simulink model "solar_pv_protected_c07_circuit"  (R2026b)
(part 5 of 16)

      | 確認の範囲　　　　　; 現在の保存回路の端子・配線から求めた静的接続。抵抗やICの内部を導線として短絡せずに集計した。説明の更新は動作シミュレーション、タイミング、実部品の性能・実機動作を保証するものではない。
      | 記録の基準　　　　　; measurement_label_layout_20261022_r01/after_layout_graph.json。部品対応表は端子名の対応付けにのみ使用。
      | 
      | 【この説明欄の略語・記号】
      | 用語1　　　　　　　 ; DC：Direct Current（直流）。ここでは直流電源または直流成分。DCバイアスはコンデンサに重なる直流電圧を指す。
      | 用語2　　　　　　　 ; DC/DC：DC-to-DC Converter（直流電圧変換器）。直流入力を別の直流電圧へ変換する電源回路。絶縁の有無は個々の部品説明で確認する。
      | 用語3　　　　　　　 ; ADC：Analog-to-Digital Converter（アナログ・デジタル変換器）。測定電圧をデジタル値へ変換する回路。電流や温度も、センサーで電圧へ変換した後に読み取る。
      | 用語4　　　　　　　 ; IC：Integrated Circuit（集積回路）。複数の電子素子と機能を小さな半導体チップに集積した部品。
      | 用語5　　　　　　　 ; CH：Channel（測定チャネル）。CH0〜CH7はADCの入力番号であり、同時測定を意味しない。
      | 用語6　　　　　　　 ; MOSFET：Metal-Oxide-Semiconductor Field-Effect Transistor（金属・酸化膜・半導体構造の電界効果トランジスタ）。ゲートとソースの電圧でドレインとソースの導通を制御する素子。N-MOSはNチャネル型を表す。
      | 用語7　　　　　　　 ; LiFePO4：Lithium Iron Phosphate（リン酸鉄リチウム）。電池の正極材料を示す化学式。英語の頭文字を並べた略語ではない。
      | 用語8　　　　　　　 ; GND：Ground（回路の基準電位・電流帰路）。この図の共通基準。保護接地や大地への接続を意味するとは限らない。
      | 用語9　　　　　　　 ; AGND：Analog Ground（アナログ回路の基準端子）。アナログ部分の電流帰路。現図では共通GNDへ接続されるが、実装時の電流経路への配慮は別途必要。
      | 用語10　　　　　　　; DGND：Digital Ground（デジタル回路の基準端子）。デジタル部分の電流帰路。現図では共通GNDへ接続される。
      | 用語11　　　　　　　; VREF/REF：基準電圧を表す端子名。REFはReference（基準）の意味。ADCの変換尺度や電流アンプの出力基準に使う。REF1/REF2の接続電位は個別に確認する。
      | 用語12　　　　　　　; VCC/VDD/VEE/VS：ICの電源端子名。文字の歴史的な由来を現在の接続機能へ当てはめない。現回路のVEEはU8/U10では浮動基準SW、U9ではGND。各電圧・基準は端子と接続を参照する。
      | 用語13　　　　　　　; GNDP：U10の一次側電源の基準端子。絶縁電源の入力側GND。二次側基準VEE=SWと直接同一の導体ではない。
      | 用語14　　　　　　　; SW：Switching Node（スイッチング点）。主電力段の上下MOSFETとL1がつながる、電圧が高速に切り替わる点。GNDとは別電位。
  GND_Label_089 : ConnectionLabel  Description=|  Label=GND
      | この回路での名前　　; GND
      | 種別　　　　　　　　; ConnectionLabel
      | この回路での役割　　; 電池BT1の負極、太陽電池列の負極、制御・測定・保護回路のGNDを結ぶ共通の帰路。高側駆動の浮動帰路SWとは別のノード。
      | 共通帰路の代表接続　; BT1（充電先の蓄電池／51.2V 100Ah LiFePO4）: -
      |                     ; PV1（直列太陽電池列の負極側パネル／400W panel 1/2）: -
      |                     ; U7（RP2040搭載Pico W／SC0918）: 3(GND), 8(GND), 13(GND), 18(GND), 23(GND), 28(GND), 33(AGND), 38(GND)
      |                     ; U1（外付けADC／MCP3208-CI/SL）: 8(CH7), 9(DGND), 14(AGND)
      |                     ; P_U1（保護MOSFETを制御する保護IC／LTC4364IMS-1#PBF）: GND
      |                     ; Q2（同期整流降圧回路の下側スイッチ／TK9R6E15Q5,S1X）: 3(S)
      |                     ; U9（低側の光ゲートドライバ／ACPL-P346-560E）: 4(VEE)
      |                     ; U10（高側ゲート用の浮動電源を作る絶縁DC/DC／UCC14131QDWNRQ1）: 1(GNDP), 2(GNDP), 5(GNDP), 8(GNDP), 9(GNDP), 10(GNDP), 11(GNDP), 12(GNDP), 13(GNDP), 14(GNDP), 15(GNDP), 16(GNDP), 17(GNDP), 18(GNDP)
      | この場所の直接接続　; U5（放熱器温度センサー／TMP235A2DBZR）: 3(GND)
      | 直接接続の範囲　　　; このラベルから実際の線・分岐・明示的な境界端子だけを追った接続。同名ラベルによる離れた場所への接続はこの欄に含めない。
      | 同一ネット全端子　　; BT1: -
      |                     ; C1: 2(n)
      |                     ; C2: 2(n)
      |                     ; C3: 2(n)
      |                     ; C4: 2(n)
      |                     ; C7: 2(n)
      |                     ; C8: 2(n)
      |                     ; C9: 2(n)
      |                     ; C10: 2(n)
      |                     ; C13: 2(n)
      |                     ; C14: 2(n)
      |                     ; C15: 2(n)
      |                     ; C16: 2(n)
      |                     ; C17: 2
      |                     ; C18: 2
      |                     ; C19: 2
      |                     ; C20: 2
      |                     ; C21: 2
      |                     ; C22: 2
      |                     ; C23: 2
      |                     ; C24: 2
      |                     ; C25: 2
      |                     ; C26: 2
      |                     ; C27: 2
      |                     ; C28: 2
      |                     ; C29: 2
      |                     ; C30: 2
      |                     ; C31: 2
      |                     ; C33: 2
      |                     ; C34: 2
      |                     ; C35: 2
      |                     ; C36: 2
      |                     ; C40: 2
      |                     ; C41: 2
      |                     ; C42: 2
      |                     ; C43: 2
      |                     ; C44: 2
      |                     ; C45: 2
      |                     ; C46: 2
      |                     ; C47: 2
      |                     ; C48: 2
      |                     ; D2: 2(A)
      |                     ; PV1: -
      |                     ; P_CHG: N
      |                     ; P_COUT: N
      |                     ; P_CTMR: N
      |                     ; P_D1: A
      |                     ; P_R3: 2
      |                     ; P_R8: 2
      |                     ; P_RSHDN_PD: 2
      |                     ; P_U1: GND
      |                     ; Q2: 3(S)
      |                     ; Q3: 1(S1), 4(S2)
      |                     ; R1: 2(n)
      |                     ; R18: 2
      |                     ; R21: 2
      |                     ; R24: 2
      |                     ; R35: 2
      |                     ; R42: 2
      |                     ; R44: 2
      |                     ; R48: 2
      |                     ; U1: 8(CH7), 9(DGND), 14(AGND)
      |                     ; U2: 2(GND), 3(REF2), 4(RESERVED_GND)
      |                     ; U3: 2(GND), 3(REF2), 4(RESERVED_GND)
      |                     ; U4: 3(GND)
      |                     ; U5: 3(GND)
      |                     ; U6: 3(GND)
      |                     ; U7: 3(GND), 8(GND), 13(GND), 18(GND), 23(GND), 28(GND), 33(AGND), 38(GND)
      |                     ; U9: 4(VEE)
      |                     ; U10: 1(GNDP), 2(GNDP), 5(GNDP), 8(GNDP), 9(GNDP), 10(GNDP), 11(GNDP), 12(GNDP), 13(GNDP), 14(GNDP), 15(GNDP), 16(GNDP), 17(GNDP), 18(GNDP)
      |                     ; U11: 2(GND)
      |                     ; U12: 2(GND)
      | 接続部品数　　　　　; 72部品（部品番号で集計。同一ネット全体）
      | 接続端子数　　　　　; 99端子（423端子の部品対応表で集計。ラベル・境界ポートの重複は含めない）
      | この場所の端子数　　; 1端子／1部品（同名ラベルによる接続を除く）
      | 同階層同名ラベル数　; 75個（このラベル自身を含む）
      | 全階層の接続ラベル　; 87個（実際に同じノードへつながるラベル。名前が違う別名も含む）
      | 接続ルール　　　　　; 同じ階層の同じラベル名を仮想配線として結ぶ。別のSubsystem内とは名前だけでつながらず、明示的なConnection Portと配線をたどる。色は用途の表示であり接続を決めない。
      | 確認の範囲　　　　　; 現在の保存回路の端子・配線から求めた静的接続。抵抗やICの内部を導線として短絡せずに集計した。説明の更新は動作シミュレーション、タイミング、実部品の性能・実機動作を保証するものではない。
      | 記録の基準　　　　　; measurement_label_layout_20261022_r01/after_layout_graph.json。部品対応表は端子名の対応付けにのみ使用。
      | 
      | 【この説明欄の略語・記号】
      | 用語1　　　　　　　 ; DC：Direct Current（直流）。ここでは直流電源または直流成分。DCバイアスはコンデンサに重なる直流電圧を指す。
      | 用語2　　　　　　　 ; DC/DC：DC-to-DC Converter（直流電圧変換器）。直流入力を別の直流電圧へ変換する電源回路。絶縁の有無は個々の部品説明で確認する。
      | 用語3　　　　　　　 ; ADC：Analog-to-Digital Converter（アナログ・デジタル変換器）。測定電圧をデジタル値へ変換する回路。電流や温度も、センサーで電圧へ変換した後に読み取る。
      | 用語4　　　　　　　 ; IC：Integrated Circuit（集積回路）。複数の電子素子と機能を小さな半導体チップに集積した部品。
      | 用語5　　　　　　　 ; CH：Channel（測定チャネル）。CH0〜CH7はADCの入力番号であり、同時測定を意味しない。
      | 用語6　　　　　　　 ; MOSFET：Metal-Oxide-Semiconductor Field-Effect Transistor（金属・酸化膜・半導体構造の電界効果トランジスタ）。ゲートとソースの電圧でドレインとソースの導通を制御する素子。N-MOSはNチャネル型を表す。
      | 用語7　　　　　　　 ; LiFePO4：Lithium Iron Phosphate（リン酸鉄リチウム）。電池の正極材料を示す化学式。英語の頭文字を並べた略語ではない。
      | 用語8　　　　　　　 ; GND：Ground（回路の基準電位・電流帰路）。この図の共通基準。保護接地や大地への接続を意味するとは限らない。
      | 用語9　　　　　　　 ; AGND：Analog Ground（アナログ回路の基準端子）。アナログ部分の電流帰路。現図では共通GNDへ接続されるが、実装時の電流経路への配慮は別途必要。
      | 用語10　　　　　　　; DGND：Digital Ground（デジタル回路の基準端子）。デジタル部分の電流帰路。現図では共通GNDへ接続される。
      | 用語11　　　　　　　; VREF/REF：基準電圧を表す端子名。REFはReference（基準）の意味。ADCの変換尺度や電流アンプの出力基準に使う。REF1/REF2の接続電位は個別に確認する。
      | 用語12　　　　　　　; VCC/VDD/VEE/VS：ICの電源端子名。文字の歴史的な由来を現在の接続機能へ当てはめない。現回路のVEEはU8/U10では浮動基準SW、U9ではGND。各電圧・基準は端子と接続を参照する。
      | 用語13　　　　　　　; GNDP：U10の一次側電源の基準端子。絶縁電源の入力側GND。二次側基準VEE=SWと直接同一の導体ではない。
      | 用語14　　　　　　　; SW：Switching Node（スイッチング点）。主電力段の上下MOSFETとL1がつながる、電圧が高速に切り替わる点。GNDとは別電位。
  GND_Label_090 : ConnectionLabel  Description=|  Label=GND
      | この回路での名前　　; GND
      | 種別　　　　　　　　; ConnectionLabel
      | この回路での役割　　; 電池BT1の負極、太陽電池列の負極、制御・測定・保護回路のGNDを結ぶ共通の帰路。高側駆動の浮動帰路SWとは別のノード。
      | 共通帰路の代表接続　; BT1（充電先の蓄電池／51.2V 100Ah LiFePO4）: -
      |                     ; PV1（直列太陽電池列の負極側パネル／400W panel 1/2）: -
      |                     ; U7（RP2040搭載Pico W／SC0918）: 3(GND), 8(GND), 13(GND), 18(GND), 23(GND), 28(GND), 33(AGND), 38(GND)
      |                     ; U1（外付けADC／MCP3208-CI/SL）: 8(CH7), 9(DGND), 14(AGND)
      |                     ; P_U1（保護MOSFETを制御する保護IC／LTC4364IMS-1#PBF）: GND
      |                     ; Q2（同期整流降圧回路の下側スイッチ／TK9R6E15Q5,S1X）: 3(S)
      |                     ; U9（低側の光ゲートドライバ／ACPL-P346-560E）: 4(VEE)
      |                     ; U10（高側ゲート用の浮動電源を作る絶縁DC/DC／UCC14131QDWNRQ1）: 1(GNDP), 2(GNDP), 5(GNDP), 8(GNDP), 9(GNDP), 10(GNDP), 11(GNDP), 12(GNDP), 13(GNDP), 14(GNDP), 15(GNDP), 16(GNDP), 17(GNDP), 18(GNDP)
      | この場所の直接接続　; U6（2.5Vの測定基準電圧源／REF3025EAIDBZR）: 3(GND)
      | 直接接続の範囲　　　; このラベルから実際の線・分岐・明示的な境界端子だけを追った接続。同名ラベルによる離れた場所への接続はこの欄に含めない。
      | 同一ネット全端子　　; BT1: -
      |                     ; C1: 2(n)
      |                     ; C2: 2(n)
      |                     ; C3: 2(n)
      |                     ; C4: 2(n)
      |                     ; C7: 2(n)
      |                     ; C8: 2(n)
      |                     ; C9: 2(n)
      |                     ; C10: 2(n)
      |                     ; C13: 2(n)
      |                     ; C14: 2(n)
      |                     ; C15: 2(n)
      |                     ; C16: 2(n)
      |                     ; C17: 2
      |                     ; C18: 2
      |                     ; C19: 2
      |                     ; C20: 2
      |                     ; C21: 2
      |                     ; C22: 2
      |                     ; C23: 2
      |                     ; C24: 2
      |                     ; C25: 2
      |                     ; C26: 2
      |                     ; C27: 2
      |                     ; C28: 2
      |                     ; C29: 2
      |                     ; C30: 2
      |                     ; C31: 2
      |                     ; C33: 2
      |                     ; C34: 2
      |                     ; C35: 2
      |                     ; C36: 2
      |                     ; C40: 2
      |                     ; C41: 2
      |                     ; C42: 2
      |                     ; C43: 2
      |                     ; C44: 2
      |                     ; C45: 2
      |                     ; C46: 2
      |                     ; C47: 2
      |                     ; C48: 2
      |                     ; D2: 2(A)
      |                     ; PV1: -
      |                     ; P_CHG: N
      |                     ; P_COUT: N
      |                     ; P_CTMR: N
      |                     ; P_D1: A
      |                     ; P_R3: 2
      |                     ; P_R8: 2
      |                     ; P_RSHDN_PD: 2
      |                     ; P_U1: GND
      |                     ; Q2: 3(S)
      |                     ; Q3: 1(S1), 4(S2)
      |                     ; R1: 2(n)
      |                     ; R18: 2
      |                     ; R21: 2
      |                     ; R24: 2
      |                     ; R35: 2
      |                     ; R42: 2
      |                     ; R44: 2
      |                     ; R48: 2
      |                     ; U1: 8(CH7), 9(DGND), 14(AGND)
      |                     ; U2: 2(GND), 3(REF2), 4(RESERVED_GND)
      |                     ; U3: 2(GND), 3(REF2), 4(RESERVED_GND)
      |                     ; U4: 3(GND)
      |                     ; U5: 3(GND)
      |                     ; U6: 3(GND)
      |                     ; U7: 3(GND), 8(GND), 13(GND), 18(GND), 23(GND), 28(GND), 33(AGND), 38(GND)
      |                     ; U9: 4(VEE)
      |                     ; U10: 1(GNDP), 2(GNDP), 5(GNDP), 8(GNDP), 9(GNDP), 10(GNDP), 11(GNDP), 12(GNDP), 13(GNDP), 14(GNDP), 15(GNDP), 16(GNDP), 17(GNDP), 18(GNDP)
      |                     ; U11: 2(GND)
      |                     ; U12: 2(GND)
      | 接続部品数　　　　　; 72部品（部品番号で集計。同一ネット全体）
      | 接続端子数　　　　　; 99端子（423端子の部品対応表で集計。ラベル・境界ポートの重複は含めない）
      | この場所の端子数　　; 1端子／1部品（同名ラベルによる接続を除く）
      | 同階層同名ラベル数　; 75個（このラベル自身を含む）
      | 全階層の接続ラベル　; 87個（実際に同じノードへつながるラベル。名前が違う別名も含む）
      | 接続ルール　　　　　; 同じ階層の同じラベル名を仮想配線として結ぶ。別のSubsystem内とは名前だけでつながらず、明示的なConnection Portと配線をたどる。色は用途の表示であり接続を決めない。
      | 確認の範囲　　　　　; 現在の保存回路の端子・配線から求めた静的接続。抵抗やICの内部を導線として短絡せずに集計した。説明の更新は動作シミュレーション、タイミング、実部品の性能・実機動作を保証するものではない。
      | 記録の基準　　　　　; measurement_label_layout_20261022_r01/after_layout_graph.json。部品対応表は端子名の対応付けにのみ使用。
      | 
      | 【この説明欄の略語・記号】
      | 用語1　　　　　　　 ; DC：Direct Current（直流）。ここでは直流電源または直流成分。DCバイアスはコンデンサに重なる直流電圧を指す。
      | 用語2　　　　　　　 ; DC/DC：DC-to-DC Converter（直流電圧変換器）。直流入力を別の直流電圧へ変換する電源回路。絶縁の有無は個々の部品説明で確認する。
      | 用語3　　　　　　　 ; ADC：Analog-to-Digital Converter（アナログ・デジタル変換器）。測定電圧をデジタル値へ変換する回路。電流や温度も、センサーで電圧へ変換した後に読み取る。
      | 用語4　　　　　　　 ; IC：Integrated Circuit（集積回路）。複数の電子素子と機能を小さな半導体チップに集積した部品。
      | 用語5　　　　　　　 ; CH：Channel（測定チャネル）。CH0〜CH7はADCの入力番号であり、同時測定を意味しない。
      | 用語6　　　　　　　 ; MOSFET：Metal-Oxide-Semiconductor Field-Effect Transistor（金属・酸化膜・半導体構造の電界効果トランジスタ）。ゲートとソースの電圧でドレインとソースの導通を制御する素子。N-MOSはNチャネル型を表す。
      | 用語7　　　　　　　 ; LiFePO4：Lithium Iron Phosphate（リン酸鉄リチウム）。電池の正極材料を示す化学式。英語の頭文字を並べた略語ではない。
      | 用語8　　　　　　　 ; GND：Ground（回路の基準電位・電流帰路）。この図の共通基準。保護接地や大地への接続を意味するとは限らない。
      | 用語9　　　　　　　 ; AGND：Analog Ground（アナログ回路の基準端子）。アナログ部分の電流帰路。現図では共通GNDへ接続されるが、実装時の電流経路への配慮は別途必要。
      | 用語10　　　　　　　; DGND：Digital Ground（デジタル回路の基準端子）。デジタル部分の電流帰路。現図では共通GNDへ接続される。
      | 用語11　　　　　　　; VREF/REF：基準電圧を表す端子名。REFはReference（基準）の意味。ADCの変換尺度や電流アンプの出力基準に使う。REF1/REF2の接続電位は個別に確認する。
      | 用語12　　　　　　　; VCC/VDD/VEE/VS：ICの電源端子名。文字の歴史的な由来を現在の接続機能へ当てはめない。現回路のVEEはU8/U10では浮動基準SW、U9ではGND。各電圧・基準は端子と接続を参照する。
      | 用語13　　　　　　　; GNDP：U10の一次側電源の基準端子。絶縁電源の入力側GND。二次側基準VEE=SWと直接同一の導体ではない。
      | 用語14　　　　　　　; SW：Switching Node（スイッチング点）。主電力段の上下MOSFETとL1がつながる、電圧が高速に切り替わる点。GNDとは別電位。
  GND_Label_091 : ConnectionLabel  Description=|  Label=GND
      | この回路での名前　　; GND
      | 種別　　　　　　　　; ConnectionLabel
      | この回路での役割　　; 電池BT1の負極、太陽電池列の負極、制御・測定・保護回路のGNDを結ぶ共通の帰路。高側駆動の浮動帰路SWとは別のノード。
      | 共通帰路の代表接続　; BT1（充電先の蓄電池／51.2V 100Ah LiFePO4）: -
      |                     ; PV1（直列太陽電池列の負極側パネル／400W panel 1/2）: -
      |                     ; U7（RP2040搭載Pico W／SC0918）: 3(GND), 8(GND), 13(GND), 18(GND), 23(GND), 28(GND), 33(AGND), 38(GND)
      |                     ; U1（外付けADC／MCP3208-CI/SL）: 8(CH7), 9(DGND), 14(AGND)
      |                     ; P_U1（保護MOSFETを制御する保護IC／LTC4364IMS-1#PBF）: GND
      |                     ; Q2（同期整流降圧回路の下側スイッチ／TK9R6E15Q5,S1X）: 3(S)
      |                     ; U9（低側の光ゲートドライバ／ACPL-P346-560E）: 4(VEE)
      |                     ; U10（高側ゲート用の浮動電源を作る絶縁DC/DC／UCC14131QDWNRQ1）: 1(GNDP), 2(GNDP), 5(GNDP), 8(GNDP), 9(GNDP), 10(GNDP), 11(GNDP), 12(GNDP), 13(GNDP), 14(GNDP), 15(GNDP), 16(GNDP), 17(GNDP), 18(GNDP)
      | この場所の直接接続　; U7（RP2040搭載Pico W／SC0918）: 3(GND)
      | 直接接続の範囲　　　; このラベルから実際の線・分岐・明示的な境界端子だけを追った接続。同名ラベルによる離れた場所への接続はこの欄に含めない。
      | 同一ネット全端子　　; BT1: -
      |                     ; C1: 2(n)
      |                     ; C2: 2(n)
      |                     ; C3: 2(n)
      |                     ; C4: 2(n)
      |                     ; C7: 2(n)
      |                     ; C8: 2(n)
      |                     ; C9: 2(n)
      |                     ; C10: 2(n)
      |                     ; C13: 2(n)
      |                     ; C14: 2(n)
      |                     ; C15: 2(n)
      |                     ; C16: 2(n)
      |                     ; C17: 2
      |                     ; C18: 2
      |                     ; C19: 2
      |                     ; C20: 2
      |                     ; C21: 2
      |                     ; C22: 2
      |                     ; C23: 2
      |                     ; C24: 2
      |                     ; C25: 2
      |                     ; C26: 2
      |                     ; C27: 2
      |                     ; C28: 2
      |                     ; C29: 2
      |                     ; C30: 2
      |                     ; C31: 2
      |                     ; C33: 2
      |                     ; C34: 2
      |                     ; C35: 2
      |                     ; C36: 2
      |                     ; C40: 2
      |                     ; C41: 2
      |                     ; C42: 2
      |                     ; C43: 2
      |                     ; C44: 2
      |                     ; C45: 2
      |                     ; C46: 2
      |                     ; C47: 2
      |                     ; C48: 2
      |                     ; D2: 2(A)
      |                     ; PV1: -
      |                     ; P_CHG: N
      |                     ; P_COUT: N
      |                     ; P_CTMR: N
      |                     ; P_D1: A
      |                     ; P_R3: 2
      |                     ; P_R8: 2
      |                     ; P_RSHDN_PD: 2
      |                     ; P_U1: GND
      |                     ; Q2: 3(S)
      |                     ; Q3: 1(S1), 4(S2)
      |                     ; R1: 2(n)
      |                     ; R18: 2
      |                     ; R21: 2
      |                     ; R24: 2
      |                     ; R35: 2
      |                     ; R42: 2
      |                     ; R44: 2
      |                     ; R48: 2
      |                     ; U1: 8(CH7), 9(DGND), 14(AGND)
      |                     ; U2: 2(GND), 3(REF2), 4(RESERVED_GND)
      |                     ; U3: 2(GND), 3(REF2), 4(RESERVED_GND)
      |                     ; U4: 3(GND)
      |                     ; U5: 3(GND)
      |                     ; U6: 3(GND)
      |                     ; U7: 3(GND), 8(GND), 13(GND), 18(GND), 23(GND), 28(GND), 33(AGND), 38(GND)
      |                     ; U9: 4(VEE)
      |                     ; U10: 1(GNDP), 2(GNDP), 5(GNDP), 8(GNDP), 9(GNDP), 10(GNDP), 11(GNDP), 12(GNDP), 13(GNDP), 14(GNDP), 15(GNDP), 16(GNDP), 17(GNDP), 18(GNDP)
      |                     ; U11: 2(GND)
      |                     ; U12: 2(GND)
      | 接続部品数　　　　　; 72部品（部品番号で集計。同一ネット全体）
      | 接続端子数　　　　　; 99端子（423端子の部品対応表で集計。ラベル・境界ポートの重複は含めない）
      | この場所の端子数　　; 1端子／1部品（同名ラベルによる接続を除く）
      | 同階層同名ラベル数　; 75個（このラベル自身を含む）
      | 全階層の接続ラベル　; 87個（実際に同じノードへつながるラベル。名前が違う別名も含む）
      | 接続ルール　　　　　; 同じ階層の同じラベル名を仮想配線として結ぶ。別のSubsystem内とは名前だけでつながらず、明示的なConnection Portと配線をたどる。色は用途の表示であり接続を決めない。
      | 確認の範囲　　　　　; 現在の保存回路の端子・配線から求めた静的接続。抵抗やICの内部を導線として短絡せずに集計した。説明の更新は動作シミュレーション、タイミング、実部品の性能・実機動作を保証するものではない。
      | 記録の基準　　　　　; measurement_label_layout_20261022_r01/after_layout_graph.json。部品対応表は端子名の対応付けにのみ使用。
      | 
      | 【この説明欄の略語・記号】
      | 用語1　　　　　　　 ; DC：Direct Current（直流）。ここでは直流電源または直流成分。DCバイアスはコンデンサに重なる直流電圧を指す。
      | 用語2　　　　　　　 ; DC/DC：DC-to-DC Converter（直流電圧変換器）。直流入力を別の直流電圧へ変換する電源回路。絶縁の有無は個々の部品説明で確認する。
      | 用語3　　　　　　　 ; ADC：Analog-to-Digital Converter（アナログ・デジタル変換器）。測定電圧をデジタル値へ変換する回路。電流や温度も、センサーで電圧へ変換した後に読み取る。
      | 用語4　　　　　　　 ; IC：Integrated Circuit（集積回路）。複数の電子素子と機能を小さな半導体チップに集積した部品。
      | 用語5　　　　　　　 ; CH：Channel（測定チャネル）。CH0〜CH7はADCの入力番号であり、同時測定を意味しない。
      | 用語6　　　　　　　 ; MOSFET：Metal-Oxide-Semiconductor Field-Effect Transistor（金属・酸化膜・半導体構造の電界効果トランジスタ）。ゲートとソースの電圧でドレインとソースの導通を制御する素子。N-MOSはNチャネル型を表す。
      | 用語7　　　　　　　 ; LiFePO4：Lithium Iron Phosphate（リン酸鉄リチウム）。電池の正極材料を示す化学式。英語の頭文字を並べた略語ではない。
      | 用語8　　　　　　　 ; GND：Ground（回路の基準電位・電流帰路）。この図の共通基準。保護接地や大地への接続を意味するとは限らない。
      | 用語9　　　　　　　 ; AGND：Analog Ground（アナログ回路の基準端子）。アナログ部分の電流帰路。現図では共通GNDへ接続されるが、実装時の電流経路への配慮は別途必要。
      | 用語10　　　　　　　; DGND：Digital Ground（デジタル回路の基準端子）。デジタル部分の電流帰路。現図では共通GNDへ接続される。
      | 用語11　　　　　　　; VREF/REF：基準電圧を表す端子名。REFはReference（基準）の意味。ADCの変換尺度や電流アンプの出力基準に使う。REF1/REF2の接続電位は個別に確認する。
      | 用語12　　　　　　　; VCC/VDD/VEE/VS：ICの電源端子名。文字の歴史的な由来を現在の接続機能へ当てはめない。現回路のVEEはU8/U10では浮動基準SW、U9ではGND。各電圧・基準は端子と接続を参照する。
      | 用語13　　　　　　　; GNDP：U10の一次側電源の基準端子。絶縁電源の入力側GND。二次側基準VEE=SWと直接同一の導体ではない。
      | 用語14　　　　　　　; SW：Switching Node（スイッチング点）。主電力段の上下MOSFETとL1がつながる、電圧が高速に切り替わる点。GNDとは別電位。
  GND_Label_092 : ConnectionLabel  Description=|  Label=GND
      | この回路での名前　　; GND
      | 種別　　　　　　　　; ConnectionLabel
      | この回路での役割　　; 電池BT1の負極、太陽電池列の負極、制御・測定・保護回路のGNDを結ぶ共通の帰路。高側駆動の浮動帰路SWとは別のノード。
      | 共通帰路の代表接続　; BT1（充電先の蓄電池／51.2V 100Ah LiFePO4）: -
      |                     ; PV1（直列太陽電池列の負極側パネル／400W panel 1/2）: -
      |                     ; U7（RP2040搭載Pico W／SC0918）: 3(GND), 8(GND), 13(GND), 18(GND), 23(GND), 28(GND), 33(AGND), 38(GND)
      |                     ; U1（外付けADC／MCP3208-CI/SL）: 8(CH7), 9(DGND), 14(AGND)
      |                     ; P_U1（保護MOSFETを制御する保護IC／LTC4364IMS-1#PBF）: GND
      |                     ; Q2（同期整流降圧回路の下側スイッチ／TK9R6E15Q5,S1X）: 3(S)
      |                     ; U9（低側の光ゲートドライバ／ACPL-P346-560E）: 4(VEE)
      |                     ; U10（高側ゲート用の浮動電源を作る絶縁DC/DC／UCC14131QDWNRQ1）: 1(GNDP), 2(GNDP), 5(GNDP), 8(GNDP), 9(GNDP), 10(GNDP), 11(GNDP), 12(GNDP), 13(GNDP), 14(GNDP), 15(GNDP), 16(GNDP), 17(GNDP), 18(GNDP)
      | この場所の直接接続　; U7（RP2040搭載Pico W／SC0918）: 8(GND)
      | 直接接続の範囲　　　; このラベルから実際の線・分岐・明示的な境界端子だけを追った接続。同名ラベルによる離れた場所への接続はこの欄に含めない。
      | 同一ネット全端子　　; BT1: -
      |                     ; C1: 2(n)
      |                     ; C2: 2(n)
      |                     ; C3: 2(n)
      |                     ; C4: 2(n)
      |                     ; C7: 2(n)
      |                     ; C8: 2(n)
      |                     ; C9: 2(n)
      |                     ; C10: 2(n)
      |                     ; C13: 2(n)
      |                     ; C14: 2(n)
      |                     ; C15: 2(n)
      |                     ; C16: 2(n)
      |                     ; C17: 2
      |                     ; C18: 2
      |                     ; C19: 2
      |                     ; C20: 2
      |                     ; C21: 2
      |                     ; C22: 2
      |                     ; C23: 2
      |                     ; C24: 2
      |                     ; C25: 2
      |                     ; C26: 2
      |                     ; C27: 2
      |                     ; C28: 2
      |                     ; C29: 2
      |                     ; C30: 2
      |                     ; C31: 2
      |                     ; C33: 2
      |                     ; C34: 2
      |                     ; C35: 2
      |                     ; C36: 2
      |                     ; C40: 2
      |                     ; C41: 2
      |                     ; C42: 2
      |                     ; C43: 2
      |                     ; C44: 2
      |                     ; C45: 2
      |                     ; C46: 2
      |                     ; C47: 2
      |                     ; C48: 2
      |                     ; D2: 2(A)
      |                     ; PV1: -
      |                     ; P_CHG: N
      |                     ; P_COUT: N
      |                     ; P_CTMR: N
      |                     ; P_D1: A
      |                     ; P_R3: 2
      |                     ; P_R8: 2
      |                     ; P_RSHDN_PD: 2
      |                     ; P_U1: GND
      |                     ; Q2: 3(S)
      |                     ; Q3: 1(S1), 4(S2)
      |                     ; R1: 2(n)
      |                     ; R18: 2
      |                     ; R21: 2
      |                     ; R24: 2
      |                     ; R35: 2
      |                     ; R42: 2
      |                     ; R44: 2
      |                     ; R48: 2
      |                     ; U1: 8(CH7), 9(DGND), 14(AGND)
      |                     ; U2: 2(GND), 3(REF2), 4(RESERVED_GND)
      |                     ; U3: 2(GND), 3(REF2), 4(RESERVED_GND)
      |                     ; U4: 3(GND)
      |                     ; U5: 3(GND)
      |                     ; U6: 3(GND)
      |                     ; U7: 3(GND), 8(GND), 13(GND), 18(GND), 23(GND), 28(GND), 33(AGND), 38(GND)
      |                     ; U9: 4(VEE)
      |                     ; U10: 1(GNDP), 2(GNDP), 5(GNDP), 8(GNDP), 9(GNDP), 10(GNDP), 11(GNDP), 12(GNDP), 13(GNDP), 14(GNDP), 15(GNDP), 16(GNDP), 17(GNDP), 18(GNDP)
      |                     ; U11: 2(GND)
      |                     ; U12: 2(GND)
      | 接続部品数　　　　　; 72部品（部品番号で集計。同一ネット全体）
      | 接続端子数　　　　　; 99端子（423端子の部品対応表で集計。ラベル・境界ポートの重複は含めない）
      | この場所の端子数　　; 1端子／1部品（同名ラベルによる接続を除く）
      | 同階層同名ラベル数　; 75個（このラベル自身を含む）
      | 全階層の接続ラベル　; 87個（実際に同じノードへつながるラベル。名前が違う別名も含む）
      | 接続ルール　　　　　; 同じ階層の同じラベル名を仮想配線として結ぶ。別のSubsystem内とは名前だけでつながらず、明示的なConnection Portと配線をたどる。色は用途の表示であり接続を決めない。
      | 確認の範囲　　　　　; 現在の保存回路の端子・配線から求めた静的接続。抵抗やICの内部を導線として短絡せずに集計した。説明の更新は動作シミュレーション、タイミング、実部品の性能・実機動作を保証するものではない。
      | 記録の基準　　　　　; measurement_label_layout_20261022_r01/after_layout_graph.json。部品対応表は端子名の対応付けにのみ使用。
      | 
      | 【この説明欄の略語・記号】
      | 用語1　　　　　　　 ; DC：Direct Current（直流）。ここでは直流電源または直流成分。DCバイアスはコンデンサに重なる直流電圧を指す。
      | 用語2　　　　　　　 ; DC/DC：DC-to-DC Converter（直流電圧変換器）。直流入力を別の直流電圧へ変換する電源回路。絶縁の有無は個々の部品説明で確認する。
      | 用語3　　　　　　　 ; ADC：Analog-to-Digital Converter（アナログ・デジタル変換器）。測定電圧をデジタル値へ変換する回路。電流や温度も、センサーで電圧へ変換した後に読み取る。
      | 用語4　　　　　　　 ; IC：Integrated Circuit（集積回路）。複数の電子素子と機能を小さな半導体チップに集積した部品。
      | 用語5　　　　　　　 ; CH：Channel（測定チャネル）。CH0〜CH7はADCの入力番号であり、同時測定を意味しない。
      | 用語6　　　　　　　 ; MOSFET：Metal-Oxide-Semiconductor Field-Effect Transistor（金属・酸化膜・半導体構造の電界効果トランジスタ）。ゲートとソースの電圧でドレインとソースの導通を制御する素子。N-MOSはNチャネル型を表す。
      | 用語7　　　　　　　 ; LiFePO4：Lithium Iron Phosphate（リン酸鉄リチウム）。電池の正極材料を示す化学式。英語の頭文字を並べた略語ではない。
      | 用語8　　　　　　　 ; GND：Ground（回路の基準電位・電流帰路）。この図の共通基準。保護接地や大地への接続を意味するとは限らない。
      | 用語9　　　　　　　 ; AGND：Analog Ground（アナログ回路の基準端子）。アナログ部分の電流帰路。現図では共通GNDへ接続されるが、実装時の電流経路への配慮は別途必要。
      | 用語10　　　　　　　; DGND：Digital Ground（デジタル回路の基準端子）。デジタル部分の電流帰路。現図では共通GNDへ接続される。
      | 用語11　　　　　　　; VREF/REF：基準電圧を表す端子名。REFはReference（基準）の意味。ADCの変換尺度や電流アンプの出力基準に使う。REF1/REF2の接続電位は個別に確認する。
      | 用語12　　　　　　　; VCC/VDD/VEE/VS：ICの電源端子名。文字の歴史的な由来を現在の接続機能へ当てはめない。現回路のVEEはU8/U10では浮動基準SW、U9ではGND。各電圧・基準は端子と接続を参照する。
      | 用語13　　　　　　　; GNDP：U10の一次側電源の基準端子。絶縁電源の入力側GND。二次側基準VEE=SWと直接同一の導体ではない。
      | 用語14　　　　　　　; SW：Switching Node（スイッチング点）。主電力段の上下MOSFETとL1がつながる、電圧が高速に切り替わる点。GNDとは別電位。
  GND_Label_093 : ConnectionLabel  Description=|  Label=GND
      | この回路での名前　　; GND
      | 種別　　　　　　　　; ConnectionLabel
      | この回路での役割　　; 電池BT1の負極、太陽電池列の負極、制御・測定・保護回路のGNDを結ぶ共通の帰路。高側駆動の浮動帰路SWとは別のノード。
      | 共通帰路の代表接続　; BT1（充電先の蓄電池／51.2V 100Ah LiFePO4）: -
      |                     ; PV1（直列太陽電池列の負極側パネル／400W panel 1/2）: -
      |                     ; U7（RP2040搭載Pico W／SC0918）: 3(GND), 8(GND), 13(GND), 18(GND), 23(GND), 28(GND), 33(AGND), 38(GND)
      |                     ; U1（外付けADC／MCP3208-CI/SL）: 8(CH7), 9(DGND), 14(AGND)
      |                     ; P_U1（保護MOSFETを制御する保護IC／LTC4364IMS-1#PBF）: GND
      |                     ; Q2（同期整流降圧回路の下側スイッチ／TK9R6E15Q5,S1X）: 3(S)
      |                     ; U9（低側の光ゲートドライバ／ACPL-P346-560E）: 4(VEE)
      |                     ; U10（高側ゲート用の浮動電源を作る絶縁DC/DC／UCC14131QDWNRQ1）: 1(GNDP), 2(GNDP), 5(GNDP), 8(GNDP), 9(GNDP), 10(GNDP), 11(GNDP), 12(GNDP), 13(GNDP), 14(GNDP), 15(GNDP), 16(GNDP), 17(GNDP), 18(GNDP)
      | この場所の直接接続　; U7（RP2040搭載Pico W／SC0918）: 13(GND)
      | 直接接続の範囲　　　; このラベルから実際の線・分岐・明示的な境界端子だけを追った接続。同名ラベルによる離れた場所への接続はこの欄に含めない。
      | 同一ネット全端子　　; BT1: -
      |                     ; C1: 2(n)
      |                     ; C2: 2(n)
      |                     ; C3: 2(n)
      |                     ; C4: 2(n)
      |                     ; C7: 2(n)
      |                     ; C8: 2(n)
      |                     ; C9: 2(n)
      |                     ; C10: 2(n)
      |                     ; C13: 2(n)
      |                     ; C14: 2(n)
      |                     ; C15: 2(n)
      |                     ; C16: 2(n)
      |                     ; C17: 2
      |                     ; C18: 2
      |                     ; C19: 2
      |                     ; C20: 2
      |                     ; C21: 2
      |                     ; C22: 2
      |                     ; C23: 2
      |                     ; C24: 2
      |                     ; C25: 2
      |                     ; C26: 2
      |                     ; C27: 2
      |                     ; C28: 2
      |                     ; C29: 2
      |                     ; C30: 2
      |                     ; C31: 2
      |                     ; C33: 2
      |                     ; C34: 2
      |                     ; C35: 2
      |                     ; C36: 2
      |                     ; C40: 2
      |                     ; C41: 2
      |                     ; C42: 2
      |                     ; C43: 2
      |                     ; C44: 2
      |                     ; C45: 2
      |                     ; C46: 2
      |                     ; C47: 2
      |                     ; C48: 2
      |                     ; D2: 2(A)
      |                     ; PV1: -
      |                     ; P_CHG: N
      |                     ; P_COUT: N
      |                     ; P_CTMR: N
      |                     ; P_D1: A
      |                     ; P_R3: 2
      |                     ; P_R8: 2
      |                     ; P_RSHDN_PD: 2
      |                     ; P_U1: GND
      |                     ; Q2: 3(S)
      |                     ; Q3: 1(S1), 4(S2)
      |                     ; R1: 2(n)
      |                     ; R18: 2
      |                     ; R21: 2
      |                     ; R24: 2
      |                     ; R35: 2
      |                     ; R42: 2
      |                     ; R44: 2
      |                     ; R48: 2
      |                     ; U1: 8(CH7), 9(DGND), 14(AGND)
      |                     ; U2: 2(GND), 3(REF2), 4(RESERVED_GND)
      |                     ; U3: 2(GND), 3(REF2), 4(RESERVED_GND)
      |                     ; U4: 3(GND)
      |                     ; U5: 3(GND)
      |                     ; U6: 3(GND)
      |                     ; U7: 3(GND), 8(GND), 13(GND), 18(GND), 23(GND), 28(GND), 33(AGND), 38(GND)
      |                     ; U9: 4(VEE)
      |                     ; U10: 1(GNDP), 2(GNDP), 5(GNDP), 8(GNDP), 9(GNDP), 10(GNDP), 11(GNDP), 12(GNDP), 13(GNDP), 14(GNDP), 15(GNDP), 16(GNDP), 17(GNDP), 18(GNDP)
      |                     ; U11: 2(GND)
      |                     ; U12: 2(GND)
      | 接続部品数　　　　　; 72部品（部品番号で集計。同一ネット全体）
      | 接続端子数　　　　　; 99端子（423端子の部品対応表で集計。ラベル・境界ポートの重複は含めない）
      | この場所の端子数　　; 1端子／1部品（同名ラベルによる接続を除く）
      | 同階層同名ラベル数　; 75個（このラベル自身を含む）
      | 全階層の接続ラベル　; 87個（実際に同じノードへつながるラベル。名前が違う別名も含む）
      | 接続ルール　　　　　; 同じ階層の同じラベル名を仮想配線として結ぶ。別のSubsystem内とは名前だけでつながらず、明示的なConnection Portと配線をたどる。色は用途の表示であり接続を決めない。
      | 確認の範囲　　　　　; 現在の保存回路の端子・配線から求めた静的接続。抵抗やICの内部を導線として短絡せずに集計した。説明の更新は動作シミュレーション、タイミング、実部品の性能・実機動作を保証するものではない。
      | 記録の基準　　　　　; measurement_label_layout_20261022_r01/after_layout_graph.json。部品対応表は端子名の対応付けにのみ使用。
      | 
      | 【この説明欄の略語・記号】
      | 用語1　　　　　　　 ; DC：Direct Current（直流）。ここでは直流電源または直流成分。DCバイアスはコンデンサに重なる直流電圧を指す。
      | 用語2　　　　　　　 ; DC/DC：DC-to-DC Converter（直流電圧変換器）。直流入力を別の直流電圧へ変換する電源回路。絶縁の有無は個々の部品説明で確認する。
      | 用語3　　　　　　　 ; ADC：Analog-to-Digital Converter（アナログ・デジタル変換器）。測定電圧をデジタル値へ変換する回路。電流や温度も、センサーで電圧へ変換した後に読み取る。
      | 用語4　　　　　　　 ; IC：Integrated Circuit（集積回路）。複数の電子素子と機能を小さな半導体チップに集積した部品。
      | 用語5　　　　　　　 ; CH：Channel（測定チャネル）。CH0〜CH7はADCの入力番号であり、同時測定を意味しない。
      | 用語6　　　　　　　 ; MOSFET：Metal-Oxide-Semiconductor Field-Effect Transistor（金属・酸化膜・半導体構造の電界効果トランジスタ）。ゲートとソースの電圧でドレインとソースの導通を制御する素子。N-MOSはNチャネル型を表す。
      | 用語7　　　　　　　 ; LiFePO4：Lithium Iron Phosphate（リン酸鉄リチウム）。電池の正極材料を示す化学式。英語の頭文字を並べた略語ではない。
      | 用語8　　　　　　　 ; GND：Ground（回路の基準電位・電流帰路）。この図の共通基準。保護接地や大地への接続を意味するとは限らない。
      | 用語9　　　　　　　 ; AGND：Analog Ground（アナログ回路の基準端子）。アナログ部分の電流帰路。現図では共通GNDへ接続されるが、実装時の電流経路への配慮は別途必要。
      | 用語10　　　　　　　; DGND：Digital Ground（デジタル回路の基準端子）。デジタル部分の電流帰路。現図では共通GNDへ接続される。
      | 用語11　　　　　　　; VREF/REF：基準電圧を表す端子名。REFはReference（基準）の意味。ADCの変換尺度や電流アンプの出力基準に使う。REF1/REF2の接続電位は個別に確認する。
      | 用語12　　　　　　　; VCC/VDD/VEE/VS：ICの電源端子名。文字の歴史的な由来を現在の接続機能へ当てはめない。現回路のVEEはU8/U10では浮動基準SW、U9ではGND。各電圧・基準は端子と接続を参照する。
      | 用語13　　　　　　　; GNDP：U10の一次側電源の基準端子。絶縁電源の入力側GND。二次側基準VEE=SWと直接同一の導体ではない。
      | 用語14　　　　　　　; SW：Switching Node（スイッチング点）。主電力段の上下MOSFETとL1がつながる、電圧が高速に切り替わる点。GNDとは別電位。
  GND_Label_094 : ConnectionLabel  Description=|  Label=GND
      | この回路での名前　　; GND
      | 種別　　　　　　　　; ConnectionLabel
      | この回路での役割　　; 電池BT1の負極、太陽電池列の負極、制御・測定・保護回路のGNDを結ぶ共通の帰路。高側駆動の浮動帰路SWとは別のノード。
      | 共通帰路の代表接続　; BT1（充電先の蓄電池／51.2V 100Ah LiFePO4）: -
      |                     ; PV1（直列太陽電池列の負極側パネル／400W panel 1/2）: -
      |                     ; U7（RP2040搭載Pico W／SC0918）: 3(GND), 8(GND), 13(GND), 18(GND), 23(GND), 28(GND), 33(AGND), 38(GND)
      |                     ; U1（外付けADC／MCP3208-CI/SL）: 8(CH7), 9(DGND), 14(AGND)
      |                     ; P_U1（保護MOSFETを制御する保護IC／LTC4364IMS-1#PBF）: GND
      |                     ; Q2（同期整流降圧回路の下側スイッチ／TK9R6E15Q5,S1X）: 3(S)
      |                     ; U9（低側の光ゲートドライバ／ACPL-P346-560E）: 4(VEE)
      |                     ; U10（高側ゲート用の浮動電源を作る絶縁DC/DC／UCC14131QDWNRQ1）: 1(GNDP), 2(GNDP), 5(GNDP), 8(GNDP), 9(GNDP), 10(GNDP), 11(GNDP), 12(GNDP), 13(GNDP), 14(GNDP), 15(GNDP), 16(GNDP), 17(GNDP), 18(GNDP)
      | この場所の直接接続　; U7（RP2040搭載Pico W／SC0918）: 18(GND)
      | 直接接続の範囲　　　; このラベルから実際の線・分岐・明示的な境界端子だけを追った接続。同名ラベルによる離れた場所への接続はこの欄に含めない。
      | 同一ネット全端子　　; BT1: -
      |                     ; C1: 2(n)
      |                     ; C2: 2(n)
      |                     ; C3: 2(n)
      |                     ; C4: 2(n)
      |                     ; C7: 2(n)
      |                     ; C8: 2(n)
      |                     ; C9: 2(n)
      |                     ; C10: 2(n)
      |                     ; C13: 2(n)
      |                     ; C14: 2(n)
      |                     ; C15: 2(n)
      |                     ; C16: 2(n)
      |                     ; C17: 2
      |                     ; C18: 2
      |                     ; C19: 2
      |                     ; C20: 2
      |                     ; C21: 2
      |                     ; C22: 2
      |                     ; C23: 2
      |                     ; C24: 2
      |                     ; C25: 2
      |                     ; C26: 2
      |                     ; C27: 2
      |                     ; C28: 2
      |                     ; C29: 2
      |                     ; C30: 2
      |                     ; C31: 2
      |                     ; C33: 2
      |                     ; C34: 2
      |                     ; C35: 2
      |                     ; C36: 2
      |                     ; C40: 2
      |                     ; C41: 2
      |                     ; C42: 2
      |                     ; C43: 2
      |                     ; C44: 2
      |                     ; C45: 2
      |                     ; C46: 2
      |                     ; C47: 2
      |                     ; C48: 2
      |                     ; D2: 2(A)
      |                     ; PV1: -
      |                     ; P_CHG: N
      |                     ; P_COUT: N
      |                     ; P_CTMR: N
      |                     ; P_D1: A
      |                     ; P_R3: 2
      |                     ; P_R8: 2
      |                     ; P_RSHDN_PD: 2
      |                     ; P_U1: GND
      |                     ; Q2: 3(S)
      |                     ; Q3: 1(S1), 4(S2)
      |                     ; R1: 2(n)
      |                     ; R18: 2
      |                     ; R21: 2
      |                     ; R24: 2
      |                     ; R35: 2
      |                     ; R42: 2
      |                     ; R44: 2
      |                     ; R48: 2
      |                     ; U1: 8(CH7), 9(DGND), 14(AGND)
      |                     ; U2: 2(GND), 3(REF2), 4(RESERVED_GND)
      |                     ; U3: 2(GND), 3(REF2), 4(RESERVED_GND)
      |                     ; U4: 3(GND)
      |                     ; U5: 3(GND)
      |                     ; U6: 3(GND)
      |                     ; U7: 3(GND), 8(GND), 13(GND), 18(GND), 23(GND), 28(GND), 33(AGND), 38(GND)
      |                     ; U9: 4(VEE)
      |                     ; U10: 1(GNDP), 2(GNDP), 5(GNDP), 8(GNDP), 9(GNDP), 10(GNDP), 11(GNDP), 12(GNDP), 13(GNDP), 14(GNDP), 15(GNDP), 16(GNDP), 17(GNDP), 18(GNDP)
      |                     ; U11: 2(GND)
      |                     ; U12: 2(GND)
      | 接続部品数　　　　　; 72部品（部品番号で集計。同一ネット全体）
      | 接続端子数　　　　　; 99端子（423端子の部品対応表で集計。ラベル・境界ポートの重複は含めない）
      | この場所の端子数　　; 1端子／1部品（同名ラベルによる接続を除く）
      | 同階層同名ラベル数　; 75個（このラベル自身を含む）
      | 全階層の接続ラベル　; 87個（実際に同じノードへつながるラベル。名前が違う別名も含む）
      | 接続ルール　　　　　; 同じ階層の同じラベル名を仮想配線として結ぶ。別のSubsystem内とは名前だけでつながらず、明示的なConnection Portと配線をたどる。色は用途の表示であり接続を決めない。
      | 確認の範囲　　　　　; 現在の保存回路の端子・配線から求めた静的接続。抵抗やICの内部を導線として短絡せずに集計した。説明の更新は動作シミュレーション、タイミング、実部品の性能・実機動作を保証するものではない。
      | 記録の基準　　　　　; measurement_label_layout_20261022_r01/after_layout_graph.json。部品対応表は端子名の対応付けにのみ使用。
      | 
      | 【この説明欄の略語・記号】
      | 用語1　　　　　　　 ; DC：Direct Current（直流）。ここでは直流電源または直流成分。DCバイアスはコンデンサに重なる直流電圧を指す。
      | 用語2　　　　　　　 ; DC/DC：DC-to-DC Converter（直流電圧変換器）。直流入力を別の直流電圧へ変換する電源回路。絶縁の有無は個々の部品説明で確認する。
      | 用語3　　　　　　　 ; ADC：Analog-to-Digital Converter（アナログ・デジタル変換器）。測定電圧をデジタル値へ変換する回路。電流や温度も、センサーで電圧へ変換した後に読み取る。
      | 用語4　　　　　　　 ; IC：Integrated Circuit（集積回路）。複数の電子素子と機能を小さな半導体チップに集積した部品。
      | 用語5　　　　　　　 ; CH：Channel（測定チャネル）。CH0〜CH7はADCの入力番号であり、同時測定を意味しない。
      | 用語6　　　　　　　 ; MOSFET：Metal-Oxide-Semiconductor Field-Effect Transistor（金属・酸化膜・半導体構造の電界効果トランジスタ）。ゲートとソースの電圧でドレインとソースの導通を制御する素子。N-MOSはNチャネル型を表す。
      | 用語7　　　　　　　 ; LiFePO4：Lithium Iron Phosphate（リン酸鉄リチウム）。電池の正極材料を示す化学式。英語の頭文字を並べた略語ではない。
      | 用語8　　　　　　　 ; GND：Ground（回路の基準電位・電流帰路）。この図の共通基準。保護接地や大地への接続を意味するとは限らない。
      | 用語9　　　　　　　 ; AGND：Analog Ground（アナログ回路の基準端子）。アナログ部分の電流帰路。現図では共通GNDへ接続されるが、実装時の電流経路への配慮は別途必要。
      | 用語10　　　　　　　; DGND：Digital Ground（デジタル回路の基準端子）。デジタル部分の電流帰路。現図では共通GNDへ接続される。
      | 用語11　　　　　　　; VREF/REF：基準電圧を表す端子名。REFはReference（基準）の意味。ADCの変換尺度や電流アンプの出力基準に使う。REF1/REF2の接続電位は個別に確認する。
      | 用語12　　　　　　　; VCC/VDD/VEE/VS：ICの電源端子名。文字の歴史的な由来を現在の接続機能へ当てはめない。現回路のVEEはU8/U10では浮動基準SW、U9ではGND。各電圧・基準は端子と接続を参照する。
      | 用語13　　　　　　　; GNDP：U10の一次側電源の基準端子。絶縁電源の入力側GND。二次側基準VEE=SWと直接同一の導体ではない。
      | 用語14　　　　　　　; SW：Switching Node（スイッチング点）。主電力段の上下MOSFETとL1がつながる、電圧が高速に切り替わる点。GNDとは別電位。
  GND_Label_095 : ConnectionLabel  Description=|  Label=GND
      | この回路での名前　　; GND
      | 種別　　　　　　　　; ConnectionLabel
      | この回路での役割　　; 電池BT1の負極、太陽電池列の負極、制御・測定・保護回路のGNDを結ぶ共通の帰路。高側駆動の浮動帰路SWとは別のノード。
      | 共通帰路の代表接続　; BT1（充電先の蓄電池／51.2V 100Ah LiFePO4）: -
      |                     ; PV1（直列太陽電池列の負極側パネル／400W panel 1/2）: -
      |                     ; U7（RP2040搭載Pico W／SC0918）: 3(GND), 8(GND), 13(GND), 18(GND), 23(GND), 28(GND), 33(AGND), 38(GND)
      |                     ; U1（外付けADC／MCP3208-CI/SL）: 8(CH7), 9(DGND), 14(AGND)
      |                     ; P_U1（保護MOSFETを制御する保護IC／LTC4364IMS-1#PBF）: GND
      |                     ; Q2（同期整流降圧回路の下側スイッチ／TK9R6E15Q5,S1X）: 3(S)
      |                     ; U9（低側の光ゲートドライバ／ACPL-P346-560E）: 4(VEE)
      |                     ; U10（高側ゲート用の浮動電源を作る絶縁DC/DC／UCC14131QDWNRQ1）: 1(GNDP), 2(GNDP), 5(GNDP), 8(GNDP), 9(GNDP), 10(GNDP), 11(GNDP), 12(GNDP), 13(GNDP), 14(GNDP), 15(GNDP), 16(GNDP), 17(GNDP), 18(GNDP)
      | この場所の直接接続　; U7（RP2040搭載Pico W／SC0918）: 23(GND)
      | 直接接続の範囲　　　; このラベルから実際の線・分岐・明示的な境界端子だけを追った接続。同名ラベルによる離れた場所への接続はこの欄に含めない。
      | 同一ネット全端子　　; BT1: -
      |                     ; C1: 2(n)
      |                     ; C2: 2(n)
      |                     ; C3: 2(n)
      |                     ; C4: 2(n)
      |                     ; C7: 2(n)
      |                     ; C8: 2(n)
      |                     ; C9: 2(n)
      |                     ; C10: 2(n)
      |                     ; C13: 2(n)
      |                     ; C14: 2(n)
      |                     ; C15: 2(n)
      |                     ; C16: 2(n)
      |                     ; C17: 2
      |                     ; C18: 2
      |                     ; C19: 2
      |                     ; C20: 2
      |                     ; C21: 2
      |                     ; C22: 2
      |                     ; C23: 2
      |                     ; C24: 2
      |                     ; C25: 2
      |                     ; C26: 2
      |                     ; C27: 2
      |                     ; C28: 2
      |                     ; C29: 2
      |                     ; C30: 2
      |                     ; C31: 2
      |                     ; C33: 2
      |                     ; C34: 2
      |                     ; C35: 2
      |                     ; C36: 2
      |                     ; C40: 2
      |                     ; C41: 2
      |                     ; C42: 2
      |                     ; C43: 2
      |                     ; C44: 2
      |                     ; C45: 2
      |                     ; C46: 2
      |                     ; C47: 2
      |                     ; C48: 2
      |                     ; D2: 2(A)
      |                     ; PV1: -
      |                     ; P_CHG: N
      |                     ; P_COUT: N
      |                     ; P_CTMR: N
      |                     ; P_D1: A
      |                     ; P_R3: 2
      |                     ; P_R8: 2
      |                     ; P_RSHDN_PD: 2
      |                     ; P_U1: GND
      |                     ; Q2: 3(S)
      |                     ; Q3: 1(S1), 4(S2)
      |                     ; R1: 2(n)
      |                     ; R18: 2
      |                     ; R21: 2
      |                     ; R24: 2
      |                     ; R35: 2
      |                     ; R42: 2
      |                     ; R44: 2
      |                     ; R48: 2
      |                     ; U1: 8(CH7), 9(DGND), 14(AGND)
      |                     ; U2: 2(GND), 3(REF2), 4(RESERVED_GND)
      |                     ; U3: 2(GND), 3(REF2), 4(RESERVED_GND)
      |                     ; U4: 3(GND)
      |                     ; U5: 3(GND)
      |                     ; U6: 3(GND)
      |                     ; U7: 3(GND), 8(GND), 13(GND), 18(GND), 23(GND), 28(GND), 33(AGND), 38(GND)
      |                     ; U9: 4(VEE)
      |                     ; U10: 1(GNDP), 2(GNDP), 5(GNDP), 8(GNDP), 9(GNDP), 10(GNDP), 11(GNDP), 12(GNDP), 13(GNDP), 14(GNDP), 15(GNDP), 16(GNDP), 17(GNDP), 18(GNDP)
      |                     ; U11: 2(GND)
      |                     ; U12: 2(GND)
      | 接続部品数　　　　　; 72部品（部品番号で集計。同一ネット全体）
      | 接続端子数　　　　　; 99端子（423端子の部品対応表で集計。ラベル・境界ポートの重複は含めない）
      | この場所の端子数　　; 1端子／1部品（同名ラベルによる接続を除く）
      | 同階層同名ラベル数　; 75個（このラベル自身を含む）
      | 全階層の接続ラベル　; 87個（実際に同じノードへつながるラベル。名前が違う別名も含む）
      | 接続ルール　　　　　; 同じ階層の同じラベル名を仮想配線として結ぶ。別のSubsystem内とは名前だけでつながらず、明示的なConnection Portと配線をたどる。色は用途の表示であり接続を決めない。
      | 確認の範囲　　　　　; 現在の保存回路の端子・配線から求めた静的接続。抵抗やICの内部を導線として短絡せずに集計した。説明の更新は動作シミュレーション、タイミング、実部品の性能・実機動作を保証するものではない。
      | 記録の基準　　　　　; measurement_label_layout_20261022_r01/after_layout_graph.json。部品対応表は端子名の対応付けにのみ使用。
      | 
      | 【この説明欄の略語・記号】
      | 用語1　　　　　　　 ; DC：Direct Current（直流）。ここでは直流電源または直流成分。DCバイアスはコンデンサに重なる直流電圧を指す。
      | 用語2　　　　　　　 ; DC/DC：DC-to-DC Converter（直流電圧変換器）。直流入力を別の直流電圧へ変換する電源回路。絶縁の有無は個々の部品説明で確認する。
      | 用語3　　　　　　　 ; ADC：Analog-to-Digital Converter（アナログ・デジタル変換器）。測定電圧をデジタル値へ変換する回路。電流や温度も、センサーで電圧へ変換した後に読み取る。
      | 用語4　　　　　　　 ; IC：Integrated Circuit（集積回路）。複数の電子素子と機能を小さな半導体チップに集積した部品。
      | 用語5　　　　　　　 ; CH：Channel（測定チャネル）。CH0〜CH7はADCの入力番号であり、同時測定を意味しない。
      | 用語6　　　　　　　 ; MOSFET：Metal-Oxide-Semiconductor Field-Effect Transistor（金属・酸化膜・半導体構造の電界効果トランジスタ）。ゲートとソースの電圧でドレインとソースの導通を制御する素子。N-MOSはNチャネル型を表す。
      | 用語7　　　　　　　 ; LiFePO4：Lithium Iron Phosphate（リン酸鉄リチウム）。電池の正極材料を示す化学式。英語の頭文字を並べた略語ではない。
      | 用語8　　　　　　　 ; GND：Ground（回路の基準電位・電流帰路）。この図の共通基準。保護接地や大地への接続を意味するとは限らない。
      | 用語9　　　　　　　 ; AGND：Analog Ground（アナログ回路の基準端子）。アナログ部分の電流帰路。現図では共通GNDへ接続されるが、実装時の電流経路への配慮は別途必要。
      | 用語10　　　　　　　; DGND：Digital Ground（デジタル回路の基準端子）。デジタル部分の電流帰路。現図では共通GNDへ接続される。
      | 用語11　　　　　　　; VREF/REF：基準電圧を表す端子名。REFはReference（基準）の意味。ADCの変換尺度や電流アンプの出力基準に使う。REF1/REF2の接続電位は個別に確認する。
      | 用語12　　　　　　　; VCC/VDD/VEE/VS：ICの電源端子名。文字の歴史的な由来を現在の接続機能へ当てはめない。現回路のVEEはU8/U10では浮動基準SW、U9ではGND。各電圧・基準は端子と接続を参照する。
      | 用語13　　　　　　　; GNDP：U10の一次側電源の基準端子。絶縁電源の入力側GND。二次側基準VEE=SWと直接同一の導体ではない。
      | 用語14　　　　　　　; SW：Switching Node（スイッチング点）。主電力段の上下MOSFETとL1がつながる、電圧が高速に切り替わる点。GNDとは別電位。
  GND_Label_096 : ConnectionLabel  Description=|  Label=GND
      | この回路での名前　　; GND
      | 種別　　　　　　　　; ConnectionLabel
      | この回路での役割　　; 電池BT1の負極、太陽電池列の負極、制御・測定・保護回路のGNDを結ぶ共通の帰路。高側駆動の浮動帰路SWとは別のノード。
      | 共通帰路の代表接続　; BT1（充電先の蓄電池／51.2V 100Ah LiFePO4）: -
      |                     ; PV1（直列太陽電池列の負極側パネル／400W panel 1/2）: -
      |                     ; U7（RP2040搭載Pico W／SC0918）: 3(GND), 8(GND), 13(GND), 18(GND), 23(GND), 28(GND), 33(AGND), 38(GND)
      |                     ; U1（外付けADC／MCP3208-CI/SL）: 8(CH7), 9(DGND), 14(AGND)
      |                     ; P_U1（保護MOSFETを制御する保護IC／LTC4364IMS-1#PBF）: GND
      |                     ; Q2（同期整流降圧回路の下側スイッチ／TK9R6E15Q5,S1X）: 3(S)
      |                     ; U9（低側の光ゲートドライバ／ACPL-P346-560E）: 4(VEE)
      |                     ; U10（高側ゲート用の浮動電源を作る絶縁DC/DC／UCC14131QDWNRQ1）: 1(GNDP), 2(GNDP), 5(GNDP), 8(GNDP), 9(GNDP), 10(GNDP), 11(GNDP), 12(GNDP), 13(GNDP), 14(GNDP), 15(GNDP), 16(GNDP), 17(GNDP), 18(GNDP)
      | この場所の直接接続　; U7（RP2040搭載Pico W／SC0918）: 28(GND)
      | 直接接続の範囲　　　; このラベルから実際の線・分岐・明示的な境界端子だけを追った接続。同名ラベルによる離れた場所への接続はこの欄に含めない。
      | 同一ネット全端子　　; BT1: -
      |                     ; C1: 2(n)
      |                     ; C2: 2(n)
      |                     ; C3: 2(n)
      |                     ; C4: 2(n)
      |                     ; C7: 2(n)
      |                     ; C8: 2(n)
      |                     ; C9: 2(n)
      |                     ; C10: 2(n)
      |                     ; C13: 2(n)
      |                     ; C14: 2(n)
      |                     ; C15: 2(n)
      |                     ; C16: 2(n)
      |                     ; C17: 2
      |                     ; C18: 2
      |                     ; C19: 2
      |                     ; C20: 2
      |                     ; C21: 2
      |                     ; C22: 2
      |                     ; C23: 2
      |                     ; C24: 2
      |                     ; C25: 2
      |                     ; C26: 2
      |                     ; C27: 2
      |                     ; C28: 2
      |                     ; C29: 2
      |                     ; C30: 2
      |                     ; C31: 2
      |                     ; C33: 2
      |                     ; C34: 2
      |                     ; C35: 2
      |                     ; C36: 2
      |                     ; C40: 2
      |                     ; C41: 2
      |                     ; C42: 2
      |                     ; C43: 2
      |                     ; C44: 2
      |                     ; C45: 2
      |                     ; C46: 2
      |                     ; C47: 2
      |                     ; C48: 2
      |                     ; D2: 2(A)
      |                     ; PV1: -
      |                     ; P_CHG: N
      |                     ; P_COUT: N
      |                     ; P_CTMR: N
      |                     ; P_D1: A
      |                     ; P_R3: 2
      |                     ; P_R8: 2
      |                     ; P_RSHDN_PD: 2
      |                     ; P_U1: GND
      |                     ; Q2: 3(S)
      |                     ; Q3: 1(S1), 4(S2)
      |                     ; R1: 2(n)
      |                     ; R18: 2
      |                     ; R21: 2
      |                     ; R24: 2
      |                     ; R35: 2
      |                     ; R42: 2
      |                     ; R44: 2
      |                     ; R48: 2
      |                     ; U1: 8(CH7), 9(DGND), 14(AGND)
      |                     ; U2: 2(GND), 3(REF2), 4(RESERVED_GND)
      |                     ; U3: 2(GND), 3(REF2), 4(RESERVED_GND)
      |                     ; U4: 3(GND)
      |                     ; U5: 3(GND)
      |                     ; U6: 3(GND)
      |                     ; U7: 3(GND), 8(GND), 13(GND), 18(GND), 23(GND), 28(GND), 33(AGND), 38(GND)
      |                     ; U9: 4(VEE)
      |                     ; U10: 1(GNDP), 2(GNDP), 5(GNDP), 8(GNDP), 9(GNDP), 10(GNDP), 11(GNDP), 12(GNDP), 13(GNDP), 14(GNDP), 15(GNDP), 16(GNDP), 17(GNDP), 18(GNDP)
      |                     ; U11: 2(GND)
      |                     ; U12: 2(GND)
      | 接続部品数　　　　　; 72部品（部品番号で集計。同一ネット全体）
      | 接続端子数　　　　　; 99端子（423端子の部品対応表で集計。ラベル・境界ポートの重複は含めない）
      | この場所の端子数　　; 1端子／1部品（同名ラベルによる接続を除く）
      | 同階層同名ラベル数　; 75個（このラベル自身を含む）
      | 全階層の接続ラベル　; 87個（実際に同じノードへつながるラベル。名前が違う別名も含む）
      | 接続ルール　　　　　; 同じ階層の同じラベル名を仮想配線として結ぶ。別のSubsystem内とは名前だけでつながらず、明示的なConnection Portと配線をたどる。色は用途の表示であり接続を決めない。
      | 確認の範囲　　　　　; 現在の保存回路の端子・配線から求めた静的接続。抵抗やICの内部を導線として短絡せずに集計した。説明の更新は動作シミュレーション、タイミング、実部品の性能・実機動作を保証するものではない。
      | 記録の基準　　　　　; measurement_label_layout_20261022_r01/after_layout_graph.json。部品対応表は端子名の対応付けにのみ使用。
      | 
      | 【この説明欄の略語・記号】
      | 用語1　　　　　　　 ; DC：Direct Current（直流）。ここでは直流電源または直流成分。DCバイアスはコンデンサに重なる直流電圧を指す。
      | 用語2　　　　　　　 ; DC/DC：DC-to-DC Converter（直流電圧変換器）。直流入力を別の直流電圧へ変換する電源回路。絶縁の有無は個々の部品説明で確認する。
      | 用語3　　　　　　　 ; ADC：Analog-to-Digital Converter（アナログ・デジタル変換器）。測定電圧をデジタル値へ変換する回路。電流や温度も、センサーで電圧へ変換した後に読み取る。
      | 用語4　　　　　　　 ; IC：Integrated Circuit（集積回路）。複数の電子素子と機能を小さな半導体チップに集積した部品。
      | 用語5　　　　　　　 ; CH：Channel（測定チャネル）。CH0〜CH7はADCの入力番号であり、同時測定を意味しない。
      | 用語6　　　　　　　 ; MOSFET：Metal-Oxide-Semiconductor Field-Effect Transistor（金属・酸化膜・半導体構造の電界効果トランジスタ）。ゲートとソースの電圧でドレインとソースの導通を制御する素子。N-MOSはNチャネル型を表す。
      | 用語7　　　　　　　 ; LiFePO4：Lithium Iron Phosphate（リン酸鉄リチウム）。電池の正極材料を示す化学式。英語の頭文字を並べた略語ではない。
      | 用語8　　　　　　　 ; GND：Ground（回路の基準電位・電流帰路）。この図の共通基準。保護接地や大地への接続を意味するとは限らない。
      | 用語9　　　　　　　 ; AGND：Analog Ground（アナログ回路の基準端子）。アナログ部分の電流帰路。現図では共通GNDへ接続されるが、実装時の電流経路への配慮は別途必要。
      | 用語10　　　　　　　; DGND：Digital Ground（デジタル回路の基準端子）。デジタル部分の電流帰路。現図では共通GNDへ接続される。
      | 用語11　　　　　　　; VREF/REF：基準電圧を表す端子名。REFはReference（基準）の意味。ADCの変換尺度や電流アンプの出力基準に使う。REF1/REF2の接続電位は個別に確認する。
      | 用語12　　　　　　　; VCC/VDD/VEE/VS：ICの電源端子名。文字の歴史的な由来を現在の接続機能へ当てはめない。現回路のVEEはU8/U10では浮動基準SW、U9ではGND。各電圧・基準は端子と接続を参照する。
      | 用語13　　　　　　　; GNDP：U10の一次側電源の基準端子。絶縁電源の入力側GND。二次側基準VEE=SWと直接同一の導体ではない。
      | 用語14　　　　　　　; SW：Switching Node（スイッチング点）。主電力段の上下MOSFETとL1がつながる、電圧が高速に切り替わる点。GNDとは別電位。
  GND_Label_097 : ConnectionLabel  Description=|  Label=GND
      | この回路での名前　　; GND
      | 種別　　　　　　　　; ConnectionLabel
      | この回路での役割　　; 電池BT1の負極、太陽電池列の負極、制御・測定・保護回路のGNDを結ぶ共通の帰路。高側駆動の浮動帰路SWとは別のノード。
      | 共通帰路の代表接続　; BT1（充電先の蓄電池／51.2V 100Ah LiFePO4）: -
      |                     ; PV1（直列太陽電池列の負極側パネル／400W panel 1/2）: -
      |                     ; U7（RP2040搭載Pico W／SC0918）: 3(GND), 8(GND), 13(GND), 18(GND), 23(GND), 28(GND), 33(AGND), 38(GND)
      |                     ; U1（外付けADC／MCP3208-CI/SL）: 8(CH7), 9(DGND), 14(AGND)
      |                     ; P_U1（保護MOSFETを制御する保護IC／LTC4364IMS-1#PBF）: GND
      |                     ; Q2（同期整流降圧回路の下側スイッチ／TK9R6E15Q5,S1X）: 3(S)
      |                     ; U9（低側の光ゲートドライバ／ACPL-P346-560E）: 4(VEE)
      |                     ; U10（高側ゲート用の浮動電源を作る絶縁DC/DC／UCC14131QDWNRQ1）: 1(GNDP), 2(GNDP), 5(GNDP), 8(GNDP), 9(GNDP), 10(GNDP), 11(GNDP), 12(GNDP), 13(GNDP), 14(GNDP), 15(GNDP), 16(GNDP), 17(GNDP), 18(GNDP)
      | この場所の直接接続　; U7（RP2040搭載Pico W／SC0918）: 33(AGND)
      | 直接接続の範囲　　　; このラベルから実際の線・分岐・明示的な境界端子だけを追った接続。同名ラベルによる離れた場所への接続はこの欄に含めない。
      | 同一ネット全端子　　; BT1: -
      |                     ; C1: 2(n)
      |                     ; C2: 2(n)
      |                     ; C3: 2(n)
      |                     ; C4: 2(n)
      |                     ; C7: 2(n)
      |                     ; C8: 2(n)
      |                     ; C9: 2(n)
      |                     ; C10: 2(n)
      |                     ; C13: 2(n)
      |                     ; C14: 2(n)
      |                     ; C15: 2(n)
      |                     ; C16: 2(n)
      |                     ; C17: 2
      |                     ; C18: 2
      |                     ; C19: 2
      |                     ; C20: 2
      |                     ; C21: 2
      |                     ; C22: 2
      |                     ; C23: 2
      |                     ; C24: 2
      |                     ; C25: 2
      |                     ; C26: 2
      |                     ; C27: 2
      |                     ; C28: 2
      |                     ; C29: 2
      |                     ; C30: 2
      |                     ; C31: 2
      |                     ; C33: 2
      |                     ; C34: 2
      |                     ; C35: 2
      |                     ; C36: 2
      |                     ; C40: 2
      |                     ; C41: 2
      |                     ; C42: 2
      |                     ; C43: 2
      |                     ; C44: 2
      |                     ; C45: 2
      |                     ; C46: 2
      |                     ; C47: 2
      |                     ; C48: 2
      |                     ; D2: 2(A)
      |                     ; PV1: -
      |                     ; P_CHG: N
      |                     ; P_COUT: N
      |                     ; P_CTMR: N
      |                     ; P_D1: A
      |                     ; P_R3: 2
      |                     ; P_R8: 2
      |                     ; P_RSHDN_PD: 2
      |                     ; P_U1: GND
      |                     ; Q2: 3(S)
      |                     ; Q3: 1(S1), 4(S2)
      |                     ; R1: 2(n)
      |                     ; R18: 2
      |                     ; R21: 2
      |                     ; R24: 2
      |                     ; R35: 2
      |                     ; R42: 2
      |                     ; R44: 2
      |                     ; R48: 2
      |                     ; U1: 8(CH7), 9(DGND), 14(AGND)
      |                     ; U2: 2(GND), 3(REF2), 4(RESERVED_GND)
      |                     ; U3: 2(GND), 3(REF2), 4(RESERVED_GND)
      |                     ; U4: 3(GND)
      |                     ; U5: 3(GND)
      |                     ; U6: 3(GND)
      |                     ; U7: 3(GND), 8(GND), 13(GND), 18(GND), 23(GND), 28(GND), 33(AGND), 38(GND)
      |                     ; U9: 4(VEE)
      |                     ; U10: 1(GNDP), 2(GNDP), 5(GNDP), 8(GNDP), 9(GNDP), 10(GNDP), 11(GNDP), 12(GNDP), 13(GNDP), 14(GNDP), 15(GNDP), 16(GNDP), 17(GNDP), 18(GNDP)
      |                     ; U11: 2(GND)
      |                     ; U12: 2(GND)
      | 接続部品数　　　　　; 72部品（部品番号で集計。同一ネット全体）
      | 接続端子数　　　　　; 99端子（423端子の部品対応表で集計。ラベル・境界ポートの重複は含めない）
      | この場所の端子数　　; 1端子／1部品（同名ラベルによる接続を除く）
      | 同階層同名ラベル数　; 75個（このラベル自身を含む）
      | 全階層の接続ラベル　; 87個（実際に同じノードへつながるラベル。名前が違う別名も含む）
      | 接続ルール　　　　　; 同じ階層の同じラベル名を仮想配線として結ぶ。別のSubsystem内とは名前だけでつながらず、明示的なConnection Portと配線をたどる。色は用途の表示であり接続を決めない。
      | 確認の範囲　　　　　; 現在の保存回路の端子・配線から求めた静的接続。抵抗やICの内部を導線として短絡せずに集計した。説明の更新は動作シミュレーション、タイミング、実部品の性能・実機動作を保証するものではない。
      | 記録の基準　　　　　; measurement_label_layout_20261022_r01/after_layout_graph.json。部品対応表は端子名の対応付けにのみ使用。
      | 
      | 【この説明欄の略語・記号】
      | 用語1　　　　　　　 ; DC：Direct Current（直流）。ここでは直流電源または直流成分。DCバイアスはコンデンサに重なる直流電圧を指す。
      | 用語2　　　　　　　 ; DC/DC：DC-to-DC Converter（直流電圧変換器）。直流入力を別の直流電圧へ変換する電源回路。絶縁の有無は個々の部品説明で確認する。
      | 用語3　　　　　　　 ; ADC：Analog-to-Digital Converter（アナログ・デジタル変換器）。測定電圧をデジタル値へ変換する回路。電流や温度も、センサーで電圧へ変換した後に読み取る。
      | 用語4　　　　　　　 ; IC：Integrated Circuit（集積回路）。複数の電子素子と機能を小さな半導体チップに集積した部品。
      | 用語5　　　　　　　 ; CH：Channel（測定チャネル）。CH0〜CH7はADCの入力番号であり、同時測定を意味しない。
      | 用語6　　　　　　　 ; MOSFET：Metal-Oxide-Semiconductor Field-Effect Transistor（金属・酸化膜・半導体構造の電界効果トランジスタ）。ゲートとソースの電圧でドレインとソースの導通を制御する素子。N-MOSはNチャネル型を表す。
      | 用語7　　　　　　　 ; LiFePO4：Lithium Iron Phosphate（リン酸鉄リチウム）。電池の正極材料を示す化学式。英語の頭文字を並べた略語ではない。
      | 用語8　　　　　　　 ; GND：Ground（回路の基準電位・電流帰路）。この図の共通基準。保護接地や大地への接続を意味するとは限らない。
      | 用語9　　　　　　　 ; AGND：Analog Ground（アナログ回路の基準端子）。アナログ部分の電流帰路。現図では共通GNDへ接続されるが、実装時の電流経路への配慮は別途必要。
      | 用語10　　　　　　　; DGND：Digital Ground（デジタル回路の基準端子）。デジタル部分の電流帰路。現図では共通GNDへ接続される。
      | 用語11　　　　　　　; VREF/REF：基準電圧を表す端子名。REFはReference（基準）の意味。ADCの変換尺度や電流アンプの出力基準に使う。REF1/REF2の接続電位は個別に確認する。
      | 用語12　　　　　　　; VCC/VDD/VEE/VS：ICの電源端子名。文字の歴史的な由来を現在の接続機能へ当てはめない。現回路のVEEはU8/U10では浮動基準SW、U9ではGND。各電圧・基準は端子と接続を参照する。
      | 用語13　　　　　　　; GNDP：U10の一次側電源の基準端子。絶縁電源の入力側GND。二次側基準VEE=SWと直接同一の導体ではない。
      | 用語14　　　　　　　; SW：Switching Node（スイッチング点）。主電力段の上下MOSFETとL1がつながる、電圧が高速に切り替わる点。GNDとは別電位。
  GND_Label_098 : ConnectionLabel  Description=|  Label=GND
      | この回路での名前　　; GND
      | 種別　　　　　　　　; ConnectionLabel
      | この回路での役割　　; 電池BT1の負極、太陽電池列の負極、制御・測定・保護回路のGNDを結ぶ共通の帰路。高側駆動の浮動帰路SWとは別のノード。
      | 共通帰路の代表接続　; BT1（充電先の蓄電池／51.2V 100Ah LiFePO4）: -
      |                     ; PV1（直列太陽電池列の負極側パネル／400W panel 1/2）: -
      |                     ; U7（RP2040搭載Pico W／SC0918）: 3(GND), 8(GND), 13(GND), 18(GND), 23(GND), 28(GND), 33(AGND), 38(GND)
      |                     ; U1（外付けADC／MCP3208-CI/SL）: 8(CH7), 9(DGND), 14(AGND)
      |                     ; P_U1（保護MOSFETを制御する保護IC／LTC4364IMS-1#PBF）: GND
      |                     ; Q2（同期整流降圧回路の下側スイッチ／TK9R6E15Q5,S1X）: 3(S)
      |                     ; U9（低側の光ゲートドライバ／ACPL-P346-560E）: 4(VEE)
      |                     ; U10（高側ゲート用の浮動電源を作る絶縁DC/DC／UCC14131QDWNRQ1）: 1(GNDP), 2(GNDP), 5(GNDP), 8(GNDP), 9(GNDP), 10(GNDP), 11(GNDP), 12(GNDP), 13(GNDP), 14(GNDP), 15(GNDP), 16(GNDP), 17(GNDP), 18(GNDP)
      | この場所の直接接続　; U7（RP2040搭載Pico W／SC0918）: 38(GND)
      | 直接接続の範囲　　　; このラベルから実際の線・分岐・明示的な境界端子だけを追った接続。同名ラベルによる離れた場所への接続はこの欄に含めない。
      | 同一ネット全端子　　; BT1: -
      |                     ; C1: 2(n)
      |                     ; C2: 2(n)
      |                     ; C3: 2(n)
      |                     ; C4: 2(n)
      |                     ; C7: 2(n)
      |                     ; C8: 2(n)
      |                     ; C9: 2(n)
      |                     ; C10: 2(n)
      |                     ; C13: 2(n)
      |                     ; C14: 2(n)
      |                     ; C15: 2(n)
      |                     ; C16: 2(n)
      |                     ; C17: 2
      |                     ; C18: 2
      |                     ; C19: 2
      |                     ; C20: 2
      |                     ; C21: 2
      |                     ; C22: 2
      |                     ; C23: 2
      |                     ; C24: 2
      |                     ; C25: 2
      |                     ; C26: 2
      |                     ; C27: 2
      |                     ; C28: 2
      |                     ; C29: 2
      |                     ; C30: 2
      |                     ; C31: 2
      |                     ; C33: 2
      |                     ; C34: 2
      |                     ; C35: 2
      |                     ; C36: 2
      |                     ; C40: 2
      |                     ; C41: 2
      |                     ; C42: 2
      |                     ; C43: 2
      |                     ; C44: 2
      |                     ; C45: 2
      |                     ; C46: 2
      |                     ; C47: 2
      |                     ; C48: 2
      |                     ; D2: 2(A)
      |                     ; PV1: -
      |                     ; P_CHG: N
      |                     ; P_COUT: N
      |                     ; P_CTMR: N
      |                     ; P_D1: A
      |                     ; P_R3: 2
      |                     ; P_R8: 2
      |                     ; P_RSHDN_PD: 2
      |                     ; P_U1: GND
      |                     ; Q2: 3(S)
      |                     ; Q3: 1(S1), 4(S2)
      |                     ; R1: 2(n)
      |                     ; R18: 2
      |                     ; R21: 2
      |                     ; R24: 2
      |                     ; R35: 2
      |                     ; R42: 2
      |                     ; R44: 2
      |                     ; R48: 2
      |                     ; U1: 8(CH7), 9(DGND), 14(AGND)
      |                     ; U2: 2(GND), 3(REF2), 4(RESERVED_GND)
      |                     ; U3: 2(GND), 3(REF2), 4(RESERVED_GND)
      |                     ; U4: 3(GND)
      |                     ; U5: 3(GND)
      |                     ; U6: 3(GND)
      |                     ; U7: 3(GND), 8(GND), 13(GND), 18(GND), 23(GND), 28(GND), 33(AGND), 38(GND)
      |                     ; U9: 4(VEE)
      |                     ; U10: 1(GNDP), 2(GNDP), 5(GNDP), 8(GNDP), 9(GNDP), 10(GNDP), 11(GNDP), 12(GNDP), 13(GNDP), 14(GNDP), 15(GNDP), 16(GNDP), 17(GNDP), 18(GNDP)
      |                     ; U11: 2(GND)
      |                     ; U12: 2(GND)
      | 接続部品数　　　　　; 72部品（部品番号で集計。同一ネット全体）
      | 接続端子数　　　　　; 99端子（423端子の部品対応表で集計。ラベル・境界ポートの重複は含めない）
      | この場所の端子数　　; 1端子／1部品（同名ラベルによる接続を除く）
      | 同階層同名ラベル数　; 75個（このラベル自身を含む）
      | 全階層の接続ラベル　; 87個（実際に同じノードへつながるラベル。名前が違う別名も含む）
      | 接続ルール　　　　　; 同じ階層の同じラベル名を仮想配線として結ぶ。別のSubsystem内とは名前だけでつながらず、明示的なConnection Portと配線をたどる。色は用途の表示であり接続を決めない。
      | 確認の範囲　　　　　; 現在の保存回路の端子・配線から求めた静的接続。抵抗やICの内部を導線として短絡せずに集計した。説明の更新は動作シミュレーション、タイミング、実部品の性能・実機動作を保証するものではない。
      | 記録の基準　　　　　; measurement_label_layout_20261022_r01/after_layout_graph.json。部品対応表は端子名の対応付けにのみ使用。
      | 
      | 【この説明欄の略語・記号】
      | 用語1　　　　　　　 ; DC：Direct Current（直流）。ここでは直流電源または直流成分。DCバイアスはコンデンサに重なる直流電圧を指す。
      | 用語2　　　　　　　 ; DC/DC：DC-to-DC Converter（直流電圧変換器）。直流入力を別の直流電圧へ変換する電源回路。絶縁の有無は個々の部品説明で確認する。
      | 用語3　　　　　　　 ; ADC：Analog-to-Digital Converter（アナログ・デジタル変換器）。測定電圧をデジタル値へ変換する回路。電流や温度も、センサーで電圧へ変換した後に読み取る。
      | 用語4　　　　　　　 ; IC：Integrated Circuit（集積回路）。複数の電子素子と機能を小さな半導体チップに集積した部品。
      | 用語5　　　　　　　 ; CH：Channel（測定チャネル）。CH0〜CH7はADCの入力番号であり、同時測定を意味しない。
      | 用語6　　　　　　　 ; MOSFET：Metal-Oxide-Semiconductor Field-Effect Transistor（金属・酸化膜・半導体構造の電界効果トランジスタ）。ゲートとソースの電圧でドレインとソースの導通を制御する素子。N-MOSはNチャネル型を表す。
      | 用語7　　　　　　　 ; LiFePO4：Lithium Iron Phosphate（リン酸鉄リチウム）。電池の正極材料を示す化学式。英語の頭文字を並べた略語ではない。
      | 用語8　　　　　　　 ; GND：Ground（回路の基準電位・電流帰路）。この図の共通基準。保護接地や大地への接続を意味するとは限らない。
      | 用語9　　　　　　　 ; AGND：Analog Ground（アナログ回路の基準端子）。アナログ部分の電流帰路。現図では共通GNDへ接続されるが、実装時の電流経路への配慮は別途必要。
      | 用語10　　　　　　　; DGND：Digital Ground（デジタル回路の基準端子）。デジタル部分の電流帰路。現図では共通GNDへ接続される。
      | 用語11　　　　　　　; VREF/REF：基準電圧を表す端子名。REFはReference（基準）の意味。ADCの変換尺度や電流アンプの出力基準に使う。REF1/REF2の接続電位は個別に確認する。
      | 用語12　　　　　　　; VCC/VDD/VEE/VS：ICの電源端子名。文字の歴史的な由来を現在の接続機能へ当てはめない。現回路のVEEはU8/U10では浮動基準SW、U9ではGND。各電圧・基準は端子と接続を参照する。
      | 用語13　　　　　　　; GNDP：U10の一次側電源の基準端子。絶縁電源の入力側GND。二次側基準VEE=SWと直接同一の導体ではない。
      | 用語14　　　　　　　; SW：Switching Node（スイッチング点）。主電力段の上下MOSFETとL1がつながる、電圧が高速に切り替わる点。GNDとは別電位。
  GND_Label_099 : ConnectionLabel  Description=|  Label=GND
      | この回路での名前　　; GND
      | 種別　　　　　　　　; ConnectionLabel
      | この回路での役割　　; 電池BT1の負極、太陽電池列の負極、制御・測定・保護回路のGNDを結ぶ共通の帰路。高側駆動の浮動帰路SWとは別のノード。
      | 共通帰路の代表接続　; BT1（充電先の蓄電池／51.2V 100Ah LiFePO4）: -
      |                     ; PV1（直列太陽電池列の負極側パネル／400W panel 1/2）: -
      |                     ; U7（RP2040搭載Pico W／SC0918）: 3(GND), 8(GND), 13(GND), 18(GND), 23(GND), 28(GND), 33(AGND), 38(GND)
      |                     ; U1（外付けADC／MCP3208-CI/SL）: 8(CH7), 9(DGND), 14(AGND)
      |                     ; P_U1（保護MOSFETを制御する保護IC／LTC4364IMS-1#PBF）: GND
      |                     ; Q2（同期整流降圧回路の下側スイッチ／TK9R6E15Q5,S1X）: 3(S)
      |                     ; U9（低側の光ゲートドライバ／ACPL-P346-560E）: 4(VEE)
      |                     ; U10（高側ゲート用の浮動電源を作る絶縁DC/DC／UCC14131QDWNRQ1）: 1(GNDP), 2(GNDP), 5(GNDP), 8(GNDP), 9(GNDP), 10(GNDP), 11(GNDP), 12(GNDP), 13(GNDP), 14(GNDP), 15(GNDP), 16(GNDP), 17(GNDP), 18(GNDP)
      | この場所の直接接続　; U9（低側の光ゲートドライバ／ACPL-P346-560E）: 4(VEE)
      | 直接接続の範囲　　　; このラベルから実際の線・分岐・明示的な境界端子だけを追った接続。同名ラベルによる離れた場所への接続はこの欄に含めない。
      | 同一ネット全端子　　; BT1: -
      |                     ; C1: 2(n)
      |                     ; C2: 2(n)
      |                     ; C3: 2(n)
      |                     ; C4: 2(n)
      |                     ; C7: 2(n)
      |                     ; C8: 2(n)
      |                     ; C9: 2(n)
      |                     ; C10: 2(n)
      |                     ; C13: 2(n)
      |                     ; C14: 2(n)
      |                     ; C15: 2(n)
      |                     ; C16: 2(n)
      |                     ; C17: 2
      |                     ; C18: 2
      |                     ; C19: 2
      |                     ; C20: 2
      |                     ; C21: 2
      |                     ; C22: 2
      |                     ; C23: 2
      |                     ; C24: 2
      |                     ; C25: 2
      |                     ; C26: 2
      |                     ; C27: 2
      |                     ; C28: 2
      |                     ; C29: 2
      |                     ; C30: 2
      |                     ; C31: 2
      |                     ; C33: 2
      |                     ; C34: 2
      |                     ; C35: 2
      |                     ; C36: 2
      |                     ; C40: 2
      |                     ; C41: 2
      |                     ; C42: 2
      |                     ; C43: 2
      |                     ; C44: 2
      |                     ; C45: 2
      |                     ; C46: 2
      |                     ; C47: 2
      |                     ; C48: 2
      |                     ; D2: 2(A)
      |                     ; PV1: -
      |                     ; P_CHG: N
      |                     ; P_COUT: N
      |                     ; P_CTMR: N
      |                     ; P_D1: A
      |                     ; P_R3: 2
      |                     ; P_R8: 2
      |                     ; P_RSHDN_PD: 2
      |                     ; P_U1: GND
      |                     ; Q2: 3(S)
      |                     ; Q3: 1(S1), 4(S2)
      |                     ; R1: 2(n)
      |                     ; R18: 2
      |                     ; R21: 2
      |                     ; R24: 2
      |                     ; R35: 2
      |                     ; R42: 2
      |                     ; R44: 2
      |                     ; R48: 2
      |                     ; U1: 8(CH7), 9(DGND), 14(AGND)
      |                     ; U2: 2(GND), 3(REF2), 4(RESERVED_GND)
      |                     ; U3: 2(GND), 3(REF2), 4(RESERVED_GND)
      |                     ; U4: 3(GND)
      |                     ; U5: 3(GND)
      |                     ; U6: 3(GND)
      |                     ; U7: 3(GND), 8(GND), 13(GND), 18(GND), 23(GND), 28(GND), 33(AGND), 38(GND)
      |                     ; U9: 4(VEE)
      |                     ; U10: 1(GNDP), 2(GNDP), 5(GNDP), 8(GNDP), 9(GNDP), 10(GNDP), 11(GNDP), 12(GNDP), 13(GNDP), 14(GNDP), 15(GNDP), 16(GNDP), 17(GNDP), 18(GNDP)
      |                     ; U11: 2(GND)
      |                     ; U12: 2(GND)
      | 接続部品数　　　　　; 72部品（部品番号で集計。同一ネット全体）
      | 接続端子数　　　　　; 99端子（423端子の部品対応表で集計。ラベル・境界ポートの重複は含めない）
      | この場所の端子数　　; 1端子／1部品（同名ラベルによる接続を除く）
      | 同階層同名ラベル数　; 75個（このラベル自身を含む）
      | 全階層の接続ラベル　; 87個（実際に同じノードへつながるラベル。名前が違う別名も含む）
      | 接続ルール　　　　　; 同じ階層の同じラベル名を仮想配線として結ぶ。別のSubsystem内とは名前だけでつながらず、明示的なConnection Portと配線をたどる。色は用途の表示であり接続を決めない。
      | 確認の範囲　　　　　; 現在の保存回路の端子・配線から求めた静的接続。抵抗やICの内部を導線として短絡せずに集計した。説明の更新は動作シミュレーション、タイミング、実部品の性能・実機動作を保証するものではない。
      | 記録の基準　　　　　; measurement_label_layout_20261022_r01/after_layout_graph.json。部品対応表は端子名の対応付けにのみ使用。
      | 
      | 【この説明欄の略語・記号】
      | 用語1　　　　　　　 ; DC：Direct Current（直流）。ここでは直流電源または直流成分。DCバイアスはコンデンサに重なる直流電圧を指す。
      | 用語2　　　　　　　 ; DC/DC：DC-to-DC Converter（直流電圧変換器）。直流入力を別の直流電圧へ変換する電源回路。絶縁の有無は個々の部品説明で確認する。
      | 用語3　　　　　　　 ; ADC：Analog-to-Digital Converter（アナログ・デジタル変換器）。測定電圧をデジタル値へ変換する回路。電流や温度も、センサーで電圧へ変換した後に読み取る。
      | 用語4　　　　　　　 ; IC：Integrated Circuit（集積回路）。複数の電子素子と機能を小さな半導体チップに集積した部品。
      | 用語5　　　　　　　 ; CH：Channel（測定チャネル）。CH0〜CH7はADCの入力番号であり、同時測定を意味しない。
      | 用語6　　　　　　　 ; MOSFET：Metal-Oxide-Semiconductor Field-Effect Transistor（金属・酸化膜・半導体構造の電界効果トランジスタ）。ゲートとソースの電圧でドレインとソースの導通を制御する素子。N-MOSはNチャネル型を表す。
      | 用語7　　　　　　　 ; LiFePO4：Lithium Iron Phosphate（リン酸鉄リチウム）。電池の正極材料を示す化学式。英語の頭文字を並べた略語ではない。
      | 用語8　　　　　　　 ; GND：Ground（回路の基準電位・電流帰路）。この図の共通基準。保護接地や大地への接続を意味するとは限らない。
      | 用語9　　　　　　　 ; AGND：Analog Ground（アナログ回路の基準端子）。アナログ部分の電流帰路。現図では共通GNDへ接続されるが、実装時の電流経路への配慮は別途必要。
      | 用語10　　　　　　　; DGND：Digital Ground（デジタル回路の基準端子）。デジタル部分の電流帰路。現図では共通GNDへ接続される。
      | 用語11　　　　　　　; VREF/REF：基準電圧を表す端子名。REFはReference（基準）の意味。ADCの変換尺度や電流アンプの出力基準に使う。REF1/REF2の接続電位は個別に確認する。
      | 用語12　　　　　　　; VCC/VDD/VEE/VS：ICの電源端子名。文字の歴史的な由来を現在の接続機能へ当てはめない。現回路のVEEはU8/U10では浮動基準SW、U9ではGND。各電圧・基準は端子と接続を参照する。
      | 用語13　　　　　　　; GNDP：U10の一次側電源の基準端子。絶縁電源の入力側GND。二次側基準VEE=SWと直接同一の導体ではない。
      | 用語14　　　　　　　; SW：Switching Node（スイッチング点）。主電力段の上下MOSFETとL1がつながる、電圧が高速に切り替わる点。GNDとは別電位。
  L1 : fl_lib/Electrical/Electrical Elements/Inductor  Description=|  l=0.0002 H  r=0 Ohm  g=1e-9 1/Ohm  i_specify=off  i_priority=None  i=0 A  i_nominal_specify=off  i_nominal_value=1  i_nominal_unit=A  v_specify=off  v_priority=None  v=0 V  v_nominal_specify=off  v_nominal_value=1  v_nominal_unit=V  i_L_specify=off  i_L_priority=High  i_L=0 A  i_L_nominal_specify=off  i_L_nominal_value=1  i_L_nominal_unit=A
      | この回路での名前　　; L1
      | 部品名　　　　　　　; NAC-20-0201
      | この回路での役割　　; 太陽電池から電池へ電力を送るとき、充電電流をならすための主インダクタ。
      | ここでの動き　　　　; 上側・下側スイッチQ1/Q2の切替に応じてエネルギーを蓄えたり渡したりし、充電電流の急な変化を抑える。
      | 
      | 【詳しい働き・仕様・接続・確認の範囲】
      | 部品種別　　　　　　; 主降圧インダクタ
      | 公称値　　　　　　　; 200 uH
      | 配置目的　　　　　　; Q1/Q2のスイッチング電圧を受け、電流の変化を抑えながら出力へエネルギーを渡す。
      | 意図する動作　　　　; Q1導通中とQ2導通中に電流経路が切り替わる。飽和電流、銅損、コア損、温度上昇の実部品適合は別途確認する。
      | 端子と接続　　　　　; 1 p → SW、2 n → L_OUT
      | モデルの範囲　　　　; Simscape標準インダクタの集中定数表現。直流重畳による飽和、銅損・コア損を型番から自動同定していない。
      | モデル設定　　　　　; l=200 µH、r=0 Ω。これらは保存モデルの設定値であり、すべてが実部品の保証値という意味ではない。
      | 確認の範囲　　　　　; 本説明は保存回路の部品情報・端子割当・既存設計意図を整理したもの。今回の説明更新によって新たな動作試験や実機検証を実施した意味ではない。
      | 設計記録　　　　　　; evaluation\component_annotations_20261022_r01\before_graph.json
      | evaluation\component_annotations_20261022_r01\before_metadata.json
      | evaluation\protection_capacitor_integration_20261021_r01\final_delivery\independent_readback\physical_bom.json
      | 
      | 【この説明欄の略語・記号】
      | 用語1　　　　　　　 ; MOSFET：Metal-Oxide-Semiconductor Field-Effect Transistor（金属・酸化膜・半導体構造の電界効果トランジスタ）。ゲートとソースの電圧でドレインとソースの導通を制御する素子。N-MOSはNチャネル型を表す。
      | 用語2　　　　　　　 ; GND：Ground（回路の基準電位・電流帰路）。この図の共通基準。保護接地や大地への接続を意味するとは限らない。
      | 用語3　　　　　　　 ; SW：Switching Node（スイッチング点）。主電力段の上下MOSFETとL1がつながる、電圧が高速に切り替わる点。GNDとは別電位。
      settings: AttributesFormatString=200 uH
  LTC4364_Protection : Subsystem  Description=|
      | この回路での名前　　; LTC4364_Protection（充電経路の保護回路全体）
      | 部品名　　　　　　　; P_U1：LTC4364IMS-1#PBF、P_Q1/P_Q2と周辺部品。複数部品の回路。
      | この回路での役割　　; 充電器と電池の間に置き、逆流を防ぐとともに、異常時には充電を制限・停止する保護回路。
      | ここでの動き　　　　; 内部の保護ICがMOSFETを制御して主電流の通し方を変える。電流・電圧の検出、動作条件の設定、マイコンへの通知などを含み、外箱1個がIC1個を意味するものではない。
      | 
      | 【内部の構成・接続・確認の範囲】
      | 識別の補足　　　　　; LTC4364_Protection（保護回路全体をまとめた外箱）
      | 部品名の補足　　　　; P_U1：LTC4364IMS-1#PBF、P_Q1/P_Q2、検出・設定用の周辺部品。IC単体ではなく、複数部品で構成する回路。
      | 詳しい役割　　　　　; 充電器出力と電池の間の保護装置。電池から充電器への逆流を防ぎ、異常時には順方向の充電電流も制限・遮断する。LTC4364が外付けMOSFETを制御する構成。
      | 通常時の動き　　　　; 充電器から電池へ電流を流す。P_Q1/P_Q2を通電させ、逆流防止をMOSFETで行うことでダイオードの順方向電圧降下による損失を抑える狙いがある。効率の改善量をここで保証するものではない。
      | 逆流時の動き　　　　; 電池側から充電器側へ電流が戻ろうとすると、DGATEでP_Q2をOFFへ制御して逆流を抑える。夜間など上流電圧が低下したときに、電池を上流へ放電させないための役割。
      | 異常時の動き　　　　; HGATEでP_Q1を制御し、出力の過電圧や過電流を制限する。設定した異常継続時間を超えると順方向の給電も停止する。採用する-1型は、この保護停止を保持するラッチ型であり、自動再試行型の-2とは異なる。
      | 独立保護の意味　　　; 通電が許可され、ICの動作条件が満たされている間は、保護判定をマイコンの計算に任せずICと周辺抵抗・コンデンサが行う。RP2040が通常の充電制御を担当し、このICが電力経路の保護を担当する。
      | マイコンとの関係　　; SHDN（採用MSOP-16品の9番端子）をLowにすると停止できる。Highは通電の許可であり、ICの保護判定を無効化する指令ではない。主電力段Q1/Q2へ送る相補PWMとは別のON/OFF制御。
      | 現在の接続　　　　　; RP2040のGP11 → MAIN_EN → MCU_EN → P_RSHDN_SER 1 kΩ → SHDNを接続済み。SHDNには47 kΩのプルダウンを置く。FLTは22 kΩで3.3 Vへプルアップし、PROTECTION_FLT_NからGP13へ接続する。
      | 現在の使用状態　　　; 独立保護回路をモデル化し、マイコン用の停止入力・故障通知の接続も用意済み。一方、現行c05用MicroPythonでの起動・停止・FLT監視・ラッチ復帰をまとめた統合実装と一貫試験は未完了。試験用GPIO刺激は、RP2040実行の確認とは区別する。
      | 拡張できること　　　; MicroPython側を追加・統合すれば、充電終了時の給電停止、測定値に応じた停止要求、故障の記録、原因解消を確認した後の復帰制御に利用できる。これは拡張候補であり、現状の完成済み機能とはしない。
      | 復帰時の注意　　　　; SHDNによるリセットも可能だが、原因が残ったまま繰り返し再投入しない。メーカーが示す冷却時間・リセット条件と、MOSFETの許容動作領域を確認して復帰シーケンスを決める。
      | 通知端子の意味　　　; FLTは保護タイマーに関係する異常予告・通知用のオープンドレイン出力であり、すべての異常や逆流を個別に知らせる信号ではない。ENOUTは現構成ではGPIO監視に未使用。
      | 電力端子　　　　　　; VINは上流のVOUT、VOUTは下流のBAT_PLUSへ接続する。外側ポートのVOUTと上流ネット名VOUTは別の役割なので混同しない。
      | 基準端子　　　　　　; RETURNは本回路で共通GNDへ接続。PROT_RETURNの名称はProtection Returnを意味し、プロトタイプの意味ではない。
      | しきい値の意味　　　; 保護用しきい値はCC/CV充電目標と区別する。保護しきい値の典型値だけで電池の57.6 V／15 A以下を保証したことにはならない。公差・応答・過渡を含む上限確認が必要。
      | モデルの範囲　　　　; P_U1内部はプロジェクト作成の機能近似。保護MOSFETの固定容量・単一点近似、寄生とSOA・熱の未検証範囲を残す。
      | メーカー資料　　　　; https://www.analog.com/media/en/technical-documentation/data-sheets/ltc4364-1-4364-2.pdf Rev.B。機能説明の根拠であり、この回路の実機成立を証明する資料ではない。
      | 確認の範囲　　　　　; 説明文だけの更新。接続、部品値、しきい値、モデル実装やMicroPythonコードは変更しない。
      | 
      | 【この説明欄の略語・記号】
      | 用語1　　　　　　　 ; IC：Integrated Circuit（集積回路）。複数の電子素子と機能を小さな半導体チップに集積した部品。
      | 用語2　　　　　　　 ; MCU：Microcontroller Unit（マイクロコントローラ）。プログラムを実行し、測定値の処理や出力制御を担当する小型計算機。
      | 用語3　　　　　　　 ; PWM：Pulse Width Modulation（パルス幅変調）。周期に対するON時間の割合を変えて、スイッチの平均的な電力伝達を調整する方式。
      | 用語4　　　　　　　 ; GPIO：General-Purpose Input/Output（汎用入出力端子）。入力・出力や周辺機能に割り当てられる端子。GPの後の数字はRP2040の端子信号番号で、基板上の物理ピン番号とは別。
      | 用語5　　　　　　　 ; MOSFET：Metal-Oxide-Semiconductor Field-Effect Transistor（金属・酸化膜・半導体構造の電界効果トランジスタ）。ゲートとソースの電圧でドレインとソースの導通を制御する素子。N-MOSはNチャネル型を表す。
      | 用語6　　　　　　　 ; SOA：Safe Operating Area（安全動作領域）。素子が扱える電圧・電流・継続時間・温度の組合せ。耐圧や最大電流を個別に満たすだけではSOAの成立にならない。
      | 用語7　　　　　　　 ; CC：Constant Current（定電流）。電流を目標値付近に保つ制御。型番に含まれるCCという文字列は対象外。
      | 用語8　　　　　　　 ; CV：Constant Voltage（定電圧）。電圧を目標値付近に保つ制御。
      | 用語9　　　　　　　 ; MSOP：Mini Small Outline Package（小型の外形パッケージ形式）。末尾の16は端子数を表す。本部品ではMSOP-16の端子配置を使用する。
      | 用語10　　　　　　　; GND：Ground（回路の基準電位・電流帰路）。この図の共通基準。保護接地や大地への接続を意味するとは限らない。
      | 用語11　　　　　　　; SHDN：Shutdown（停止制御端子）。LTC4364ではLowで停止を指示する。Highは動作許可であり、保護判定を無効にするものではない。
      | 用語12　　　　　　　; FLT：Fault（故障状態通知）。LTC4364の故障警告出力。全種類の異常や逆流を一律に通知する信号という意味ではない。
      | 用語13　　　　　　　; EN：Enable（動作許可）。対象機能の動作を許可する信号。端子ごとの有効レベルや接続状態に従う。
      | 用語14　　　　　　　; ENOUT：Enable Output（動作許可状態の出力）。LTC4364の下流回路向け許可出力。SHDNへの外部停止指示とは方向が逆の別端子。
      | 用語15　　　　　　　; VIN/VOUT：入力電圧・出力電圧を表す端子／ネット名。INは入力、OUTは出力。電源変換器の電力端子なのか、検出用端子なのかは対象部品によって異なるため、端子と接続の説明に従う。
      | 用語16　　　　　　　; HGATE/DGATE：LTC4364の二つの外付けMOSFETゲート駆動出力。HGATEは主に電圧・電流制限側のP_Q1、DGATEは理想ダイオード／逆流防止側のP_Q2を駆動する。主電力段の上下PWMとは別の仕組み。
      | 用語17　　　　　　　; PROT_RETURN：保護回路の共通帰路。PROTはProtection（保護）、RETURNは帰路。プロトタイプの略ではなく、現回路では共通GNDへつながる。
      settings: AttributesFormatString=LTC4364 保護回路
  MCU_GP13_Protection : ConnectionLabel  Description=|  Label=PROTECTION_FLT_N
      | この回路での名前　　; PROTECTION_FLT_N
      | 種別　　　　　　　　; ConnectionLabel
      | この回路での役割　　; 保護IC P_U1のFLT出力から、RP2040基板U7のGP13へ異常状態を返す。P_RFLT_PUを介して3.3Vへプルアップされる。すべての異常や逆流を個別通知する信号ではない。
      | この場所の直接接続　; U7（RP2040搭載Pico W／SC0918）: 17(GP13)
      | 直接接続の範囲　　　; このラベルから実際の線・分岐・明示的な境界端子だけを追った接続。同名ラベルによる離れた場所への接続はこの欄に含めない。
      | 同一ネットの主接続　; P_U1（保護MOSFETを制御する保護IC／LTC4364IMS-1#PBF）: FLT
      |                     ; U7（RP2040搭載Pico W／SC0918）: 17(GP13)
      |                     ; P_RFLT_PU（LTC4364のオープンドレインFLTをMCUの3.3 V系へ引き上げる／22 kΩ）: 2
      | 同一ネット全端子　　; P_RFLT_PU: 2
      |                     ; P_U1: FLT
      |                     ; U7: 17(GP13)
      | 接続部品数　　　　　; 3部品（部品番号で集計。同一ネット全体）
      | 接続端子数　　　　　; 3端子（423端子の部品対応表で集計。ラベル・境界ポートの重複は含めない）
      | この場所の端子数　　; 1端子／1部品（同名ラベルによる接続を除く）
      | 同階層同名ラベル数　; 2個（このラベル自身を含む）
      | 全階層の接続ラベル　; 2個（実際に同じノードへつながるラベル。名前が違う別名も含む）
      | 接続ルール　　　　　; 同じ階層の同じラベル名を仮想配線として結ぶ。別のSubsystem内とは名前だけでつながらず、明示的なConnection Portと配線をたどる。色は用途の表示であり接続を決めない。
      | 確認の範囲　　　　　; 現在の保存回路の端子・配線から求めた静的接続。抵抗やICの内部を導線として短絡せずに集計した。説明の更新は動作シミュレーション、タイミング、実部品の性能・実機動作を保証するものではない。
      | 記録の基準　　　　　; measurement_label_layout_20261022_r01/after_layout_graph.json。部品対応表は端子名の対応付けにのみ使用。
      | 
      | 【この説明欄の略語・記号】
      | 用語1　　　　　　　 ; IC：Integrated Circuit（集積回路）。複数の電子素子と機能を小さな半導体チップに集積した部品。
      | 用語2　　　　　　　 ; MCU：Microcontroller Unit（マイクロコントローラ）。プログラムを実行し、測定値の処理や出力制御を担当する小型計算機。
      | 用語3　　　　　　　 ; GPIO：General-Purpose Input/Output（汎用入出力端子）。入力・出力や周辺機能に割り当てられる端子。GPの後の数字はRP2040の端子信号番号で、基板上の物理ピン番号とは別。
      | 用語4　　　　　　　 ; MOSFET：Metal-Oxide-Semiconductor Field-Effect Transistor（金属・酸化膜・半導体構造の電界効果トランジスタ）。ゲートとソースの電圧でドレインとソースの導通を制御する素子。N-MOSはNチャネル型を表す。
      | 用語5　　　　　　　 ; FLT：Fault（故障状態通知）。LTC4364の故障警告出力。全種類の異常や逆流を一律に通知する信号という意味ではない。
  MeasureLabel_C19_ADC_VPV : ConnectionLabel  Description=|  Label=ADC_VPV
      | この回路での名前　　; ADC_VPV
      | 種別　　　　　　　　; ConnectionLabel
      | この回路での役割　　; PV入力電圧をR16・R17・R18で分圧した測定信号を、コンデンサC19で平滑し、ADC U1のCH0へ渡す。測定元のVINと同じ導線ではなく、分圧後の電圧を運ぶ。
      | この場所の直接接続　; C19（PV入力電圧の分圧後の信号を平滑するコンデンサ／100 nF）: 1
      |                     ; R17（PV入力電圧の分圧抵抗・上側2段目／75 kohm 0.1%）: 2
      |                     ; R18（PV入力電圧の分圧抵抗・下側／3.3 kohm 0.1%）: 1
      | 直接接続の範囲　　　; このラベルから実際の線・分岐・明示的な境界端子だけを追った接続。同名ラベルによる離れた場所への接続はこの欄に含めない。
      | 同一ネットの主接続　; R17（PV入力電圧の分圧抵抗・上側2段目／75 kohm 0.1%）: 2
      |                     ; R18（PV入力電圧の分圧抵抗・下側／3.3 kohm 0.1%）: 1
      |                     ; C19（PV入力電圧の分圧後の信号を平滑するコンデンサ／100 nF）: 1
      |                     ; U1（外付けADC／MCP3208-CI/SL）: 1(CH0)
      | 同一ネット全端子　　; C19: 1
      |                     ; R17: 2
      |                     ; R18: 1
      |                     ; U1: 1(CH0)
      | 接続部品数　　　　　; 4部品（部品番号で集計。同一ネット全体）
      | 接続端子数　　　　　; 4端子（423端子の部品対応表で集計。ラベル・境界ポートの重複は含めない）
      | この場所の端子数　　; 3端子／3部品（同名ラベルによる接続を除く）
      | 同階層同名ラベル数　; 2個（このラベル自身を含む）
      | 全階層の接続ラベル　; 2個（実際に同じノードへつながるラベル。名前が違う別名も含む）
      | 接続ルール　　　　　; 同じ階層の同じラベル名を仮想配線として結ぶ。別のSubsystem内とは名前だけでつながらず、明示的なConnection Portと配線をたどる。色は用途の表示であり接続を決めない。
      | 確認の範囲　　　　　; 現在の保存回路の端子・配線から求めた静的接続。抵抗やICの内部を導線として短絡せずに集計した。説明の更新は動作シミュレーション、タイミング、実部品の性能・実機動作を保証するものではない。
      | 記録の基準　　　　　; measurement_label_layout_20261022_r01/after_layout_graph.json。部品対応表は端子名の対応付けにのみ使用。
      | 
      | 【この説明欄の略語・記号】
      | 用語1　　　　　　　 ; ADC：Analog-to-Digital Converter（アナログ・デジタル変換器）。測定電圧をデジタル値へ変換する回路。電流や温度も、センサーで電圧へ変換した後に読み取る。
      | 用語2　　　　　　　 ; IC：Integrated Circuit（集積回路）。複数の電子素子と機能を小さな半導体チップに集積した部品。
      | 用語3　　　　　　　 ; CH：Channel（測定チャネル）。CH0〜CH7はADCの入力番号であり、同時測定を意味しない。
      | 用語4　　　　　　　 ; PV：Photovoltaic（太陽光発電）。光を電気へ変える発電方式。PVを含むネット名は太陽電池側の測定・電力経路を表す。
      | 用語5　　　　　　　 ; VIN/VOUT：入力電圧・出力電圧を表す端子／ネット名。INは入力、OUTは出力。電源変換器の電力端子なのか、検出用端子なのかは対象部品によって異なるため、端子と接続の説明に従う。
  MeasureLabel_C20_ADC_VOUT : ConnectionLabel  Description=|  Label=ADC_VOUT
      | この回路での名前　　; ADC_VOUT
      | 種別　　　　　　　　; ConnectionLabel
      | この回路での役割　　; 保護回路より手前の出力電圧VOUTをR19・R20・R21で分圧した測定信号を、コンデンサC20で平滑し、ADC U1のCH2へ渡す。分圧前のVOUTとは別の電圧ノード。
      | この場所の直接接続　; C20（出力電圧の分圧後の信号を平滑するコンデンサ／100 nF）: 1
      |                     ; R20（出力電圧の分圧抵抗・上側2段目／75 kohm 0.1%）: 2
      |                     ; R21（出力電圧の分圧抵抗・下側／3.3 kohm 0.1%）: 1
      | 直接接続の範囲　　　; このラベルから実際の線・分岐・明示的な境界端子だけを追った接続。同名ラベルによる離れた場所への接続はこの欄に含めない。
      | 同一ネットの主接続　; R20（出力電圧の分圧抵抗・上側2段目／75 kohm 0.1%）: 2
      |                     ; R21（出力電圧の分圧抵抗・下側／3.3 kohm 0.1%）: 1
      |                     ; C20（出力電圧の分圧後の信号を平滑するコンデンサ／100 nF）: 1
      |                     ; U1（外付けADC／MCP3208-CI/SL）: 3(CH2)
      | 同一ネット全端子　　; C20: 1
      |                     ; R20: 2
      |                     ; R21: 1
      |                     ; U1: 3(CH2)
      | 接続部品数　　　　　; 4部品（部品番号で集計。同一ネット全体）
      | 接続端子数　　　　　; 4端子（423端子の部品対応表で集計。ラベル・境界ポートの重複は含めない）
      | この場所の端子数　　; 3端子／3部品（同名ラベルによる接続を除く）
      | 同階層同名ラベル数　; 2個（このラベル自身を含む）
      | 全階層の接続ラベル　; 2個（実際に同じノードへつながるラベル。名前が違う別名も含む）
      | 接続ルール　　　　　; 同じ階層の同じラベル名を仮想配線として結ぶ。別のSubsystem内とは名前だけでつながらず、明示的なConnection Portと配線をたどる。色は用途の表示であり接続を決めない。
      | 確認の範囲　　　　　; 現在の保存回路の端子・配線から求めた静的接続。抵抗やICの内部を導線として短絡せずに集計した。説明の更新は動作シミュレーション、タイミング、実部品の性能・実機動作を保証するものではない。
      | 記録の基準　　　　　; measurement_label_layout_20261022_r01/after_layout_graph.json。部品対応表は端子名の対応付けにのみ使用。
      | 
      | 【この説明欄の略語・記号】
      | 用語1　　　　　　　 ; ADC：Analog-to-Digital Converter（アナログ・デジタル変換器）。測定電圧をデジタル値へ変換する回路。電流や温度も、センサーで電圧へ変換した後に読み取る。
      | 用語2　　　　　　　 ; IC：Integrated Circuit（集積回路）。複数の電子素子と機能を小さな半導体チップに集積した部品。
      | 用語3　　　　　　　 ; CH：Channel（測定チャネル）。CH0〜CH7はADCの入力番号であり、同時測定を意味しない。
      | 用語4　　　　　　　 ; VIN/VOUT：入力電圧・出力電圧を表す端子／ネット名。INは入力、OUTは出力。電源変換器の電力端子なのか、検出用端子なのかは対象部品によって異なるため、端子と接続の説明に従う。
  MeasureLabel_C21_ADC_VBAT : ConnectionLabel  Description=|  Label=ADC_VBAT
      | この回路での名前　　; ADC_VBAT
      | 種別　　　　　　　　; ConnectionLabel
      | この回路での役割　　; 充電経路のヒューズF3より充電器側にあるBAT_PLUSを、R22・R23・R24で分圧した測定信号。コンデンサC21で平滑してADC U1のCH6へ渡す。F3が開放した状態では、BT1正極の電圧と同じとは限らない。
      | この場所の直接接続　; C21（電池側電圧の分圧後の信号を平滑するコンデンサ／100 nF）: 1
      |                     ; R23（電池側電圧の分圧抵抗・上側2段目／75 kohm 0.1%）: 2
      |                     ; R24（電池側電圧の分圧抵抗・下側／3.3 kohm 0.1%）: 1
      | 直接接続の範囲　　　; このラベルから実際の線・分岐・明示的な境界端子だけを追った接続。同名ラベルによる離れた場所への接続はこの欄に含めない。
      | 同一ネットの主接続　; R23（電池側電圧の分圧抵抗・上側2段目／75 kohm 0.1%）: 2
      |                     ; R24（電池側電圧の分圧抵抗・下側／3.3 kohm 0.1%）: 1
      |                     ; C21（電池側電圧の分圧後の信号を平滑するコンデンサ／100 nF）: 1
      |                     ; U1（外付けADC／MCP3208-CI/SL）: 7(CH6)
      | 同一ネット全端子　　; C21: 1
      |                     ; R23: 2
      |                     ; R24: 1
      |                     ; U1: 7(CH6)
      | 接続部品数　　　　　; 4部品（部品番号で集計。同一ネット全体）
      | 接続端子数　　　　　; 4端子（423端子の部品対応表で集計。ラベル・境界ポートの重複は含めない）
      | この場所の端子数　　; 3端子／3部品（同名ラベルによる接続を除く）
      | 同階層同名ラベル数　; 2個（このラベル自身を含む）
      | 全階層の接続ラベル　; 2個（実際に同じノードへつながるラベル。名前が違う別名も含む）
      | 接続ルール　　　　　; 同じ階層の同じラベル名を仮想配線として結ぶ。別のSubsystem内とは名前だけでつながらず、明示的なConnection Portと配線をたどる。色は用途の表示であり接続を決めない。
      | 確認の範囲　　　　　; 現在の保存回路の端子・配線から求めた静的接続。抵抗やICの内部を導線として短絡せずに集計した。説明の更新は動作シミュレーション、タイミング、実部品の性能・実機動作を保証するものではない。
      | 記録の基準　　　　　; measurement_label_layout_20261022_r01/after_layout_graph.json。部品対応表は端子名の対応付けにのみ使用。
      | 
      | 【この説明欄の略語・記号】
      | 用語1　　　　　　　 ; ADC：Analog-to-Digital Converter（アナログ・デジタル変換器）。測定電圧をデジタル値へ変換する回路。電流や温度も、センサーで電圧へ変換した後に読み取る。
      | 用語2　　　　　　　 ; IC：Integrated Circuit（集積回路）。複数の電子素子と機能を小さな半導体チップに集積した部品。
      | 用語3　　　　　　　 ; CH：Channel（測定チャネル）。CH0〜CH7はADCの入力番号であり、同時測定を意味しない。
  MeasureLabel_C25_ADC_IL : ConnectionLabel  Description=|  Label=ADC_IL
      | この回路での名前　　; ADC_IL
      | 種別　　　　　　　　; ConnectionLabel
      | この回路での役割　　; L1直後の電流検出アンプU3の出力を、R26とC25のRCフィルタに通してADC U1のCH3へ渡す。R2より下流に出力コンデンサがあるため、過渡時の電池端子電流と常に同じ量ではない。
      | この場所の直接接続　; C25（L1出力電流の測定信号を平滑するコンデンサ／100 nF）: 1
      |                     ; R26（L1出力電流の測定信号を整えるRCフィルタの直列抵抗／100 ohm 0.1%）: 2
      | 直接接続の範囲　　　; このラベルから実際の線・分岐・明示的な境界端子だけを追った接続。同名ラベルによる離れた場所への接続はこの欄に含めない。
      | 同一ネットの主接続　; R26（L1出力電流の測定信号を整えるRCフィルタの直列抵抗／100 ohm 0.1%）: 2
      |                     ; C25（L1出力電流の測定信号を平滑するコンデンサ／100 nF）: 1
      |                     ; U1（外付けADC／MCP3208-CI/SL）: 4(CH3)
      | 同一ネット全端子　　; C25: 1
      |                     ; R26: 2
      |                     ; U1: 4(CH3)
      | 接続部品数　　　　　; 3部品（部品番号で集計。同一ネット全体）
      | 接続端子数　　　　　; 3端子（423端子の部品対応表で集計。ラベル・境界ポートの重複は含めない）
      | この場所の端子数　　; 2端子／2部品（同名ラベルによる接続を除く）
      | 同階層同名ラベル数　; 2個（このラベル自身を含む）
      | 全階層の接続ラベル　; 2個（実際に同じノードへつながるラベル。名前が違う別名も含む）
      | 接続ルール　　　　　; 同じ階層の同じラベル名を仮想配線として結ぶ。別のSubsystem内とは名前だけでつながらず、明示的なConnection Portと配線をたどる。色は用途の表示であり接続を決めない。
      | 確認の範囲　　　　　; 現在の保存回路の端子・配線から求めた静的接続。抵抗やICの内部を導線として短絡せずに集計した。説明の更新は動作シミュレーション、タイミング、実部品の性能・実機動作を保証するものではない。
      | 記録の基準　　　　　; measurement_label_layout_20261022_r01/after_layout_graph.json。部品対応表は端子名の対応付けにのみ使用。
      | 
      | 【この説明欄の略語・記号】
      | 用語1　　　　　　　 ; ADC：Analog-to-Digital Converter（アナログ・デジタル変換器）。測定電圧をデジタル値へ変換する回路。電流や温度も、センサーで電圧へ変換した後に読み取る。
      | 用語2　　　　　　　 ; IC：Integrated Circuit（集積回路）。複数の電子素子と機能を小さな半導体チップに集積した部品。
      | 用語3　　　　　　　 ; CH：Channel（測定チャネル）。CH0〜CH7はADCの入力番号であり、同時測定を意味しない。
      | 用語4　　　　　　　 ; RC：Resistor-Capacitor（抵抗とコンデンサの組合せ）。主に測定信号のフィルタや時定数を作る。カットオフ周波数は実際の接続と抵抗・容量から求める。
  MeasureLabel_C27_ADC_TBAT : ConnectionLabel  Description=|  Label=ADC_TBAT
      | この回路での名前　　; ADC_TBAT
      | 種別　　　　　　　　; ConnectionLabel
      | この回路での役割　　; 電池付近の温度センサーU4の出力を、R28とC27のRC回路に通してADC U1のCH4へ渡す。温度を表す電圧信号であり、電池端子電圧を測るADC_VBATとは役割が異なる。
      | この場所の直接接続　; C27（電池温度の測定信号を整えるコンデンサ／680 pF）: 1
      |                     ; R28（電池温度の測定信号を整えるRC回路の直列抵抗／47 ohm）: 2
      | 直接接続の範囲　　　; このラベルから実際の線・分岐・明示的な境界端子だけを追った接続。同名ラベルによる離れた場所への接続はこの欄に含めない。
      | 同一ネットの主接続　; R28（電池温度の測定信号を整えるRC回路の直列抵抗／47 ohm）: 2
      |                     ; C27（電池温度の測定信号を整えるコンデンサ／680 pF）: 1
      |                     ; U1（外付けADC／MCP3208-CI/SL）: 5(CH4)
      | 同一ネット全端子　　; C27: 1
      |                     ; R28: 2
      |                     ; U1: 5(CH4)
      | 接続部品数　　　　　; 3部品（部品番号で集計。同一ネット全体）
      | 接続端子数　　　　　; 3端子（423端子の部品対応表で集計。ラベル・境界ポートの重複は含めない）
      | この場所の端子数　　; 2端子／2部品（同名ラベルによる接続を除く）
      | 同階層同名ラベル数　; 2個（このラベル自身を含む）
      | 全階層の接続ラベル　; 2個（実際に同じノードへつながるラベル。名前が違う別名も含む）
      | 接続ルール　　　　　; 同じ階層の同じラベル名を仮想配線として結ぶ。別のSubsystem内とは名前だけでつながらず、明示的なConnection Portと配線をたどる。色は用途の表示であり接続を決めない。
      | 確認の範囲　　　　　; 現在の保存回路の端子・配線から求めた静的接続。抵抗やICの内部を導線として短絡せずに集計した。説明の更新は動作シミュレーション、タイミング、実部品の性能・実機動作を保証するものではない。
      | 記録の基準　　　　　; measurement_label_layout_20261022_r01/after_layout_graph.json。部品対応表は端子名の対応付けにのみ使用。
      | 
      | 【この説明欄の略語・記号】
      | 用語1　　　　　　　 ; ADC：Analog-to-Digital Converter（アナログ・デジタル変換器）。測定電圧をデジタル値へ変換する回路。電流や温度も、センサーで電圧へ変換した後に読み取る。
      | 用語2　　　　　　　 ; IC：Integrated Circuit（集積回路）。複数の電子素子と機能を小さな半導体チップに集積した部品。
      | 用語3　　　　　　　 ; CH：Channel（測定チャネル）。CH0〜CH7はADCの入力番号であり、同時測定を意味しない。
      | 用語4　　　　　　　 ; RC：Resistor-Capacitor（抵抗とコンデンサの組合せ）。主に測定信号のフィルタや時定数を作る。カットオフ周波数は実際の接続と抵抗・容量から求める。
  MeasureLabel_C29_ADC_TSINK : ConnectionLabel  Description=|  Label=ADC_TSINK
      | この回路での名前　　; ADC_TSINK
      | 種別　　　　　　　　; ConnectionLabel
      | この回路での役割　　; 放熱器付近の温度センサーU5の出力を、R29とC29のRC回路に通してADC U1のCH5へ渡す。温度を表す電圧信号を読み取る経路。
      | この場所の直接接続　; C29（放熱器温度の測定信号を整えるコンデンサ／680 pF）: 1
      |                     ; R29（放熱器温度の測定信号を整えるRC回路の直列抵抗／47 ohm）: 2
      | 直接接続の範囲　　　; このラベルから実際の線・分岐・明示的な境界端子だけを追った接続。同名ラベルによる離れた場所への接続はこの欄に含めない。
      | 同一ネットの主接続　; R29（放熱器温度の測定信号を整えるRC回路の直列抵抗／47 ohm）: 2
      |                     ; C29（放熱器温度の測定信号を整えるコンデンサ／680 pF）: 1
      |                     ; U1（外付けADC／MCP3208-CI/SL）: 6(CH5)
      | 同一ネット全端子　　; C29: 1
      |                     ; R29: 2
      |                     ; U1: 6(CH5)
      | 接続部品数　　　　　; 3部品（部品番号で集計。同一ネット全体）
      | 接続端子数　　　　　; 3端子（423端子の部品対応表で集計。ラベル・境界ポートの重複は含めない）
      | この場所の端子数　　; 2端子／2部品（同名ラベルによる接続を除く）
      | 同階層同名ラベル数　; 2個（このラベル自身を含む）
      | 全階層の接続ラベル　; 2個（実際に同じノードへつながるラベル。名前が違う別名も含む）
      | 接続ルール　　　　　; 同じ階層の同じラベル名を仮想配線として結ぶ。別のSubsystem内とは名前だけでつながらず、明示的なConnection Portと配線をたどる。色は用途の表示であり接続を決めない。
      | 確認の範囲　　　　　; 現在の保存回路の端子・配線から求めた静的接続。抵抗やICの内部を導線として短絡せずに集計した。説明の更新は動作シミュレーション、タイミング、実部品の性能・実機動作を保証するものではない。
      | 記録の基準　　　　　; measurement_label_layout_20261022_r01/after_layout_graph.json。部品対応表は端子名の対応付けにのみ使用。
      | 
      | 【この説明欄の略語・記号】
      | 用語1　　　　　　　 ; ADC：Analog-to-Digital Converter（アナログ・デジタル変換器）。測定電圧をデジタル値へ変換する回路。電流や温度も、センサーで電圧へ変換した後に読み取る。
      | 用語2　　　　　　　 ; IC：Integrated Circuit（集積回路）。複数の電子素子と機能を小さな半導体チップに集積した部品。
      | 用語3　　　　　　　 ; CH：Channel（測定チャネル）。CH0〜CH7はADCの入力番号であり、同時測定を意味しない。
      | 用語4　　　　　　　 ; RC：Resistor-Capacitor（抵抗とコンデンサの組合せ）。主に測定信号のフィルタや時定数を作る。カットオフ周波数は実際の接続と抵抗・容量から求める。
  MeasureLabel_R16_VIN : ConnectionLabel  Description=|  Label=VIN
      | この回路での名前　　; VIN
      | 種別　　　　　　　　; ConnectionLabel
      | この回路での役割　　; PV入力の電流検出シャントR27を通過した後の、降圧主電力段の入力電圧。入力コンデンサと上側MOSFET Q1へ電力を供給し、分圧抵抗R16にも電圧を渡す。太陽電池パネル端子そのものとは、途中の主電力部品を介するため区別する。
      | この場所の直接接続　; R16（PV入力電圧の分圧抵抗・上側1段目／75 kohm 0.1%）: 1
      | 直接接続の範囲　　　; このラベルから実際の線・分岐・明示的な境界端子だけを追った接続。同名ラベルによる離れた場所への接続はこの欄に含めない。
      | 同一ネットの主接続　; R27（PV入力電流を検出する4端子シャント抵抗／1 mohm）: IM, KM
      |                     ; Q1（同期整流降圧回路の上側スイッチ／TK9R6E15Q5,S1X）: 2(D)
      |                     ; R16（PV入力電圧の分圧抵抗・上側1段目／75 kohm 0.1%）: 1
      |                     ; C2（入力バルク／470 uF）: 1(p)
      |                     ; U2（PV入力電流の検出アンプ／INA241A3IDDFR）: 1(IN-)
      | 部品を介する経路　　; R16→R17の上側抵抗とR18の下側抵抗で分圧し、C19とADC U1のCH0へ渡す。ADC入力はVINと同じ導線ではない。PV入力電流はR27の両端をU2で読み、R25/C23を通してU1のCH1へ渡す。
      | 同一ネット全端子　　; C2: 1(p)
      |                     ; C3: 1(p)
      |                     ; C4: 1(p)
      |                     ; C7: 1(p)
      |                     ; C8: 1(p)
      |                     ; C9: 1(p)
      |                     ; C10: 1(p)
      |                     ; Q1: 2(D)
      |                     ; R1: 1(p)
      |                     ; R16: 1
      |                     ; R27: IM, KM
      |                     ; U2: 1(IN-)
      | 接続部品数　　　　　; 12部品（部品番号で集計。同一ネット全体）
      | 接続端子数　　　　　; 13端子（423端子の部品対応表で集計。ラベル・境界ポートの重複は含めない）
      | この場所の端子数　　; 1端子／1部品（同名ラベルによる接続を除く）
      | 同階層同名ラベル数　; 2個（このラベル自身を含む）
      | 全階層の接続ラベル　; 4個（実際に同じノードへつながるラベル。名前が違う別名も含む）
      | 接続ルール　　　　　; 同じ階層の同じラベル名を仮想配線として結ぶ。別のSubsystem内とは名前だけでつながらず、明示的なConnection Portと配線をたどる。色は用途の表示であり接続を決めない。
      | 確認の範囲　　　　　; 現在の保存回路の端子・配線から求めた静的接続。抵抗やICの内部を導線として短絡せずに集計した。説明の更新は動作シミュレーション、タイミング、実部品の性能・実機動作を保証するものではない。
      | 記録の基準　　　　　; measurement_label_layout_20261022_r01/after_layout_graph.json。部品対応表は端子名の対応付けにのみ使用。
      | 
      | 【この説明欄の略語・記号】
      | 用語1　　　　　　　 ; ADC：Analog-to-Digital Converter（アナログ・デジタル変換器）。測定電圧をデジタル値へ変換する回路。電流や温度も、センサーで電圧へ変換した後に読み取る。
      | 用語2　　　　　　　 ; IC：Integrated Circuit（集積回路）。複数の電子素子と機能を小さな半導体チップに集積した部品。
      | 用語3　　　　　　　 ; CH：Channel（測定チャネル）。CH0〜CH7はADCの入力番号であり、同時測定を意味しない。
      | 用語4　　　　　　　 ; MOSFET：Metal-Oxide-Semiconductor Field-Effect Transistor（金属・酸化膜・半導体構造の電界効果トランジスタ）。ゲートとソースの電圧でドレインとソースの導通を制御する素子。N-MOSはNチャネル型を表す。
      | 用語5　　　　　　　 ; PV：Photovoltaic（太陽光発電）。光を電気へ変える発電方式。PVを含むネット名は太陽電池側の測定・電力経路を表す。
      | 用語6　　　　　　　 ; GND：Ground（回路の基準電位・電流帰路）。この図の共通基準。保護接地や大地への接続を意味するとは限らない。
      | 用語7　　　　　　　 ; VIN/VOUT：入力電圧・出力電圧を表す端子／ネット名。INは入力、OUTは出力。電源変換器の電力端子なのか、検出用端子なのかは対象部品によって異なるため、端子と接続の説明に従う。
      | 用語8　　　　　　　 ; IP/IM・KP/KM：4端子シャントの端子役割を区別する設計上の表記。IP/IMは主電流端子、KP/KMはKelvin（4端子測定）の検出端子。P/Mは正側・負側の区別であり、端子番号は採用部品の割当を参照する。
      | 用語9　　　　　　　 ; IN+/IN−：差動測定の正側・負側入力。電流検出アンプは両端子の電圧差を読む。IN−は必ずGNDという意味ではない。
  MeasureLabel_R19_VOUT : ConnectionLabel  Description=|  Label=VOUT
      | この回路での名前　　; VOUT
      | 種別　　　　　　　　; ConnectionLabel
      | この回路での役割　　; 降圧電力段の出力平滑コンデンサ、L1後の出力電流検出抵抗R2の出力側、保護回路の入力を結ぶ。保護回路より上流の電圧をR19の分圧回路でも測る。
      | この場所の直接接続　; R19（保護回路より上流の出力電圧の分圧抵抗・上側／75 kohm 0.1%）: 1
      | 直接接続の範囲　　　; このラベルから実際の線・分岐・明示的な境界端子だけを追った接続。同名ラベルによる離れた場所への接続はこの欄に含めない。
      | 同一ネットの主接続　; C13（出力バルク／470 uF）: 1(p)
      |                     ; C14（出力バルク／470 uF）: 1(p)
      |                     ; C15（出力高速バイパス／10 uF）: 1(p)
      |                     ; C16（出力高速バイパス／10 uF）: 1(p)
      |                     ; R2（L1直後の出力電流を検出する4端子シャント抵抗／CSS4J-4026R-1L00F）: IM, KM
      |                     ; U3（L1直後の出力電流の検出アンプ／INA241A3IDDFR）: 1(IN-)
      |                     ; P_Q1（充電器から蓄電池へ向かう電力経路を開閉し、起動時や異常時には流れる電流・出力電圧を制限するために置く／150V / 4.8mOhm max at25C10V）: D
      |                     ; R19（保護回路より上流の出力電圧の分圧抵抗・上側／75 kohm 0.1%）: 1
      | 部品を介する経路　　; R19→R20の上側抵抗とR21の下側抵抗で分圧し、C20とADC U1のCH2へ渡す。ADC入力はVOUTと同じ導線ではない。電流の測定経路はR2両端→U3→R26/C25→U1 CH3。R2より下流に出力コンデンサがあるため、過渡時の電池端子電流と常時同一ではない。
      | 同一ネット全端子　　; C13: 1(p)
      |                     ; C14: 1(p)
      |                     ; C15: 1(p)
      |                     ; C16: 1(p)
      |                     ; P_Q1: D
      |                     ; P_R1: 1
      |                     ; P_R4: 1
      |                     ; R2: IM, KM
      |                     ; R19: 1
      |                     ; U3: 1(IN-)
      | 接続部品数　　　　　; 10部品（部品番号で集計。同一ネット全体）
      | 接続端子数　　　　　; 11端子（423端子の部品対応表で集計。ラベル・境界ポートの重複は含めない）
      | この場所の端子数　　; 1端子／1部品（同名ラベルによる接続を除く）
      | 同階層同名ラベル数　; 3個（このラベル自身を含む）
      | 全階層の接続ラベル　; 5個（実際に同じノードへつながるラベル。名前が違う別名も含む）
      | 接続ルール　　　　　; 同じ階層の同じラベル名を仮想配線として結ぶ。別のSubsystem内とは名前だけでつながらず、明示的なConnection Portと配線をたどる。色は用途の表示であり接続を決めない。
      | 確認の範囲　　　　　; 現在の保存回路の端子・配線から求めた静的接続。抵抗やICの内部を導線として短絡せずに集計した。説明の更新は動作シミュレーション、タイミング、実部品の性能・実機動作を保証するものではない。
      | 記録の基準　　　　　; measurement_label_layout_20261022_r01/after_layout_graph.json。部品対応表は端子名の対応付けにのみ使用。
      | 
      | 【この説明欄の略語・記号】
      | 用語1　　　　　　　 ; ADC：Analog-to-Digital Converter（アナログ・デジタル変換器）。測定電圧をデジタル値へ変換する回路。電流や温度も、センサーで電圧へ変換した後に読み取る。
      | 用語2　　　　　　　 ; IC：Integrated Circuit（集積回路）。複数の電子素子と機能を小さな半導体チップに集積した部品。
      | 用語3　　　　　　　 ; CH：Channel（測定チャネル）。CH0〜CH7はADCの入力番号であり、同時測定を意味しない。
      | 用語4　　　　　　　 ; GND：Ground（回路の基準電位・電流帰路）。この図の共通基準。保護接地や大地への接続を意味するとは限らない。
      | 用語5　　　　　　　 ; VIN/VOUT：入力電圧・出力電圧を表す端子／ネット名。INは入力、OUTは出力。電源変換器の電力端子なのか、検出用端子なのかは対象部品によって異なるため、端子と接続の説明に従う。
      | 用語6　　　　　　　 ; IP/IM・KP/KM：4端子シャントの端子役割を区別する設計上の表記。IP/IMは主電流端子、KP/KMはKelvin（4端子測定）の検出端子。P/Mは正側・負側の区別であり、端子番号は採用部品の割当を参照する。
      | 用語7　　　　　　　 ; IN+/IN−：差動測定の正側・負側入力。電流検出アンプは両端子の電圧差を読む。IN−は必ずGNDという意味ではない。
  MeasureLabel_R1_VIN : ConnectionLabel  Description=|  Label=VIN
      | この回路での名前　　; VIN
      | 種別　　　　　　　　; ConnectionLabel
      | この回路での役割　　; PV入力の電流検出シャントR27を通過した後の、降圧主電力段の入力電圧。入力コンデンサと上側MOSFET Q1へ電力を供給し、分圧抵抗R16にも電圧を渡す。太陽電池パネル端子そのものとは、途中の主電力部品を介するため区別する。
      | この場所の直接接続　; C2（入力バルク／470 uF）: 1(p)
      |                     ; C3（入力バルク／470 uF）: 1(p)
      |                     ; C4（入力バルク／470 uF）: 1(p)
      |                     ; C7（入力フィルム／3.3 uF）: 1(p)
      |                     ; C8（入力高速バイパス／2.2 uF）: 1(p)
      |                     ; C9（入力高速バイパス／2.2 uF）: 1(p)
      |                     ; C10（入力高速バイパス／2.2 uF）: 1(p)
      |                     ; Q1（同期整流降圧回路の上側スイッチ／TK9R6E15Q5,S1X）: 2(D)
      |                     ; R1（VIN–GND間へ常時接続し、入力側コンデンサの電荷を徐々に放電する／15 kohm）: 1(p)
      |                     ; R27（PV入力電流を検出する4端子シャント抵抗／1 mohm）: IM, KM
      | 直接接続の範囲　　　; このラベルから実際の線・分岐・明示的な境界端子だけを追った接続。同名ラベルによる離れた場所への接続はこの欄に含めない。
      | 同一ネットの主接続　; R27（PV入力電流を検出する4端子シャント抵抗／1 mohm）: IM, KM
      |                     ; Q1（同期整流降圧回路の上側スイッチ／TK9R6E15Q5,S1X）: 2(D)
      |                     ; R16（PV入力電圧の分圧抵抗・上側1段目／75 kohm 0.1%）: 1
      |                     ; C2（入力バルク／470 uF）: 1(p)
      |                     ; U2（PV入力電流の検出アンプ／INA241A3IDDFR）: 1(IN-)
      | 部品を介する経路　　; R16→R17の上側抵抗とR18の下側抵抗で分圧し、C19とADC U1のCH0へ渡す。ADC入力はVINと同じ導線ではない。PV入力電流はR27の両端をU2で読み、R25/C23を通してU1のCH1へ渡す。
      | 同一ネット全端子　　; C2: 1(p)
      |                     ; C3: 1(p)
      |                     ; C4: 1(p)
      |                     ; C7: 1(p)
      |                     ; C8: 1(p)
      |                     ; C9: 1(p)
      |                     ; C10: 1(p)
      |                     ; Q1: 2(D)
      |                     ; R1: 1(p)
      |                     ; R16: 1
      |                     ; R27: IM, KM
      |                     ; U2: 1(IN-)
      | 接続部品数　　　　　; 12部品（部品番号で集計。同一ネット全体）
      | 接続端子数　　　　　; 13端子（423端子の部品対応表で集計。ラベル・境界ポートの重複は含めない）
      | この場所の端子数　　; 11端子／10部品（同名ラベルによる接続を除く）
      | 同階層同名ラベル数　; 2個（このラベル自身を含む）
      | 全階層の接続ラベル　; 4個（実際に同じノードへつながるラベル。名前が違う別名も含む）
      | 接続ルール　　　　　; 同じ階層の同じラベル名を仮想配線として結ぶ。別のSubsystem内とは名前だけでつながらず、明示的なConnection Portと配線をたどる。色は用途の表示であり接続を決めない。
      | 確認の範囲　　　　　; 現在の保存回路の端子・配線から求めた静的接続。抵抗やICの内部を導線として短絡せずに集計した。説明の更新は動作シミュレーション、タイミング、実部品の性能・実機動作を保証するものではない。
      | 記録の基準　　　　　; measurement_label_layout_20261022_r01/after_layout_graph.json。部品対応表は端子名の対応付けにのみ使用。
      | 
      | 【この説明欄の略語・記号】
      | 用語1　　　　　　　 ; ADC：Analog-to-Digital Converter（アナログ・デジタル変換器）。測定電圧をデジタル値へ変換する回路。電流や温度も、センサーで電圧へ変換した後に読み取る。
      | 用語2　　　　　　　 ; IC：Integrated Circuit（集積回路）。複数の電子素子と機能を小さな半導体チップに集積した部品。
      | 用語3　　　　　　　 ; CH：Channel（測定チャネル）。CH0〜CH7はADCの入力番号であり、同時測定を意味しない。
      | 用語4　　　　　　　 ; MOSFET：Metal-Oxide-Semiconductor Field-Effect Transistor（金属・酸化膜・半導体構造の電界効果トランジスタ）。ゲートとソースの電圧でドレインとソースの導通を制御する素子。N-MOSはNチャネル型を表す。
      | 用語5　　　　　　　 ; PV：Photovoltaic（太陽光発電）。光を電気へ変える発電方式。PVを含むネット名は太陽電池側の測定・電力経路を表す。
      | 用語6　　　　　　　 ; GND：Ground（回路の基準電位・電流帰路）。この図の共通基準。保護接地や大地への接続を意味するとは限らない。
      | 用語7　　　　　　　 ; VIN/VOUT：入力電圧・出力電圧を表す端子／ネット名。INは入力、OUTは出力。電源変換器の電力端子なのか、検出用端子なのかは対象部品によって異なるため、端子と接続の説明に従う。
      | 用語8　　　　　　　 ; IP/IM・KP/KM：4端子シャントの端子役割を区別する設計上の表記。IP/IMは主電流端子、KP/KMはKelvin（4端子測定）の検出端子。P/Mは正側・負側の区別であり、端子番号は採用部品の割当を参照する。
      | 用語9　　　　　　　 ; IN+/IN−：差動測定の正側・負側入力。電流検出アンプは両端子の電圧差を読む。IN−は必ずGNDという意味ではない。
  MeasureLabel_R2_IL_SENSE_M : ConnectionLabel  Description=|  Label=IL_SENSE_M
      | この回路での名前　　; IL_SENSE_M
      | 種別　　　　　　　　; ConnectionLabel
      | この回路での役割　　; 主インダクタL1直後のシャントR2のマイナス側ケルビン端子KMから、電流検出アンプU3のIN−へ電圧を伝える測定用の枝線。理想モデルではVOUTと同電位だが、図では測定用ケルビン接続として区別している。
      | この場所の直接接続　; C13（出力バルク／470 uF）: 1(p)
      |                     ; C14（出力バルク／470 uF）: 1(p)
      |                     ; C15（出力高速バイパス／10 uF）: 1(p)
      |                     ; C16（出力高速バイパス／10 uF）: 1(p)
      |                     ; R2（L1直後の出力電流を検出する4端子シャント抵抗／CSS4J-4026R-1L00F）: IM, KM
      | 直接接続の範囲　　　; このラベルから実際の線・分岐・明示的な境界端子だけを追った接続。同名ラベルによる離れた場所への接続はこの欄に含めない。
      | 同一ネットの主接続　; R2（L1直後の出力電流を検出する4端子シャント抵抗／CSS4J-4026R-1L00F）: IM, KM
      |                     ; U3（L1直後の出力電流の検出アンプ／INA241A3IDDFR）: 1(IN-)
      | 部品を介する経路　　; R2のKP/KM両端→U3のIN+/IN−→U3 OUT→R26/C25→U1 CH3。R2より下流に出力コンデンサがあるため、過渡時の電池端子電流と常時同一ではない。
      | 同一ネット全端子　　; C13: 1(p)
      |                     ; C14: 1(p)
      |                     ; C15: 1(p)
      |                     ; C16: 1(p)
      |                     ; P_Q1: D
      |                     ; P_R1: 1
      |                     ; P_R4: 1
      |                     ; R2: IM, KM
      |                     ; R19: 1
      |                     ; U3: 1(IN-)
      | 接続部品数　　　　　; 10部品（部品番号で集計。同一ネット全体）
      | 接続端子数　　　　　; 11端子（423端子の部品対応表で集計。ラベル・境界ポートの重複は含めない）
      | この場所の端子数　　; 6端子／5部品（同名ラベルによる接続を除く）
      | 同階層同名ラベル数　; 2個（このラベル自身を含む）
      | 全階層の接続ラベル　; 5個（実際に同じノードへつながるラベル。名前が違う別名も含む）
      | 接続ルール　　　　　; 同じ階層の同じラベル名を仮想配線として結ぶ。別のSubsystem内とは名前だけでつながらず、明示的なConnection Portと配線をたどる。色は用途の表示であり接続を決めない。
      | 確認の範囲　　　　　; 現在の保存回路の端子・配線から求めた静的接続。抵抗やICの内部を導線として短絡せずに集計した。説明の更新は動作シミュレーション、タイミング、実部品の性能・実機動作を保証するものではない。
      | 記録の基準　　　　　; measurement_label_layout_20261022_r01/after_layout_graph.json。部品対応表は端子名の対応付けにのみ使用。
      | 
      | 【この説明欄の略語・記号】
      | 用語1　　　　　　　 ; ADC：Analog-to-Digital Converter（アナログ・デジタル変換器）。測定電圧をデジタル値へ変換する回路。電流や温度も、センサーで電圧へ変換した後に読み取る。
      | 用語2　　　　　　　 ; IC：Integrated Circuit（集積回路）。複数の電子素子と機能を小さな半導体チップに集積した部品。
      | 用語3　　　　　　　 ; CH：Channel（測定チャネル）。CH0〜CH7はADCの入力番号であり、同時測定を意味しない。
      | 用語4　　　　　　　 ; GND：Ground（回路の基準電位・電流帰路）。この図の共通基準。保護接地や大地への接続を意味するとは限らない。
      | 用語5　　　　　　　 ; VIN/VOUT：入力電圧・出力電圧を表す端子／ネット名。INは入力、OUTは出力。電源変換器の電力端子なのか、検出用端子なのかは対象部品によって異なるため、端子と接続の説明に従う。
      | 用語6　　　　　　　 ; IP/IM・KP/KM：4端子シャントの端子役割を区別する設計上の表記。IP/IMは主電流端子、KP/KMはKelvin（4端子測定）の検出端子。P/Mは正側・負側の区別であり、端子番号は採用部品の割当を参照する。
      | 用語7　　　　　　　 ; IN+/IN−：差動測定の正側・負側入力。電流検出アンプは両端子の電圧差を読む。IN−は必ずGNDという意味ではない。
  MeasureLabel_R2_IL_SENSE_P : ConnectionLabel  Description=|  Label=IL_SENSE_P
      | この回路での名前　　; IL_SENSE_P
      | 種別　　　　　　　　; ConnectionLabel
      | この回路での役割　　; 主インダクタL1直後のシャントR2のプラス側ケルビン端子KPから、電流検出アンプU3のIN+へ電圧を伝える測定用の枝線。R2を流れるL1出力電流を調べるための入力。
      | この場所の直接接続　; L1（Q1/Q2のスイッチング電圧を受け、電流の変化を抑えながら出力へエネルギーを渡す／200 uH）: 2(n)
      |                     ; R2（L1直後の出力電流を検出する4端子シャント抵抗／CSS4J-4026R-1L00F）: IP, KP
      | 直接接続の範囲　　　; このラベルから実際の線・分岐・明示的な境界端子だけを追った接続。同名ラベルによる離れた場所への接続はこの欄に含めない。
      | 同一ネットの主接続　; R2（L1直後の出力電流を検出する4端子シャント抵抗／CSS4J-4026R-1L00F）: IP, KP
      |                     ; U3（L1直後の出力電流の検出アンプ／INA241A3IDDFR）: 8(IN+)
      |                     ; L1（Q1/Q2のスイッチング電圧を受け、電流の変化を抑えながら出力へエネルギーを渡す／200 uH）: 2(n)
      | 部品を介する経路　　; R2のKP/KM両端→U3のIN+/IN−→U3 OUT→R26/C25→U1 CH3。R2より下流に出力コンデンサがあるため、過渡時の電池端子電流と常時同一ではない。
      | 同一ネット全端子　　; L1: 2(n)
      |                     ; R2: IP, KP
      |                     ; U3: 8(IN+)
      | 接続部品数　　　　　; 3部品（部品番号で集計。同一ネット全体）
      | 接続端子数　　　　　; 4端子（423端子の部品対応表で集計。ラベル・境界ポートの重複は含めない）
      | この場所の端子数　　; 3端子／2部品（同名ラベルによる接続を除く）
      | 同階層同名ラベル数　; 2個（このラベル自身を含む）
      | 全階層の接続ラベル　; 2個（実際に同じノードへつながるラベル。名前が違う別名も含む）
      | 接続ルール　　　　　; 同じ階層の同じラベル名を仮想配線として結ぶ。別のSubsystem内とは名前だけでつながらず、明示的なConnection Portと配線をたどる。色は用途の表示であり接続を決めない。
      | 確認の範囲　　　　　; 現在の保存回路の端子・配線から求めた静的接続。抵抗やICの内部を導線として短絡せずに集計した。説明の更新は動作シミュレーション、タイミング、実部品の性能・実機動作を保証するものではない。
      | 記録の基準　　　　　; measurement_label_layout_20261022_r01/after_layout_graph.json。部品対応表は端子名の対応付けにのみ使用。
      | 
      | 【この説明欄の略語・記号】
      | 用語1　　　　　　　 ; ADC：Analog-to-Digital Converter（アナログ・デジタル変換器）。測定電圧をデジタル値へ変換する回路。電流や温度も、センサーで電圧へ変換した後に読み取る。
      | 用語2　　　　　　　 ; IC：Integrated Circuit（集積回路）。複数の電子素子と機能を小さな半導体チップに集積した部品。
      | 用語3　　　　　　　 ; CH：Channel（測定チャネル）。CH0〜CH7はADCの入力番号であり、同時測定を意味しない。
      | 用語4　　　　　　　 ; GND：Ground（回路の基準電位・電流帰路）。この図の共通基準。保護接地や大地への接続を意味するとは限らない。
      | 用語5　　　　　　　 ; IP/IM・KP/KM：4端子シャントの端子役割を区別する設計上の表記。IP/IMは主電流端子、KP/KMはKelvin（4端子測定）の検出端子。P/Mは正側・負側の区別であり、端子番号は採用部品の割当を参照する。
      | 用語6　　　　　　　 ; IN+/IN−：差動測定の正側・負側入力。電流検出アンプは両端子の電圧差を読む。IN−は必ずGNDという意味ではない。
  MeasureLabel_U1_ADC_IL : ConnectionLabel  Description=|  Label=ADC_IL
      | この回路での名前　　; ADC_IL
      | 種別　　　　　　　　; ConnectionLabel
      | この回路での役割　　; L1直後の電流検出アンプU3の出力を、R26とC25のRCフィルタに通してADC U1のCH3へ渡す。R2より下流に出力コンデンサがあるため、過渡時の電池端子電流と常に同じ量ではない。
      | この場所の直接接続　; U1（外付けADC／MCP3208-CI/SL）: 4(CH3)
      | 直接接続の範囲　　　; このラベルから実際の線・分岐・明示的な境界端子だけを追った接続。同名ラベルによる離れた場所への接続はこの欄に含めない。
      | 同一ネットの主接続　; R26（L1出力電流の測定信号を整えるRCフィルタの直列抵抗／100 ohm 0.1%）: 2
      |                     ; C25（L1出力電流の測定信号を平滑するコンデンサ／100 nF）: 1
      |                     ; U1（外付けADC／MCP3208-CI/SL）: 4(CH3)
      | 同一ネット全端子　　; C25: 1
      |                     ; R26: 2
      |                     ; U1: 4(CH3)
      | 接続部品数　　　　　; 3部品（部品番号で集計。同一ネット全体）
      | 接続端子数　　　　　; 3端子（423端子の部品対応表で集計。ラベル・境界ポートの重複は含めない）
      | この場所の端子数　　; 1端子／1部品（同名ラベルによる接続を除く）
      | 同階層同名ラベル数　; 2個（このラベル自身を含む）
      | 全階層の接続ラベル　; 2個（実際に同じノードへつながるラベル。名前が違う別名も含む）
      | 接続ルール　　　　　; 同じ階層の同じラベル名を仮想配線として結ぶ。別のSubsystem内とは名前だけでつながらず、明示的なConnection Portと配線をたどる。色は用途の表示であり接続を決めない。
      | 確認の範囲　　　　　; 現在の保存回路の端子・配線から求めた静的接続。抵抗やICの内部を導線として短絡せずに集計した。説明の更新は動作シミュレーション、タイミング、実部品の性能・実機動作を保証するものではない。
      | 記録の基準　　　　　; measurement_label_layout_20261022_r01/after_layout_graph.json。部品対応表は端子名の対応付けにのみ使用。
      | 
      | 【この説明欄の略語・記号】
      | 用語1　　　　　　　 ; ADC：Analog-to-Digital Converter（アナログ・デジタル変換器）。測定電圧をデジタル値へ変換する回路。電流や温度も、センサーで電圧へ変換した後に読み取る。
      | 用語2　　　　　　　 ; IC：Integrated Circuit（集積回路）。複数の電子素子と機能を小さな半導体チップに集積した部品。
      | 用語3　　　　　　　 ; CH：Channel（測定チャネル）。CH0〜CH7はADCの入力番号であり、同時測定を意味しない。
      | 用語4　　　　　　　 ; RC：Resistor-Capacitor（抵抗とコンデンサの組合せ）。主に測定信号のフィルタや時定数を作る。カットオフ周波数は実際の接続と抵抗・容量から求める。
  MeasureLabel_U1_ADC_TBAT : ConnectionLabel  Description=|  Label=ADC_TBAT
      | この回路での名前　　; ADC_TBAT
      | 種別　　　　　　　　; ConnectionLabel
      | この回路での役割　　; 電池付近の温度センサーU4の出力を、R28とC27のRC回路に通してADC U1のCH4へ渡す。温度を表す電圧信号であり、電池端子電圧を測るADC_VBATとは役割が異なる。
      | この場所の直接接続　; U1（外付けADC／MCP3208-CI/SL）: 5(CH4)
      | 直接接続の範囲　　　; このラベルから実際の線・分岐・明示的な境界端子だけを追った接続。同名ラベルによる離れた場所への接続はこの欄に含めない。
      | 同一ネットの主接続　; R28（電池温度の測定信号を整えるRC回路の直列抵抗／47 ohm）: 2
      |                     ; C27（電池温度の測定信号を整えるコンデンサ／680 pF）: 1
      |                     ; U1（外付けADC／MCP3208-CI/SL）: 5(CH4)
      | 同一ネット全端子　　; C27: 1
      |                     ; R28: 2
      |                     ; U1: 5(CH4)
      | 接続部品数　　　　　; 3部品（部品番号で集計。同一ネット全体）
      | 接続端子数　　　　　; 3端子（423端子の部品対応表で集計。ラベル・境界ポートの重複は含めない）
      | この場所の端子数　　; 1端子／1部品（同名ラベルによる接続を除く）
      | 同階層同名ラベル数　; 2個（このラベル自身を含む）
      | 全階層の接続ラベル　; 2個（実際に同じノードへつながるラベル。名前が違う別名も含む）
      | 接続ルール　　　　　; 同じ階層の同じラベル名を仮想配線として結ぶ。別のSubsystem内とは名前だけでつながらず、明示的なConnection Portと配線をたどる。色は用途の表示であり接続を決めない。
      | 確認の範囲　　　　　; 現在の保存回路の端子・配線から求めた静的接続。抵抗やICの内部を導線として短絡せずに集計した。説明の更新は動作シミュレーション、タイミング、実部品の性能・実機動作を保証するものではない。
      | 記録の基準　　　　　; measurement_label_layout_20261022_r01/after_layout_graph.json。部品対応表は端子名の対応付けにのみ使用。
      | 
      | 【この説明欄の略語・記号】
      | 用語1　　　　　　　 ; ADC：Analog-to-Digital Converter（アナログ・デジタル変換器）。測定電圧をデジタル値へ変換する回路。電流や温度も、センサーで電圧へ変換した後に読み取る。
      | 用語2　　　　　　　 ; IC：Integrated Circuit（集積回路）。複数の電子素子と機能を小さな半導体チップに集積した部品。
      | 用語3　　　　　　　 ; CH：Channel（測定チャネル）。CH0〜CH7はADCの入力番号であり、同時測定を意味しない。
      | 用語4　　　　　　　 ; RC：Resistor-Capacitor（抵抗とコンデンサの組合せ）。主に測定信号のフィルタや時定数を作る。カットオフ周波数は実際の接続と抵抗・容量から求める。
  MeasureLabel_U1_ADC_TSINK : ConnectionLabel  Description=|  Label=ADC_TSINK
      | この回路での名前　　; ADC_TSINK
      | 種別　　　　　　　　; ConnectionLabel
      | この回路での役割　　; 放熱器付近の温度センサーU5の出力を、R29とC29のRC回路に通してADC U1のCH5へ渡す。温度を表す電圧信号を読み取る経路。
      | この場所の直接接続　; U1（外付けADC／MCP3208-CI/SL）: 6(CH5)
      | 直接接続の範囲　　　; このラベルから実際の線・分岐・明示的な境界端子だけを追った接続。同名ラベルによる離れた場所への接続はこの欄に含めない。
      | 同一ネットの主接続　; R29（放熱器温度の測定信号を整えるRC回路の直列抵抗／47 ohm）: 2
      |                     ; C29（放熱器温度の測定信号を整えるコンデンサ／680 pF）: 1
      |                     ; U1（外付けADC／MCP3208-CI/SL）: 6(CH5)
      | 同一ネット全端子　　; C29: 1
      |                     ; R29: 2
      |                     ; U1: 6(CH5)
      | 接続部品数　　　　　; 3部品（部品番号で集計。同一ネット全体）
      | 接続端子数　　　　　; 3端子（423端子の部品対応表で集計。ラベル・境界ポートの重複は含めない）
      | この場所の端子数　　; 1端子／1部品（同名ラベルによる接続を除く）
      | 同階層同名ラベル数　; 2個（このラベル自身を含む）
      | 全階層の接続ラベル　; 2個（実際に同じノードへつながるラベル。名前が違う別名も含む）
      | 接続ルール　　　　　; 同じ階層の同じラベル名を仮想配線として結ぶ。別のSubsystem内とは名前だけでつながらず、明示的なConnection Portと配線をたどる。色は用途の表示であり接続を決めない。
      | 確認の範囲　　　　　; 現在の保存回路の端子・配線から求めた静的接続。抵抗やICの内部を導線として短絡せずに集計した。説明の更新は動作シミュレーション、タイミング、実部品の性能・実機動作を保証するものではない。
      | 記録の基準　　　　　; measurement_label_layout_20261022_r01/after_layout_graph.json。部品対応表は端子名の対応付けにのみ使用。
      | 
      | 【この説明欄の略語・記号】
      | 用語1　　　　　　　 ; ADC：Analog-to-Digital Converter（アナログ・デジタル変換器）。測定電圧をデジタル値へ変換する回路。電流や温度も、センサーで電圧へ変換した後に読み取る。
      | 用語2　　　　　　　 ; IC：Integrated Circuit（集積回路）。複数の電子素子と機能を小さな半導体チップに集積した部品。
      | 用語3　　　　　　　 ; CH：Channel（測定チャネル）。CH0〜CH7はADCの入力番号であり、同時測定を意味しない。
      | 用語4　　　　　　　 ; RC：Resistor-Capacitor（抵抗とコンデンサの組合せ）。主に測定信号のフィルタや時定数を作る。カットオフ周波数は実際の接続と抵抗・容量から求める。
  MeasureLabel_U1_VREF2V5_ADC : ConnectionLabel  Description=|  Label=VREF2V5_ADC
      | この回路での名前　　; VREF2V5_ADC
      | 種別　　　　　　　　; ConnectionLabel
      | この回路での役割　　; 基準電圧IC U6のOUTから、ADC U1のVREFと電流検出アンプU2・U3のREF1へ2.5V基準を分配する。3.3V給電とは別の測定基準。R30の入力側も同じノードで、C31の上端にはR30を介してつながる。
      | この場所の直接接続　; U1（外付けADC／MCP3208-CI/SL）: 15(VREF)
      | 直接接続の範囲　　　; このラベルから実際の線・分岐・明示的な境界端子だけを追った接続。同名ラベルによる離れた場所への接続はこの欄に含めない。
      | 同一ネットの主接続　; U6（2.5Vの測定基準電圧源／REF3025EAIDBZR）: 2(OUT)
      |                     ; U1（外付けADC／MCP3208-CI/SL）: 15(VREF)
      |                     ; U2（PV入力電流の検出アンプ／INA241A3IDDFR）: 7(REF1)
      |                     ; U3（L1直後の出力電流の検出アンプ／INA241A3IDDFR）: 7(REF1)
      |                     ; R30（基準電圧出力のコンデンサ枝路に入る直列抵抗／0.1 ohm 1%）: 1
      | 部品を介する経路　　; U6 OUT→R30→C31→GNDは基準電圧出力のコンデンサ枝路。R30の両端は別ノードであり、このラベルはR30入力側へ接続する。
      | 同一ネット全端子　　; R30: 1
      |                     ; U1: 15(VREF)
      |                     ; U2: 7(REF1)
      |                     ; U3: 7(REF1)
      |                     ; U6: 2(OUT)
      | 接続部品数　　　　　; 5部品（部品番号で集計。同一ネット全体）
      | 接続端子数　　　　　; 5端子（423端子の部品対応表で集計。ラベル・境界ポートの重複は含めない）
      | この場所の端子数　　; 1端子／1部品（同名ラベルによる接続を除く）
      | 同階層同名ラベル数　; 4個（このラベル自身を含む）
      | 全階層の接続ラベル　; 4個（実際に同じノードへつながるラベル。名前が違う別名も含む）
      | 接続ルール　　　　　; 同じ階層の同じラベル名を仮想配線として結ぶ。別のSubsystem内とは名前だけでつながらず、明示的なConnection Portと配線をたどる。色は用途の表示であり接続を決めない。
      | 確認の範囲　　　　　; 現在の保存回路の端子・配線から求めた静的接続。抵抗やICの内部を導線として短絡せずに集計した。説明の更新は動作シミュレーション、タイミング、実部品の性能・実機動作を保証するものではない。
      | 記録の基準　　　　　; measurement_label_layout_20261022_r01/after_layout_graph.json。部品対応表は端子名の対応付けにのみ使用。
      | 
      | 【この説明欄の略語・記号】
      | 用語1　　　　　　　 ; ADC：Analog-to-Digital Converter（アナログ・デジタル変換器）。測定電圧をデジタル値へ変換する回路。電流や温度も、センサーで電圧へ変換した後に読み取る。
      | 用語2　　　　　　　 ; IC：Integrated Circuit（集積回路）。複数の電子素子と機能を小さな半導体チップに集積した部品。
      | 用語3　　　　　　　 ; PV：Photovoltaic（太陽光発電）。光を電気へ変える発電方式。PVを含むネット名は太陽電池側の測定・電力経路を表す。
      | 用語4　　　　　　　 ; GND：Ground（回路の基準電位・電流帰路）。この図の共通基準。保護接地や大地への接続を意味するとは限らない。
      | 用語5　　　　　　　 ; VREF/REF：基準電圧を表す端子名。REFはReference（基準）の意味。ADCの変換尺度や電流アンプの出力基準に使う。REF1/REF2の接続電位は個別に確認する。
  MeasureLabel_U3_IL_SENSE_M : ConnectionLabel  Description=|  Label=IL_SENSE_M
      | この回路での名前　　; IL_SENSE_M
      | 種別　　　　　　　　; ConnectionLabel
      | この回路での役割　　; 主インダクタL1直後のシャントR2のマイナス側ケルビン端子KMから、電流検出アンプU3のIN−へ電圧を伝える測定用の枝線。理想モデルではVOUTと同電位だが、図では測定用ケルビン接続として区別している。
      | この場所の直接接続　; U3（L1直後の出力電流の検出アンプ／INA241A3IDDFR）: 1(IN-)
      | 直接接続の範囲　　　; このラベルから実際の線・分岐・明示的な境界端子だけを追った接続。同名ラベルによる離れた場所への接続はこの欄に含めない。
      | 同一ネットの主接続　; R2（L1直後の出力電流を検出する4端子シャント抵抗／CSS4J-4026R-1L00F）: IM, KM
      |                     ; U3（L1直後の出力電流の検出アンプ／INA241A3IDDFR）: 1(IN-)
      | 部品を介する経路　　; R2のKP/KM両端→U3のIN+/IN−→U3 OUT→R26/C25→U1 CH3。R2より下流に出力コンデンサがあるため、過渡時の電池端子電流と常時同一ではない。
      | 同一ネット全端子　　; C13: 1(p)
      |                     ; C14: 1(p)
      |                     ; C15: 1(p)
      |                     ; C16: 1(p)
      |                     ; P_Q1: D
      |                     ; P_R1: 1
      |                     ; P_R4: 1
      |                     ; R2: IM, KM
      |                     ; R19: 1
      |                     ; U3: 1(IN-)
      | 接続部品数　　　　　; 10部品（部品番号で集計。同一ネット全体）
      | 接続端子数　　　　　; 11端子（423端子の部品対応表で集計。ラベル・境界ポートの重複は含めない）
      | この場所の端子数　　; 1端子／1部品（同名ラベルによる接続を除く）
      | 同階層同名ラベル数　; 2個（このラベル自身を含む）
      | 全階層の接続ラベル　; 5個（実際に同じノードへつながるラベル。名前が違う別名も含む）
      | 接続ルール　　　　　; 同じ階層の同じラベル名を仮想配線として結ぶ。別のSubsystem内とは名前だけでつながらず、明示的なConnection Portと配線をたどる。色は用途の表示であり接続を決めない。
      | 確認の範囲　　　　　; 現在の保存回路の端子・配線から求めた静的接続。抵抗やICの内部を導線として短絡せずに集計した。説明の更新は動作シミュレーション、タイミング、実部品の性能・実機動作を保証するものではない。
      | 記録の基準　　　　　; measurement_label_layout_20261022_r01/after_layout_graph.json。部品対応表は端子名の対応付けにのみ使用。
      | 
      | 【この説明欄の略語・記号】
      | 用語1　　　　　　　 ; ADC：Analog-to-Digital Converter（アナログ・デジタル変換器）。測定電圧をデジタル値へ変換する回路。電流や温度も、センサーで電圧へ変換した後に読み取る。
      | 用語2　　　　　　　 ; IC：Integrated Circuit（集積回路）。複数の電子素子と機能を小さな半導体チップに集積した部品。
      | 用語3　　　　　　　 ; CH：Channel（測定チャネル）。CH0〜CH7はADCの入力番号であり、同時測定を意味しない。
      | 用語4　　　　　　　 ; GND：Ground（回路の基準電位・電流帰路）。この図の共通基準。保護接地や大地への接続を意味するとは限らない。
      | 用語5　　　　　　　 ; VIN/VOUT：入力電圧・出力電圧を表す端子／ネット名。INは入力、OUTは出力。電源変換器の電力端子なのか、検出用端子なのかは対象部品によって異なるため、端子と接続の説明に従う。
      | 用語6　　　　　　　 ; IP/IM・KP/KM：4端子シャントの端子役割を区別する設計上の表記。IP/IMは主電流端子、KP/KMはKelvin（4端子測定）の検出端子。P/Mは正側・負側の区別であり、端子番号は採用部品の割当を参照する。
      | 用語7　　　　　　　 ; IN+/IN−：差動測定の正側・負側入力。電流検出アンプは両端子の電圧差を読む。IN−は必ずGNDという意味ではない。
  MeasureLabel_U3_IL_SENSE_P : ConnectionLabel  Description=|  Label=IL_SENSE_P
      | この回路での名前　　; IL_SENSE_P
      | 種別　　　　　　　　; ConnectionLabel
      | この回路での役割　　; 主インダクタL1直後のシャントR2のプラス側ケルビン端子KPから、電流検出アンプU3のIN+へ電圧を伝える測定用の枝線。R2を流れるL1出力電流を調べるための入力。
      | この場所の直接接続　; U3（L1直後の出力電流の検出アンプ／INA241A3IDDFR）: 8(IN+)
      | 直接接続の範囲　　　; このラベルから実際の線・分岐・明示的な境界端子だけを追った接続。同名ラベルによる離れた場所への接続はこの欄に含めない。
      | 同一ネットの主接続　; R2（L1直後の出力電流を検出する4端子シャント抵抗／CSS4J-4026R-1L00F）: IP, KP
      |                     ; U3（L1直後の出力電流の検出アンプ／INA241A3IDDFR）: 8(IN+)
      |                     ; L1（Q1/Q2のスイッチング電圧を受け、電流の変化を抑えながら出力へエネルギーを渡す／200 uH）: 2(n)
      | 部品を介する経路　　; R2のKP/KM両端→U3のIN+/IN−→U3 OUT→R26/C25→U1 CH3。R2より下流に出力コンデンサがあるため、過渡時の電池端子電流と常時同一ではない。
      | 同一ネット全端子　　; L1: 2(n)
      |                     ; R2: IP, KP
      |                     ; U3: 8(IN+)
      | 接続部品数　　　　　; 3部品（部品番号で集計。同一ネット全体）
      | 接続端子数　　　　　; 4端子（423端子の部品対応表で集計。ラベル・境界ポートの重複は含めない）
      | この場所の端子数　　; 1端子／1部品（同名ラベルによる接続を除く）
      | 同階層同名ラベル数　; 2個（このラベル自身を含む）
      | 全階層の接続ラベル　; 2個（実際に同じノードへつながるラベル。名前が違う別名も含む）
      | 接続ルール　　　　　; 同じ階層の同じラベル名を仮想配線として結ぶ。別のSubsystem内とは名前だけでつながらず、明示的なConnection Portと配線をたどる。色は用途の表示であり接続を決めない。
      | 確認の範囲　　　　　; 現在の保存回路の端子・配線から求めた静的接続。抵抗やICの内部を導線として短絡せずに集計した。説明の更新は動作シミュレーション、タイミング、実部品の性能・実機動作を保証するものではない。
      | 記録の基準　　　　　; measurement_label_layout_20261022_r01/after_layout_graph.json。部品対応表は端子名の対応付けにのみ使用。
      | 
      | 【この説明欄の略語・記号】
      | 用語1　　　　　　　 ; ADC：Analog-to-Digital Converter（アナログ・デジタル変換器）。測定電圧をデジタル値へ変換する回路。電流や温度も、センサーで電圧へ変換した後に読み取る。
      | 用語2　　　　　　　 ; IC：Integrated Circuit（集積回路）。複数の電子素子と機能を小さな半導体チップに集積した部品。
      | 用語3　　　　　　　 ; CH：Channel（測定チャネル）。CH0〜CH7はADCの入力番号であり、同時測定を意味しない。
      | 用語4　　　　　　　 ; GND：Ground（回路の基準電位・電流帰路）。この図の共通基準。保護接地や大地への接続を意味するとは限らない。
      | 用語5　　　　　　　 ; IP/IM・KP/KM：4端子シャントの端子役割を区別する設計上の表記。IP/IMは主電流端子、KP/KMはKelvin（4端子測定）の検出端子。P/Mは正側・負側の区別であり、端子番号は採用部品の割当を参照する。
      | 用語6　　　　　　　 ; IN+/IN−：差動測定の正側・負側入力。電流検出アンプは両端子の電圧差を読む。IN−は必ずGNDという意味ではない。
  MeasureLabel_U3_VREF2V5_ADC : ConnectionLabel  Description=|  Label=VREF2V5_ADC
      | この回路での名前　　; VREF2V5_ADC
      | 種別　　　　　　　　; ConnectionLabel
      | この回路での役割　　; 基準電圧IC U6のOUTから、ADC U1のVREFと電流検出アンプU2・U3のREF1へ2.5V基準を分配する。3.3V給電とは別の測定基準。R30の入力側も同じノードで、C31の上端にはR30を介してつながる。
      | この場所の直接接続　; U3（L1直後の出力電流の検出アンプ／INA241A3IDDFR）: 7(REF1)
      | 直接接続の範囲　　　; このラベルから実際の線・分岐・明示的な境界端子だけを追った接続。同名ラベルによる離れた場所への接続はこの欄に含めない。
      | 同一ネットの主接続　; U6（2.5Vの測定基準電圧源／REF3025EAIDBZR）: 2(OUT)
      |                     ; U1（外付けADC／MCP3208-CI/SL）: 15(VREF)
      |                     ; U2（PV入力電流の検出アンプ／INA241A3IDDFR）: 7(REF1)
      |                     ; U3（L1直後の出力電流の検出アンプ／INA241A3IDDFR）: 7(REF1)
      |                     ; R30（基準電圧出力のコンデンサ枝路に入る直列抵抗／0.1 ohm 1%）: 1
      | 部品を介する経路　　; U6 OUT→R30→C31→GNDは基準電圧出力のコンデンサ枝路。R30の両端は別ノードであり、このラベルはR30入力側へ接続する。
      | 同一ネット全端子　　; R30: 1
      |                     ; U1: 15(VREF)
      |                     ; U2: 7(REF1)
      |                     ; U3: 7(REF1)
      |                     ; U6: 2(OUT)
      | 接続部品数　　　　　; 5部品（部品番号で集計。同一ネット全体）
      | 接続端子数　　　　　; 5端子（423端子の部品対応表で集計。ラベル・境界ポートの重複は含めない）
      | この場所の端子数　　; 1端子／1部品（同名ラベルによる接続を除く）
      | 同階層同名ラベル数　; 4個（このラベル自身を含む）
      | 全階層の接続ラベル　; 4個（実際に同じノードへつながるラベル。名前が違う別名も含む）
      | 接続ルール　　　　　; 同じ階層の同じラベル名を仮想配線として結ぶ。別のSubsystem内とは名前だけでつながらず、明示的なConnection Portと配線をたどる。色は用途の表示であり接続を決めない。
      | 確認の範囲　　　　　; 現在の保存回路の端子・配線から求めた静的接続。抵抗やICの内部を導線として短絡せずに集計した。説明の更新は動作シミュレーション、タイミング、実部品の性能・実機動作を保証するものではない。
      | 記録の基準　　　　　; measurement_label_layout_20261022_r01/after_layout_graph.json。部品対応表は端子名の対応付けにのみ使用。
      | 
      | 【この説明欄の略語・記号】
      | 用語1　　　　　　　 ; ADC：Analog-to-Digital Converter（アナログ・デジタル変換器）。測定電圧をデジタル値へ変換する回路。電流や温度も、センサーで電圧へ変換した後に読み取る。
      | 用語2　　　　　　　 ; IC：Integrated Circuit（集積回路）。複数の電子素子と機能を小さな半導体チップに集積した部品。
      | 用語3　　　　　　　 ; PV：Photovoltaic（太陽光発電）。光を電気へ変える発電方式。PVを含むネット名は太陽電池側の測定・電力経路を表す。
      | 用語4　　　　　　　 ; GND：Ground（回路の基準電位・電流帰路）。この図の共通基準。保護接地や大地への接続を意味するとは限らない。
      | 用語5　　　　　　　 ; VREF/REF：基準電圧を表す端子名。REFはReference（基準）の意味。ADCの変換尺度や電流アンプの出力基準に使う。REF1/REF2の接続電位は個別に確認する。
  MeasureLabel_U6_VREF2V5_ADC : ConnectionLabel  Description=|  Label=VREF2V5_ADC
      | この回路での名前　　; VREF2V5_ADC
      | 種別　　　　　　　　; ConnectionLabel
      | この回路での役割　　; 基準電圧IC U6のOUTから、ADC U1のVREFと電流検出アンプU2・U3のREF1へ2.5V基準を分配する。3.3V給電とは別の測定基準。R30の入力側も同じノードで、C31の上端にはR30を介してつながる。
      | この場所の直接接続　; R30（基準電圧出力のコンデンサ枝路に入る直列抵抗／0.1 ohm 1%）: 1
      |                     ; U6（2.5Vの測定基準電圧源／REF3025EAIDBZR）: 2(OUT)
      | 直接接続の範囲　　　; このラベルから実際の線・分岐・明示的な境界端子だけを追った接続。同名ラベルによる離れた場所への接続はこの欄に含めない。
      | 同一ネットの主接続　; U6（2.5Vの測定基準電圧源／REF3025EAIDBZR）: 2(OUT)
      |                     ; U1（外付けADC／MCP3208-CI/SL）: 15(VREF)
      |                     ; U2（PV入力電流の検出アンプ／INA241A3IDDFR）: 7(REF1)
      |                     ; U3（L1直後の出力電流の検出アンプ／INA241A3IDDFR）: 7(REF1)
      |                     ; R30（基準電圧出力のコンデンサ枝路に入る直列抵抗／0.1 ohm 1%）: 1
      | 部品を介する経路　　; U6 OUT→R30→C31→GNDは基準電圧出力のコンデンサ枝路。R30の両端は別ノードであり、このラベルはR30入力側へ接続する。
      | 同一ネット全端子　　; R30: 1
      |                     ; U1: 15(VREF)
      |                     ; U2: 7(REF1)
      |                     ; U3: 7(REF1)
      |                     ; U6: 2(OUT)
      | 接続部品数　　　　　; 5部品（部品番号で集計。同一ネット全体）
      | 接続端子数　　　　　; 5端子（423端子の部品対応表で集計。ラベル・境界ポートの重複は含めない）
      | この場所の端子数　　; 2端子／2部品（同名ラベルによる接続を除く）
      | 同階層同名ラベル数　; 4個（このラベル自身を含む）
      | 全階層の接続ラベル　; 4個（実際に同じノードへつながるラベル。名前が違う別名も含む）
      | 接続ルール　　　　　; 同じ階層の同じラベル名を仮想配線として結ぶ。別のSubsystem内とは名前だけでつながらず、明示的なConnection Portと配線をたどる。色は用途の表示であり接続を決めない。
      | 確認の範囲　　　　　; 現在の保存回路の端子・配線から求めた静的接続。抵抗やICの内部を導線として短絡せずに集計した。説明の更新は動作シミュレーション、タイミング、実部品の性能・実機動作を保証するものではない。
      | 記録の基準　　　　　; measurement_label_layout_20261022_r01/after_layout_graph.json。部品対応表は端子名の対応付けにのみ使用。
      | 
      | 【この説明欄の略語・記号】
      | 用語1　　　　　　　 ; ADC：Analog-to-Digital Converter（アナログ・デジタル変換器）。測定電圧をデジタル値へ変換する回路。電流や温度も、センサーで電圧へ変換した後に読み取る。
      | 用語2　　　　　　　 ; IC：Integrated Circuit（集積回路）。複数の電子素子と機能を小さな半導体チップに集積した部品。
      | 用語3　　　　　　　 ; PV：Photovoltaic（太陽光発電）。光を電気へ変える発電方式。PVを含むネット名は太陽電池側の測定・電力経路を表す。
      | 用語4　　　　　　　 ; GND：Ground（回路の基準電位・電流帰路）。この図の共通基準。保護接地や大地への接続を意味するとは限らない。
      | 用語5　　　　　　　 ; VREF/REF：基準電圧を表す端子名。REFはReference（基準）の意味。ADCの変換尺度や電流アンプの出力基準に使う。REF1/REF2の接続電位は個別に確認する。
  PV1 : Subsystem  Description=|  mask(太陽光充電回路 編集用部品){PartRef=PV1, PartMPN=AXITEC AC-400MH/108V, PartValue=400W panel 1/2, DesignValue=400W panel 1/2, SourceRef=}
      | この回路での名前　　; PV1
      | 部品名　　　　　　　; AXITEC AC-400MH/108V
      | この回路での役割　　; 太陽光を電力へ変え、この充電器へ入力する太陽電池パネルの1枚目。
      | ここでの動き　　　　; PV2と直列に接続して2枚分の電圧を加える。発電量は日射と温度などで変化し、公称400 Wが常に得られる意味ではない。
      | 
      | 【詳しい働き・仕様・接続・確認の範囲】
      | 部品種別　　　　　　; 太陽電池モジュール
      | 公称値　　　　　　　; 400W panel 1/2
      | 配置目的　　　　　　; PV2と直列にして充電器入力の太陽電池列を構成する。
      | 意図する動作　　　　; 400 Wは部品情報上の公称出力であり、常時400 Wを発生するという意味ではない。日射・温度によるI–V変化は別の動作モデルで扱う。
      | 端子と接続　　　　　; + + → PV_SERIES、- - → GND
      | モデルの範囲　　　　; 端子配置・接続確認用の図面ブロック。内部はConnection Portによる端子表現であり、このブロック単体は対象IC/モジュールの電気的機能やソフトウェアを再現しない。
      | 確認の範囲　　　　　; 本説明は保存回路の部品情報・端子割当・既存設計意図を整理したもの。今回の説明更新によって新たな動作試験や実機検証を実施した意味ではない。
      | 設計記録　　　　　　; evaluation\component_annotations_20261022_r01\before_graph.json
      | evaluation\component_annotations_20261022_r01\before_metadata.json
      | evaluation\protection_capacitor_integration_20261021_r01\final_delivery\independent_readback\physical_bom.json
      | 
      | 【この説明欄の略語・記号】
      | 用語1　　　　　　　 ; IC：Integrated Circuit（集積回路）。複数の電子素子と機能を小さな半導体チップに集積した部品。
      | 用語2　　　　　　　 ; PV：Photovoltaic（太陽光発電）。光を電気へ変える発電方式。PVを含むネット名は太陽電池側の測定・電力経路を表す。
      | 用語3　　　　　　　 ; GND：Ground（回路の基準電位・電流帰路）。この図の共通基準。保護接地や大地への接続を意味するとは限らない。
      mask prompts: PartRef "物理部品番号"; PartMPN "部品型番"; PartValue "部品値・表示値"; DesignValue "元設計値（記録）"; SourceRef "旧参照名（記録）"
      mask help: 回路図編集用です。端子・配線は実際のSimscape接続ですが、部品内部の動作式は未実装です。値・型番を変更し、配線をドラッグして編集できます。
      settings: AttributesFormatString=400W panel 1/2
      mask Display:
      | color('black');
      | plot([0 0.42],[0.5 0.5]);
      | plot([0.58 1],[0.5 0.5]);
      | plot([0.42 0.42],[0.14 0.86]);
      | plot([0.58 0.58],[0.3 0.7]);
      | plot([0.19 0.35 0.31],[0.96 0.79 0.92]);
      | plot([0.35 0.23],[0.79 0.83]);
      | plot([0.34 0.5 0.46],[0.96 0.79 0.92]);
      | plot([0.5 0.38],[0.79 0.83]);
      | port_label('rconn',1,'+');
      | port_label('lconn',1,'-');
  PV2 : Subsystem  Description=|  mask(太陽光充電回路 編集用部品){PartRef=PV2, PartMPN=AXITEC AC-400MH/108V, PartValue=400W panel 2/2, DesignValue=400W panel 2/2, SourceRef=}
      | この回路での名前　　; PV2
      | 部品名　　　　　　　; AXITEC AC-400MH/108V
      | この回路での役割　　; 太陽光を電力へ変え、この充電器へ入力する太陽電池パネルの2枚目。
      | ここでの動き　　　　; PV1と直列に接続した列のプラス側から、入力ヒューズF2を通して充電器へ電力を送る。
      | 
      | 【詳しい働き・仕様・接続・確認の範囲】
      | 部品種別　　　　　　; 太陽電池モジュール
      | 公称値　　　　　　　; 400W panel 2/2
      | 配置目的　　　　　　; PV1と直列にして充電器入力の太陽電池列を構成する。
      | 意図する動作　　　　; 400 Wは部品情報上の公称出力。遮光・温度・バイパスダイオードを含む実機挙動はこの端子図だけでは再現しない。
      | 端子と接続　　　　　; + + → PV_RAW、- - → PV_SERIES
      | モデルの範囲　　　　; 端子配置・接続確認用の図面ブロック。内部はConnection Portによる端子表現であり、このブロック単体は対象IC/モジュールの電気的機能やソフトウェアを再現しない。
      | 確認の範囲　　　　　; 本説明は保存回路の部品情報・端子割当・既存設計意図を整理したもの。今回の説明更新によって新たな動作試験や実機検証を実施した意味ではない。
      | 設計記録　　　　　　; evaluation\component_annotations_20261022_r01\before_graph.json
      | evaluation\component_annotations_20261022_r01\before_metadata.json
      | evaluation\protection_capacitor_integration_20261021_r01\final_delivery\independent_readback\physical_bom.json
      | 
      | 【この説明欄の略語・記号】
      | 用語1　　　　　　　 ; IC：Integrated Circuit（集積回路）。複数の電子素子と機能を小さな半導体チップに集積した部品。
      | 用語2　　　　　　　 ; PV：Photovoltaic（太陽光発電）。光を電気へ変える発電方式。PVを含むネット名は太陽電池側の測定・電力経路を表す。
      mask prompts: PartRef "物理部品番号"; PartMPN "部品型番"; PartValue "部品値・表示値"; DesignValue "元設計値（記録）"; SourceRef "旧参照名（記録）"
      mask help: 回路図編集用です。端子・配線は実際のSimscape接続ですが、部品内部の動作式は未実装です。値・型番を変更し、配線をドラッグして編集できます。
      settings: AttributesFormatString=400W panel 2/2
      mask Display:
      | color('black');
      | plot([0 0.42],[0.5 0.5]);
      | plot([0.58 1],[0.5 0.5]);
      | plot([0.42 0.42],[0.14 0.86]);
      | plot([0.58 0.58],[0.3 0.7]);
      | plot([0.19 0.35 0.31],[0.96 0.79 0.92]);
      | plot([0.35 0.23],[0.79 0.83]);
      | plot([0.34 0.5 0.46],[0.96 0.79 0.92]);
      | plot([0.5 0.38],[0.79 0.83]);
      | port_label('rconn',1,'+');
      | port_label('lconn',1,'-');
  PVLabel_ADC_CurrentInput : ConnectionLabel  Description=|  Label=IPV_OUT
      | 接続名              ; IPV_OUT
      | この接続の役割      ; アナログ測定。この階層内の同名ラベルを電気的に結ぶ。
      | この場所の接続先    ; solar_pv_protected_c06_circuit/R25
      | 階層の境界          ; 異なる階層とはConnection Portで明示的に接続する。
      | 同階層の同名接続    ; PVLabel_ADC_CurrentInput、PVLabel_Module_IPV_OUT
      | 実際につながる端子  ; PV_Reverse_Protection (RConn:2)
  PVLabel_Input : ConnectionLabel  Description=|  Label=PV_FUSED
      | 接続名              ; PV_FUSED
      | この接続の役割      ; 電源。この階層内の同名ラベルを電気的に結ぶ。
      | この場所の接続先    ; solar_pv_protected_c06_circuit/F2
      | 階層の境界          ; 異なる階層とはConnection Portで明示的に接続する。
      | 同階層の同名接続    ; PVLabel_Input、PVLabel_Voltage_Input
      | 実際につながる端子  ; PV_RV_H1 (LConn:1)
  PVLabel_Module_GND : ConnectionLabel  Description=|  Label=GND
      | 接続名              ; GND
      | この接続の役割      ; 共通GND。この階層内の同名ラベルを電気的に結ぶ。
      | この場所の接続先    ; solar_pv_protected_c06_circuit/PV_Reverse_Protection
      | 階層の境界          ; 異なる階層とはConnection Portで明示的に接続する。
      | 同階層の同名接続    ; GND_Label_001、GND_Label_002、GND_Label_003、GND_Label_006、GND_Label_007、GND_Label_008、GND_Label_009、GND_Label_010、GND_Label_011、GND_Label_012、GND_Label_013、GND_Label_014、GND_Label_015、GND_Label_017、GND_Label_018、GND_Label_019、GND_Label_020、GND_Label_021、GND_Label_022、GND_Label_023、GND_Label_024、GND_Label_025、GND_Label_026、GND_Label_027、GND_Label_028、GND_Label_029、GND_Label_030、GND_Label_031、GND_Label_032、GND_Label_033、GND_Label_034、GND_Label_035、GND_Label_036、GND_Label_037、GND_Label_038、GND_Label_039、GND_Label_040、GND_Label_043、GND_Label_044、GND_Label_045、GND_Label_046、GND_Label_047、GND_Label_049、GND_Label_050、GND_Label_053、GND_Label_054、GND_Label_055、GND_Label_056、GND_Label_057、GND_Label_058、GND_Label_060、GND_Label_064、GND_Label_065、GND_Label_069、GND_Label_080、GND_Label_081、GND_Label_085、GND_Label_086、GND_Label_087、GND_Label_088、GND_Label_089、GND_Label_090、GND_Label_091、GND_Label_092、GND_Label_093、GND_Label_094、GND_Label_095、GND_Label_096、GND_Label_097、GND_Label_098、GND_Label_099、PVLabel_Module_GND、PVLabel_Voltage_CGround、PVLabel_Voltage_RGround、ProtectionNet_RETURN
      | 実際につながる端子  ; BT1 (RConn:1)、C1 (RConn:1)、C10 (RConn:1)、C13 (RConn:1)、C14 (RConn:1)、C15 (RConn:1)、C16 (RConn:1)、C17 (RConn:1)、C18 (RConn:1)、C19 (RConn:1)、C2 (RConn:1)、C20 (RConn:1)、C21 (RConn:1)、C23 (RConn:1)、C24 (RConn:1)、C25 (RConn:1)、C26 (RConn:1)、C27 (RConn:1)、C28 (RConn:1)、C29 (RConn:1)、C3 (RConn:1)、C30 (RConn:1)、C31 (RConn:1)、C33 (RConn:1)、C34 (RConn:1)、C35 (RConn:1)、C36 (RConn:1)、C4 (RConn:1)、C40 (RConn:1)、C41 (RConn:1)、C42 (RConn:1)、C43 (RConn:1)、C44 (RConn:1)、C45 (RConn:1)、C46 (RConn:1)、C47 (RConn:1)、C48 (RConn:1)、C7 (RConn:1)、C8 (RConn:1)、C9 (RConn:1)、LTC4364_Protection (LConn:3)、PV1 (LConn:1)、PV_CV_ADC (RConn:1)、PV_RV_L (RConn:1)、PV_Reverse_Protection (LConn:2)、Q3A (RConn:2)、Q3B (RConn:2)、R1 (RConn:1)、R18 (RConn:1)、R21 (RConn:1)、R24 (RConn:1)、R35 (RConn:1)、R42 (RConn:1)、R48 (RConn:1)、U1 (RConn:3)、U1 (RConn:8)、U11 (LConn:3)、U12 (LConn:2)、U3 (LConn:2)、U3 (LConn:3)、U3 (LConn:4)、U4 (RConn:1)、U5 (RConn:1)、U6 (RConn:1)、U7 (LConn:13)、U7 (LConn:18)、U7 (LConn:3)、U7 (LConn:8)、U7 (RConn:13)、U7 (RConn:18)、U7 (RConn:3)、U7 (RConn:8)、U9 (RConn:3)
  PVLabel_Module_IPV_OUT : ConnectionLabel  Description=|  Label=IPV_OUT
      | 接続名              ; IPV_OUT
      | この接続の役割      ; アナログ測定。この階層内の同名ラベルを電気的に結ぶ。
      | この場所の接続先    ; solar_pv_protected_c06_circuit/PV_Reverse_Protection
      | 階層の境界          ; 異なる階層とはConnection Portで明示的に接続する。
      | 同階層の同名接続    ; PVLabel_ADC_CurrentInput、PVLabel_Module_IPV_OUT
      | 実際につながる端子  ; PV_Reverse_Protection (RConn:2)
  PVLabel_Module_MCU_REARM : ConnectionLabel  Description=|  Label=PV_MCU_REARM
      | 接続名              ; PV_MCU_REARM
      | この接続の役割      ; デジタル制御。この階層内の同名ラベルを電気的に結ぶ。
      | この場所の接続先    ; solar_pv_protected_c06_circuit/PV_Reverse_Protection
      | 階層の境界          ; 異なる階層とはConnection Portで明示的に接続する。
      | 同階層の同名接続    ; PVLabel_Module_MCU_REARM、PVLabel_U7_GP12
      | 実際につながる端子  ; PV_Reverse_Protection (LConn:6)、U7 (LConn:16)
  PVLabel_Module_MCU_RUN : ConnectionLabel  Description=|  Label=PV_MCU_RUN
      | 接続名              ; PV_MCU_RUN
      | この接続の役割      ; デジタル制御。この階層内の同名ラベルを電気的に結ぶ。
      | この場所の接続先    ; solar_pv_protected_c06_circuit/PV_Reverse_Protection
      | 階層の境界          ; 異なる階層とはConnection Portで明示的に接続する。
      | 同階層の同名接続    ; PVLabel_Module_MCU_RUN、PVLabel_U7_GP10
      | 実際につながる端子  ; PV_Reverse_Protection (LConn:5)、U7 (LConn:14)
  PVLabel_Module_OC_FAULT_N : ConnectionLabel  Description=|  Label=PV_OC_FAULT_N
      | 接続名              ; PV_OC_FAULT_N
      | この接続の役割      ; 保護・状態。この階層内の同名ラベルを電気的に結ぶ。
      | この場所の接続先    ; solar_pv_protected_c06_circuit/PV_Reverse_Protection
      | 階層の境界          ; 異なる階層とはConnection Portで明示的に接続する。
      | 同階層の同名接続    ; PVLabel_Module_OC_FAULT_N、PVLabel_U7_GP14
      | 実際につながる端子  ; PV_Reverse_Protection (RConn:3)、U7 (LConn:19)
  PVLabel_Module_P3V3 : ConnectionLabel  Description=|  Label=V3V3
      | 接続名              ; V3V3
      | この接続の役割      ; 電源。この階層内の同名ラベルを電気的に結ぶ。
      | この場所の接続先    ; solar_pv_protected_c06_circuit/PV_Reverse_Protection
      | 階層の境界          ; 異なる階層とはConnection Portで明示的に接続する。
      | 同階層の同名接続    ; PVLabel_Module_P3V3、ProtectionNet_VLOGIC、ReadLabel_R15_V3V3、ReadLabel_R49_V3V3、ReadLabel_U1_V3V3、ReadLabel_U3_V3V3、ReadLabel_U4_V3V3、ReadLabel_U5_V3V3、ReadLabel_U6_V3V3、ReadLabel_U7_V3V3
      | 実際につながる端子  ; LTC4364_Protection (LConn:4)、PV_Reverse_Protection (LConn:3)、R15 (LConn:1)、R49 (RConn:1)、U7 (RConn:5)
  PVLabel_Module_PV_STOPPED : ConnectionLabel  Description=|  Label=PV_STOPPED
      | 接続名              ; PV_STOPPED
      | この接続の役割      ; 保護・状態。この階層内の同名ラベルを電気的に結ぶ。
      | この場所の接続先    ; solar_pv_protected_c06_circuit/PV_Reverse_Protection
      | 階層の境界          ; 異なる階層とはConnection Portで明示的に接続する。
      | 同階層の同名接続    ; PVLabel_Module_PV_STOPPED、PVLabel_U7_GP15
      | 実際につながる端子  ; PV_Reverse_Protection (RConn:4)、U7 (LConn:20)
  PVLabel_Module_VREF2V5 : ConnectionLabel  Description=|  Label=VREF2V5_ADC
      | 接続名              ; VREF2V5_ADC
      | この接続の役割      ; アナログ測定。この階層内の同名ラベルを電気的に結ぶ。
      | この場所の接続先    ; solar_pv_protected_c06_circuit/PV_Reverse_Protection
      | 階層の境界          ; 異なる階層とはConnection Portで明示的に接続する。
      | 同階層の同名接続    ; MeasureLabel_U1_VREF2V5_ADC、MeasureLabel_U3_VREF2V5_ADC、MeasureLabel_U6_VREF2V5_ADC、PVLabel_Module_VREF2V5
      | 実際につながる端子  ; PV_Reverse_Protection (LConn:4)、U1 (RConn:2)、U3 (RConn:2)
  PVLabel_U7_GP10 : ConnectionLabel  Description=|  Label=PV_MCU_RUN
      | 接続名              ; PV_MCU_RUN
      | この接続の役割      ; デジタル制御。この階層内の同名ラベルを電気的に結ぶ。
      | この場所の接続先    ; solar_pv_protected_c06_circuit/U7
      | 階層の境界          ; 異なる階層とはConnection Portで明示的に接続する。
      | 同階層の同名接続    ; PVLabel_Module_MCU_RUN、PVLabel_U7_GP10
      | 実際につながる端子  ; PV_Reverse_Protection (LConn:5)、U7 (LConn:14)
  PVLabel_U7_GP12 : ConnectionLabel  Description=|  Label=PV_MCU_REARM
      | 接続名              ; PV_MCU_REARM
      | この接続の役割      ; デジタル制御。この階層内の同名ラベルを電気的に結ぶ。
      | この場所の接続先    ; solar_pv_protected_c06_circuit/U7
      | 階層の境界          ; 異なる階層とはConnection Portで明示的に接続する。
      | 同階層の同名接続    ; PVLabel_Module_MCU_REARM、PVLabel_U7_GP12
      | 実際につながる端子  ; PV_Reverse_Protection (LConn:6)、U7 (LConn:16)
  PVLabel_U7_GP14 : ConnectionLabel  Description=|  Label=PV_OC_FAULT_N
      | 接続名              ; PV_OC_FAULT_N
      | この接続の役割      ; 保護・状態。この階層内の同名ラベルを電気的に結ぶ。
      | この場所の接続先    ; solar_pv_protected_c06_circuit/U7
      | 階層の境界          ; 異なる階層とはConnection Portで明示的に接続する。
      | 同階層の同名接続    ; PVLabel_Module_OC_FAULT_N、PVLabel_U7_GP14
      | 実際につながる端子  ; PV_Reverse_Protection (RConn:3)、U7 (LConn:19)
  PVLabel_U7_GP15 : ConnectionLabel  Description=|  Label=PV_STOPPED
      | 接続名              ; PV_STOPPED
      | この接続の役割      ; 保護・状態。この階層内の同名ラベルを電気的に結ぶ。
      | この場所の接続先    ; solar_pv_protected_c06_circuit/U7
      | 階層の境界          ; 異なる階層とはConnection Portで明示的に接続する。
      | 同階層の同名接続    ; PVLabel_Module_PV_STOPPED、PVLabel_U7_GP15
      | 実際につながる端子  ; PV_Reverse_Protection (RConn:4)、U7 (LConn:20)
  PVLabel_Voltage_CGround : ConnectionLabel  Description=|  Label=GND
      | 接続名              ; GND
      | この接続の役割      ; 共通GND。この階層内の同名ラベルを電気的に結ぶ。
      | この場所の接続先    ; solar_pv_protected_c06_circuit/PV_CV_ADC
      | 階層の境界          ; 異なる階層とはConnection Portで明示的に接続する。
      | 同階層の同名接続    ; GND_Label_001、GND_Label_002、GND_Label_003、GND_Label_006、GND_Label_007、GND_Label_008、GND_Label_009、GND_Label_010、GND_Label_011、GND_Label_012、GND_Label_013、GND_Label_014、GND_Label_015、GND_Label_017、GND_Label_018、GND_Label_019、GND_Label_020、GND_Label_021、GND_Label_022、GND_Label_023、GND_Label_024、GND_Label_025、GND_Label_026、GND_Label_027、GND_Label_028、GND_Label_029、GND_Label_030、GND_Label_031、GND_Label_032、GND_Label_033、GND_Label_034、GND_Label_035、GND_Label_036、GND_Label_037、GND_Label_038、GND_Label_039、GND_Label_040、GND_Label_043、GND_Label_044、GND_Label_045、GND_Label_046、GND_Label_047、GND_Label_049、GND_Label_050、GND_Label_053、GND_Label_054、GND_Label_055、GND_Label_056、GND_Label_057、GND_Label_058、GND_Label_060、GND_Label_064、GND_Label_065、GND_Label_069、GND_Label_080、GND_Label_081、GND_Label_085、GND_Label_086、GND_Label_087、GND_Label_088、GND_Label_089、GND_Label_090、GND_Label_091、GND_Label_092、GND_Label_093、GND_Label_094、GND_Label_095、GND_Label_096、GND_Label_097、GND_Label_098、GND_Label_099、PVLabel_Module_GND、PVLabel_Voltage_CGround、PVLabel_Voltage_RGround、ProtectionNet_RETURN
      | 実際につながる端子  ; BT1 (RConn:1)、C1 (RConn:1)、C10 (RConn:1)、C13 (RConn:1)、C14 (RConn:1)、C15 (RConn:1)、C16 (RConn:1)、C17 (RConn:1)、C18 (RConn:1)、C19 (RConn:1)、C2 (RConn:1)、C20 (RConn:1)、C21 (RConn:1)、C23 (RConn:1)、C24 (RConn:1)、C25 (RConn:1)、C26 (RConn:1)、C27 (RConn:1)、C28 (RConn:1)、C29 (RConn:1)、C3 (RConn:1)、C30 (RConn:1)、C31 (RConn:1)、C33 (RConn:1)、C34 (RConn:1)、C35 (RConn:1)、C36 (RConn:1)、C4 (RConn:1)、C40 (RConn:1)、C41 (RConn:1)、C42 (RConn:1)、C43 (RConn:1)、C44 (RConn:1)、C45 (RConn:1)、C46 (RConn:1)、C47 (RConn:1)、C48 (RConn:1)、C7 (RConn:1)、C8 (RConn:1)、C9 (RConn:1)、LTC4364_Protection (LConn:3)、PV1 (LConn:1)、PV_CV_ADC (RConn:1)、PV_RV_L (RConn:1)、PV_Reverse_Protection (LConn:2)、Q3A (RConn:2)、Q3B (RConn:2)、R1 (RConn:1)、R18 (RConn:1)、R21 (RConn:1)、R24 (RConn:1)、R35 (RConn:1)、R42 (RConn:1)、R48 (RConn:1)、U1 (RConn:3)、U1 (RConn:8)、U11 (LConn:3)、U12 (LConn:2)、U3 (LConn:2)、U3 (LConn:3)、U3 (LConn:4)、U4 (RConn:1)、U5 (RConn:1)、U6 (RConn:1)、U7 (LConn:13)、U7 (LConn:18)、U7 (LConn:3)、U7 (LConn:8)、U7 (RConn:13)、U7 (RConn:18)、U7 (RConn:3)、U7 (RConn:8)、U9 (RConn:3)
  PVLabel_Voltage_Input : ConnectionLabel  Description=|  Label=PV_FUSED
      | 接続名              ; PV_FUSED
      | この接続の役割      ; 電源。この階層内の同名ラベルを電気的に結ぶ。
      | この場所の接続先    ; solar_pv_protected_c06_circuit/PV_RV_H1
      | 階層の境界          ; 異なる階層とはConnection Portで明示的に接続する。
      | 同階層の同名接続    ; PVLabel_Input、PVLabel_Voltage_Input
      | 実際につながる端子  ; PV_RV_H1 (LConn:1)
  PVLabel_Voltage_RGround : ConnectionLabel  Description=|  Label=GND
      | 接続名              ; GND
      | この接続の役割      ; 共通GND。この階層内の同名ラベルを電気的に結ぶ。
      | この場所の接続先    ; solar_pv_protected_c06_circuit/PV_RV_L
      | 階層の境界          ; 異なる階層とはConnection Portで明示的に接続する。
      | 同階層の同名接続    ; GND_Label_001、GND_Label_002、GND_Label_003、GND_Label_006、GND_Label_007、GND_Label_008、GND_Label_009、GND_Label_010、GND_Label_011、GND_Label_012、GND_Label_013、GND_Label_014、GND_Label_015、GND_Label_017、GND_Label_018、GND_Label_019、GND_Label_020、GND_Label_021、GND_Label_022、GND_Label_023、GND_Label_024、GND_Label_025、GND_Label_026、GND_Label_027、GND_Label_028、GND_Label_029、GND_Label_030、GND_Label_031、GND_Label_032、GND_Label_033、GND_Label_034、GND_Label_035、GND_Label_036、GND_Label_037、GND_Label_038、GND_Label_039、GND_Label_040、GND_Label_043、GND_Label_044、GND_Label_045、GND_Label_046、GND_Label_047、GND_Label_049、GND_Label_050、GND_Label_053、GND_Label_054、GND_Label_055、GND_Label_056、GND_Label_057、GND_Label_058、GND_Label_060、GND_Label_064、GND_Label_065、GND_Label_069、GND_Label_080、GND_Label_081、GND_Label_085、GND_Label_086、GND_Label_087、GND_Label_088、GND_Label_089、GND_Label_090、GND_Label_091、GND_Label_092、GND_Label_093、GND_Label_094、GND_Label_095、GND_Label_096、GND_Label_097、GND_Label_098、GND_Label_099、PVLabel_Module_GND、PVLabel_Voltage_CGround、PVLabel_Voltage_RGround、ProtectionNet_RETURN
      | 実際につながる端子  ; BT1 (RConn:1)、C1 (RConn:1)、C10 (RConn:1)、C13 (RConn:1)、C14 (RConn:1)、C15 (RConn:1)、C16 (RConn:1)、C17 (RConn:1)、C18 (RConn:1)、C19 (RConn:1)、C2 (RConn:1)、C20 (RConn:1)、C21 (RConn:1)、C23 (RConn:1)、C24 (RConn:1)、C25 (RConn:1)、C26 (RConn:1)、C27 (RConn:1)、C28 (RConn:1)、C29 (RConn:1)、C3 (RConn:1)、C30 (RConn:1)、C31 (RConn:1)、C33 (RConn:1)、C34 (RConn:1)、C35 (RConn:1)、C36 (RConn:1)、C4 (RConn:1)、C40 (RConn:1)、C41 (RConn:1)、C42 (RConn:1)、C43 (RConn:1)、C44 (RConn:1)、C45 (RConn:1)、C46 (RConn:1)、C47 (RConn:1)、C48 (RConn:1)、C7 (RConn:1)、C8 (RConn:1)、C9 (RConn:1)、LTC4364_Protection (LConn:3)、PV1 (LConn:1)、PV_CV_ADC (RConn:1)、PV_RV_L (RConn:1)、PV_Reverse_Protection (LConn:2)、Q3A (RConn:2)、Q3B (RConn:2)、R1 (RConn:1)、R18 (RConn:1)、R21 (RConn:1)、R24 (RConn:1)、R35 (RConn:1)、R42 (RConn:1)、R48 (RConn:1)、U1 (RConn:3)、U1 (RConn:8)、U11 (LConn:3)、U12 (LConn:2)、U3 (LConn:2)、U3 (LConn:3)、U3 (LConn:4)、U4 (RConn:1)、U5 (RConn:1)、U6 (RConn:1)、U7 (LConn:13)、U7 (LConn:18)、U7 (LConn:3)、U7 (LConn:8)、U7 (RConn:13)、U7 (RConn:18)、U7 (RConn:3)、U7 (RConn:8)、U9 (RConn:3)
  PV_CV_ADC : fl_lib/Electrical/Electrical Elements/Capacitor  Description=|  c=1e-07 F  r=1e-6 Ohm  g=0 1/Ohm  i_specify=off  i_priority=None  i=0 A  i_nominal_specify=off  i_nominal_value=1  i_nominal_unit=A  v_specify=off  v_priority=None  v=0 V  v_nominal_specify=off  v_nominal_value=1  v_nominal_unit=V  vc_specify=off  vc_priority=High  vc=0 V  vc_nominal_specify=off  vc_nominal_value=1  vc_nominal_unit=V
      | この回路での名前    ; PV_CV_ADC
      | 部品名              ; CC0603KRX7R9BB104
      | この回路での役割    ; 上流パネル電圧のADC入力を落ち着かせる局所コンデンサ。
      | ここでの動き        ; 75 kΩを2本直列にした上側と3.3 kΩの下側で、保護より上流のPV_FUSEDをADC_VPV_INPUTへ分圧する。100 nFはMCP3208のCH7/AGND近傍へ置く。保護OFF中にもパネル電圧を読み、CH0の保護後VINと比較して復帰条件を判断する。
      | 公称計算            ; 分圧比=3300/(75000+75000+3300)=0.0215264。90.34 V入力で約1.945 V、110 Vで約2.368 V。Rth≈3.229 kΩ、100 nFとの時定数≈323 µs。これらは公称計算で公差・ADC誤差を含まない。
      | 読み取り条件        ; MCP3208の取得時間は1.5クロック。大きなソース抵抗は取得精度へ影響する。復帰判定には少なくとも5 ms等の整定待ちと十分な電圧差余裕を置き、ADCのクロック/チャネル切替/漏れ/基準誤差を別途検証する。速い逆流遮断の判定には使わない。
      | モデルの範囲        ; 標準Simscapeの公称R/C。ADC内部のサンプル保持、入力クランプ、無電源時の流入、基板寄生はこの部品モデルだけでは再現しない。
      | メーカー根拠        ; Microchip MCP3204/3208 DS21298E §4.1, Fig4-1/4-2, §6.3: https://ww1.microchip.com/downloads/aemDocuments/documents/APID/ProductDocuments/DataSheets/21298e.pdf 。Susumu RG series: https://www.susumu.co.jp/common/pdf/e_all.pdf 。部品型番/値は既存R16/R17/R18/C19と同じ。
      | 用語                ; ADC：Analog-to-Digital Converter（アナログ・デジタル変換器）。Rth：Thevenin resistance（分圧回路の出力から見た等価抵抗）。CH：Channel（入力チャネル）。AGND：Analog Ground（アナログ基準）。MLCC：Multilayer Ceramic Capacitor（積層セラミックコンデンサ）。
      settings: AttributesFormatString=|
      | MLCC
      | 100 nF
  PV_RV_H1 : fl_lib/Electrical/Electrical Elements/Resistor  Description=|  R=75000 Ohm  i_specify=off  i_priority=None  i=0 A  i_nominal_specify=off  i_nominal_value=1  i_nominal_unit=A  v_specify=off  v_priority=None  v=0 V  v_nominal_specify=off  v_nominal_value=1  v_nominal_unit=V
      | この回路での名前    ; PV_RV_H1
      | 部品名              ; RG2012P-753-B-T5
      | この回路での役割    ; 上流パネル電圧をADCへ渡す分圧器の上側1本目。
      | ここでの動き        ; 75 kΩを2本直列にした上側と3.3 kΩの下側で、保護より上流のPV_FUSEDをADC_VPV_INPUTへ分圧する。100 nFはMCP3208のCH7/AGND近傍へ置く。保護OFF中にもパネル電圧を読み、CH0の保護後VINと比較して復帰条件を判断する。
      | 公称計算            ; 分圧比=3300/(75000+75000+3300)=0.0215264。90.34 V入力で約1.945 V、110 Vで約2.368 V。Rth≈3.229 kΩ、100 nFとの時定数≈323 µs。これらは公称計算で公差・ADC誤差を含まない。
      | 読み取り条件        ; MCP3208の取得時間は1.5クロック。大きなソース抵抗は取得精度へ影響する。復帰判定には少なくとも5 ms等の整定待ちと十分な電圧差余裕を置き、ADCのクロック/チャネル切替/漏れ/基準誤差を別途検証する。速い逆流遮断の判定には使わない。
      | モデルの範囲        ; 標準Simscapeの公称R/C。ADC内部のサンプル保持、入力クランプ、無電源時の流入、基板寄生はこの部品モデルだけでは再現しない。
      | メーカー根拠        ; Microchip MCP3204/3208 DS21298E §4.1, Fig4-1/4-2, §6.3: https://ww1.microchip.com/downloads/aemDocuments/documents/APID/ProductDocuments/DataSheets/21298e.pdf 。Susumu RG series: https://www.susumu.co.jp/common/pdf/e_all.pdf 。部品型番/値は既存R16/R17/R18/C19と同じ。
      | 用語                ; ADC：Analog-to-Digital Converter（アナログ・デジタル変換器）。Rth：Thevenin resistance（分圧回路の出力から見た等価抵抗）。CH：Channel（入力チャネル）。AGND：Analog Ground（アナログ基準）。MLCC：Multilayer Ceramic Capacitor（積層セラミックコンデンサ）。
      settings: AttributesFormatString=75 kΩ
  PV_RV_H2 : fl_lib/Electrical/Electrical Elements/Resistor  Description=|  R=75000 Ohm  i_specify=off  i_priority=None  i=0 A  i_nominal_specify=off  i_nominal_value=1  i_nominal_unit=A  v_specify=off  v_priority=None  v=0 V  v_nominal_specify=off  v_nominal_value=1  v_nominal_unit=V
      | この回路での名前    ; PV_RV_H2
      | 部品名              ; RG2012P-753-B-T5
      | この回路での役割    ; 上流パネル電圧をADCへ渡す分圧器の上側2本目。
      | ここでの動き        ; 75 kΩを2本直列にした上側と3.3 kΩの下側で、保護より上流のPV_FUSEDをADC_VPV_INPUTへ分圧する。100 nFはMCP3208のCH7/AGND近傍へ置く。保護OFF中にもパネル電圧を読み、CH0の保護後VINと比較して復帰条件を判断する。
      | 公称計算            ; 分圧比=3300/(75000+75000+3300)=0.0215264。90.34 V入力で約1.945 V、110 Vで約2.368 V。Rth≈3.229 kΩ、100 nFとの時定数≈323 µs。これらは公称計算で公差・ADC誤差を含まない。
      | 読み取り条件        ; MCP3208の取得時間は1.5クロック。大きなソース抵抗は取得精度へ影響する。復帰判定には少なくとも5 ms等の整定待ちと十分な電圧差余裕を置き、ADCのクロック/チャネル切替/漏れ/基準誤差を別途検証する。速い逆流遮断の判定には使わない。
      | モデルの範囲        ; 標準Simscapeの公称R/C。ADC内部のサンプル保持、入力クランプ、無電源時の流入、基板寄生はこの部品モデルだけでは再現しない。
      | メーカー根拠        ; Microchip MCP3204/3208 DS21298E §4.1, Fig4-1/4-2, §6.3: https://ww1.microchip.com/downloads/aemDocuments/documents/APID/ProductDocuments/DataSheets/21298e.pdf 。Susumu RG series: https://www.susumu.co.jp/common/pdf/e_all.pdf 。部品型番/値は既存R16/R17/R18/C19と同じ。
      | 用語                ; ADC：Analog-to-Digital Converter（アナログ・デジタル変換器）。Rth：Thevenin resistance（分圧回路の出力から見た等価抵抗）。CH：Channel（入力チャネル）。AGND：Analog Ground（アナログ基準）。MLCC：Multilayer Ceramic Capacitor（積層セラミックコンデンサ）。
      settings: AttributesFormatString=75 kΩ
  PV_RV_L : fl_lib/Electrical/Electrical Elements/Resistor  Description=|  R=3300 Ohm  i_specify=off  i_priority=None  i=0 A  i_nominal_specify=off  i_nominal_value=1  i_nominal_unit=A  v_specify=off  v_priority=None  v=0 V  v_nominal_specify=off  v_nominal_value=1  v_nominal_unit=V
      | この回路での名前    ; PV_RV_L
      | 部品名              ; RG2012P-332-B-T5
      | この回路での役割    ; 上流パネル電圧をADCで読める電圧へ下げる分圧器の下側抵抗。
      | ここでの動き        ; 75 kΩを2本直列にした上側と3.3 kΩの下側で、保護より上流のPV_FUSEDをADC_VPV_INPUTへ分圧する。100 nFはMCP3208のCH7/AGND近傍へ置く。保護OFF中にもパネル電圧を読み、CH0の保護後VINと比較して復帰条件を判断する。
      | 公称計算            ; 分圧比=3300/(75000+75000+3300)=0.0215264。90.34 V入力で約1.945 V、110 Vで約2.368 V。Rth≈3.229 kΩ、100 nFとの時定数≈323 µs。これらは公称計算で公差・ADC誤差を含まない。
      | 読み取り条件        ; MCP3208の取得時間は1.5クロック。大きなソース抵抗は取得精度へ影響する。復帰判定には少なくとも5 ms等の整定待ちと十分な電圧差余裕を置き、ADCのクロック/チャネル切替/漏れ/基準誤差を別途検証する。速い逆流遮断の判定には使わない。
      | モデルの範囲        ; 標準Simscapeの公称R/C。ADC内部のサンプル保持、入力クランプ、無電源時の流入、基板寄生はこの部品モデルだけでは再現しない。
      | メーカー根拠        ; Microchip MCP3204/3208 DS21298E §4.1, Fig4-1/4-2, §6.3: https://ww1.microchip.com/downloads/aemDocuments/documents/APID/ProductDocuments/DataSheets/21298e.pdf 。Susumu RG series: https://www.susumu.co.jp/common/pdf/e_all.pdf 。部品型番/値は既存R16/R17/R18/C19と同じ。
      | 用語                ; ADC：Analog-to-Digital Converter（アナログ・デジタル変換器）。Rth：Thevenin resistance（分圧回路の出力から見た等価抵抗）。CH：Channel（入力チャネル）。AGND：Analog Ground（アナログ基準）。MLCC：Multilayer Ceramic Capacitor（積層セラミックコンデンサ）。
      settings: AttributesFormatString=3.3 kΩ
  PV_Reverse_Protection : Subsystem  Description=|
      | この回路での名前    ; PV_Reverse_Protection
      | 部品名              ; パネル側保護回路（詳細は内部）
      | この回路での役割    ; パネル電流を測り、逆流または許可条件消失で電力経路を遮断する。
      | ここでの動き        ; R27、L2、U2を内部へ移し、2個のMOSFETをLTC7000Aで開閉する。
      | 試験との対応        ; 入力の保存モジュールと同じ部品・接続を回路図へ複写する。個々の試験範囲は証拠記録を参照する。
      | モデルの範囲        ; 実部品の回路図表現。試験電源・観測・計算補助を含まない。図面単独の実行可能性は要求しない。
      | 元モジュールSHA256  ; f40bf5e1ef20bc97d0d4775a6ac457f3c30378c5fe9d07d29ab7bde4d975da32
